simulink model "Hexalock.slx"  (R2026b)
settings: Solver=VariableStepAuto  StopTime=inf
undefined symbols (not defined in the file): gray
(part 1 of 5)
settings Model: Creator=joseph  LastModifiedBy=Medici

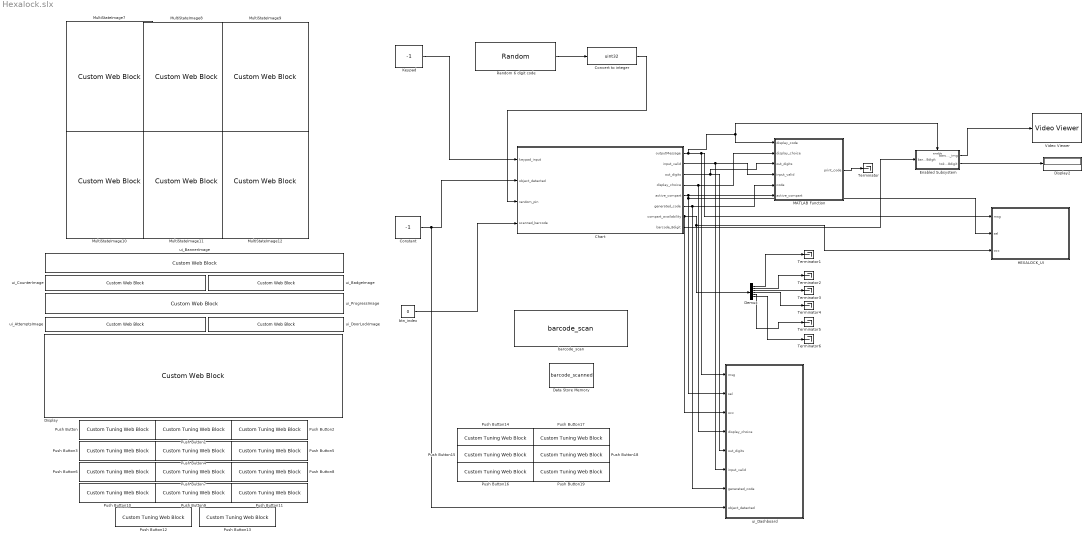
== system Hexalock.slx ==
  Chart : Stateflow chart  TreatAsAtomicUnit=on
  Constant : Constant  Value=-1
  Convert to integer : DataTypeConversion  OutDataTypeStr=uint32  RndMeth=Floor
  Data Store Memory : DataStoreMemory  DataStoreName=barcode_scanned  WriteAfterWriteMsg=warning  ShowAdditionalParam=off  OutDataTypeStr=double  Dimensions=1
  Demux : Demux  Outputs=6
  Display : CustomWebBlock  LabelPosition=Hide  ShowInitialText=on  Configuration="{\"components\":[{\"name\":\"DisplayComponent\",\"settings\":{\"alignment\":\"center\",\"bold\":false,\"font\":\"Noto Sans\",\"fontColor\":[255,255,200],\"fontSize\":18,\"format\":\"short\",\"formatString\":\"%d\",\"gridColor\":[252,252,197],\"italic\":false,\"position\":[0.1524671052631579,-0.02081787833827893,1.1009829376854599,0.7483552631578947],\"showGrid\":true,\"underline\":false}},{\"name\":\"BackgroundImageComponent\",\"settings\":{\"image\":{\"size\":[920,260],\"src\":\"data:image\\/svg+xml;base64,PHN2ZyB4bWxucz0iaHR0cDovL3d3dy53My5vcmcvMjAwMC9zdmciIHdpZHRoPSI5MjAiIGhlaWdodD0iMjYwIiB2aWV3Qm94PSIwIDAgOTIwIDI2MCI+CiAgPGRlZnM+CiAgICA8bGluZWFyR3JhZGllbnQgaWQ9InNoZWxsIiB4MT0iMCIgeTE9IjAiIHgyPSIwIiB5Mj0iMSI+CiAgICAgIDxzdG9wIG9mZnNldD0iMCIgc3RvcC1jb2xvcj0iIzQyNDk0RSIvPgogICAgICA8c3RvcCBvZmZzZXQ9IjAuNTAiIHN0b3AtY29sb3I9IiMyOTJGMzQiLz4KICAgICAgPHN0b3Agb2Zmc2V0PSIxIiBzdG9wLWNvbG9yPSIjMUIyMjI2Ii8+CiAg ...(+4416 chars)\",\"srcOrientation\":\"Right\"},\"position\":[0,0,1,1],\"scaleMode\":\"0\"}},{\"name\":\"ForegroundImageComponent\",\"settings\":{\"angle\":0,\"image\":{\"size\":[0,0],\"src\":\"default\"},\"isForeground\":1,\"position\":[0,0,1,1],\"scaleMode\":\"0\"}}],\"derived\":{\"blockParameters\":{\"alignment\":\"center\",\"fixedAspectRatio\":\"on\",\"format\":\"short\",\"formatString\":\"%d\",\"gridColor\":[252,252,197],\"showGrid\":true}},\"settings\":{\"BindingType\":\"signal\",\"aspectRatio\":1.032258064516129,\"backgroundColor\":[0,0,0,\"1\"],\"backgroundOffset\":0.14,\"backgroundOpacity\":1,\"fixedAspectRatio\":\"on\",\"showBackgroundColor\":false,\"value\":0,\"version\":\"R2026b\"},\"type\":\"Display\"}"
  Display2 : Display
  Enabled Subsystem : Subsystem  TreatAsAtomicUnit=on
  HEXALOCK_UI : Subsystem  Description=DISPLAY ONLY. Derives the per-locker visual code (0-11) from read-only branches of the controller outputs outputMessage, active_compart and compart_availability. Nothing in here feeds back into the controller.
  Keypad : Constant  Value=-1  VectorParams1D=off  OutDataTypeStr=double
  MATLAB Function : MATLAB Function  TreatAsAtomicUnit=on
  MultiStateImage10 : CustomWebBlock  LabelPosition=Hide  ShowInitialText=on  Configuration="{\"components\":[{\"name\":\"BackgroundImageComponent\",\"settings\":{\"image\":{\"size\":[0,0],\"src\":\"default\",\"srcOrientation\":\"Right\"},\"position\":[0,0,1,1],\"scaleMode\":\"0\"}},{\"name\":\"MultistateImageStateComponent\",\"settings\":{\"applyDefaults\":true,\"position\":[0,0,1,1],\"states\":[{\"image\":{\"size\":[0.7746478873239436,1],\"src\":\"data:image\\/svg+xml;base64,PHN2ZyB4bWxucz0iaHR0cDovL3d3dy53My5vcmcvMjAwMC9zdmciIHdpZHRoPSIyMjAiIGhlaWdodD0iMjg0IiB2aWV3Qm94PSIwIDAgMjIwIDI4NCIgcm9sZT0iaW1nIiA+Cjx0aXRsZT5IRVhBTE9DSyBtb2R1bGFyIGludGVyZmFjZSBhc3NldDwvdGl0bGU+CjxkZWZzPjwvZGVmcz4KICAgICAgPHJlY3QgeD0iOCIgeT0iOCIgd2lkdGg9IjIwNCIgaGVpZ2h0PSIyNjgiIHJ4PSIxNCIgZmlsbD0iIzExMUMyMiIgc3Ryb2tlPSIjNTM2NjZFIiBzdHJva2Utd2lkdGg9IjIiLz4KICAgICAgPHJlY3QgeD0iMTIiIHk9IjEyIiB3aWR0 ...(+3224 chars)\",\"srcOrientation\":\"Right\"},\"position\":[0,0,1,1],\"value\":[]},{\"image\":{\"size\":[0,0],\"src\":\"data:image\\/svg+xml;base64,PHN2ZyB4bWxucz0iaHR0cDovL3d3dy53My5vcmcvMjAwMC9zdmciIHdpZHRoPSIyMjAiIGhlaWdodD0iMjg0IiB2aWV3Qm94PSIwIDAgMjIwIDI4NCIgcm9sZT0iaW1nIiA+Cjx0aXRsZT5IRVhBTE9DSyBtb2R1bGFyIGludGVyZmFjZSBhc3NldDwvdGl0bGU+CjxkZWZzPjwvZGVmcz4KICAgICAgPHJlY3QgeD0iOCIgeT0iOCIgd2lkdGg9IjIwNCIgaGVpZ2h0PSIyNjgiIHJ4PSIxNCIgZmlsbD0iIzExMUMyMiIgc3Ryb2tlPSIjNTM2NjZFIiBzdHJva2Utd2lkdGg9IjIiLz4KICAgICAgPHJlY3QgeD0iMTIiIHk9IjEyIiB3aWR0 ...(+3224 chars)\",\"srcOrientation\":\"Right\"},\"position\":[0,0,1,1],\"value\":\"0\"},{\"image\":{\"size\":[0,0],\"src\":\"data:image\\/svg+xml;base64,PHN2ZyB4bWxucz0iaHR0cDovL3d3dy53My5vcmcvMjAwMC9zdmciIHdpZHRoPSIyMjAiIGhlaWdodD0iMjg0IiB2aWV3Qm94PSIwIDAgMjIwIDI4NCIgcm9sZT0iaW1nIiA+Cjx0aXRsZT5IRVhBTE9DSyBtb2R1bGFyIGludGVyZmFjZSBhc3NldDwvdGl0bGU+CjxkZWZzPjwvZGVmcz4KICAgICAgPHJlY3QgeD0iOCIgeT0iOCIgd2lkdGg9IjIwNCIgaGVpZ2h0PSIyNjgiIHJ4PSIxNCIgZmlsbD0iIzExMUMyMiIgc3Ryb2tlPSIjNTM2NjZFIiBzdHJva2Utd2lkdGg9IjIiLz4KICAgICAgPHJlY3QgeD0iMTIiIHk9IjEyIiB3aWR0 ...(+3220 chars)\",\"srcOrientation\":\"Right\"},\"position\":[0,0,1,1],\"value\":\"1\"},{\"image\":{\"size\":[0,0],\"src\":\"data:image\\/svg+xml;base64,PHN2ZyB4bWxucz0iaHR0cDovL3d3dy53My5vcmcvMjAwMC9zdmciIHdpZHRoPSIyMjAiIGhlaWdodD0iMjg0IiB2aWV3Qm94PSIwIDAgMjIwIDI4NCIgcm9sZT0iaW1nIiA+Cjx0aXRsZT5IRVhBTE9DSyBtb2R1bGFyIGludGVyZmFjZSBhc3NldDwvdGl0bGU+CjxkZWZzPjwvZGVmcz4KICAgICAgPHJlY3QgeD0iOCIgeT0iOCIgd2lkdGg9IjIwNCIgaGVpZ2h0PSIyNjgiIHJ4PSIxNCIgZmlsbD0iIzExMUMyMiIgc3Ryb2tlPSIjQjk4NTZFIiBzdHJva2Utd2lkdGg9IjIuNiIvPgogICAgICA8cmVjdCB4PSIxMiIgeT0iMTIiIHdp ...(+3488 chars)\",\"srcOrientation\":\"Right\"},\"position\":[0,0,1,1],\"value\":\"2\"},{\"image\":{\"size\":[0,0],\"src\":\"data:image\\/svg+xml;base64,PHN2ZyB4bWxucz0iaHR0cDovL3d3dy53My5vcmcvMjAwMC9zdmciIHdpZHRoPSIyMjAiIGhlaWdodD0iMjg0IiB2aWV3Qm94PSIwIDAgMjIwIDI4NCIgcm9sZT0iaW1nIiA+Cjx0aXRsZT5IRVhBTE9DSyBtb2R1bGFyIGludGVyZmFjZSBhc3NldDwvdGl0bGU+CjxkZWZzPjwvZGVmcz4KICAgICAgPHJlY3QgeD0iOCIgeT0iOCIgd2lkdGg9IjIwNCIgaGVpZ2h0PSIyNjgiIHJ4PSIxNCIgZmlsbD0iIzExMUMyMiIgc3Ryb2tlPSIjQjk4NTZFIiBzdHJva2Utd2lkdGg9IjIuNiIvPgogICAgICA8cmVjdCB4PSIxMiIgeT0iMTIiIHdp ...(+3484 chars)\",\"srcOrientation\":\"Right\"},\"position\":[0,0,1,1],\"value\":\"3\"},{\"image\":{\"size\":[0,0],\"src\":\"data:image\\/svg+xml;base64,PHN2ZyB4bWxucz0iaHR0cDovL3d3dy53My5vcmcvMjAwMC9zdmciIHdpZHRoPSIyMjAiIGhlaWdodD0iMjg0IiB2aWV3Qm94PSIwIDAgMjIwIDI4NCIgcm9sZT0iaW1nIiA+Cjx0aXRsZT5IRVhBTE9DSyBtb2R1bGFyIGludGVyZmFjZSBhc3NldDwvdGl0bGU+CjxkZWZzPjwvZGVmcz4KICAgICAgPHJlY3QgeD0iOCIgeT0iOCIgd2lkdGg9IjIwNCIgaGVpZ2h0PSIyNjgiIHJ4PSIxNCIgZmlsbD0iIzExMUMyMiIgc3Ryb2tlPSIjQjk4NTZFIiBzdHJva2Utd2lkdGg9IjIuNiIvPgogICAgICA8cmVjdCB4PSIxMiIgeT0iMTIiIHdp ...(+3532 chars)\",\"srcOrientation\":\"Right\"},\"position\":[0,0,1,1],\"value\":\"4\"},{\"image\":{\"size\":[0,0],\"src\":\"data:image\\/svg+xml;base64,PHN2ZyB4bWxucz0iaHR0cDovL3d3dy53My5vcmcvMjAwMC9zdmciIHdpZHRoPSIyMjAiIGhlaWdodD0iMjg0IiB2aWV3Qm94PSIwIDAgMjIwIDI4NCIgcm9sZT0iaW1nIiA+Cjx0aXRsZT5IRVhBTE9DSyBtb2R1bGFyIGludGVyZmFjZSBhc3NldDwvdGl0bGU+CjxkZWZzPjwvZGVmcz4KICAgICAgPHJlY3QgeD0iOCIgeT0iOCIgd2lkdGg9IjIwNCIgaGVpZ2h0PSIyNjgiIHJ4PSIxNCIgZmlsbD0iIzExMUMyMiIgc3Ryb2tlPSIjQjk4NTZFIiBzdHJva2Utd2lkdGg9IjIuNiIvPgogICAgICA8cmVjdCB4PSIxMiIgeT0iMTIiIHdp ...(+3532 chars)\",\"srcOrientation\":\"Right\"},\"position\":[0,0,1,1],\"value\":\"5\"},{\"image\":{\"size\":[0,0],\"src\":\"data:image\\/svg+xml;base64,PHN2ZyB4bWxucz0iaHR0cDovL3d3dy53My5vcmcvMjAwMC9zdmciIHdpZHRoPSIyMjAiIGhlaWdodD0iMjg0IiB2aWV3Qm94PSIwIDAgMjIwIDI4NCIgcm9sZT0iaW1nIiA+Cjx0aXRsZT5IRVhBTE9DSyBtb2R1bGFyIGludGVyZmFjZSBhc3NldDwvdGl0bGU+CjxkZWZzPjwvZGVmcz4KICAgICAgPHJlY3QgeD0iOCIgeT0iOCIgd2lkdGg9IjIwNCIgaGVpZ2h0PSIyNjgiIHJ4PSIxNCIgZmlsbD0iIzExMUMyMiIgc3Ryb2tlPSIjQjk4NTZFIiBzdHJva2Utd2lkdGg9IjIuNiIvPgogICAgICA8cmVjdCB4PSIxMiIgeT0iMTIiIHdp ...(+3532 chars)\",\"srcOrientation\":\"Right\"},\"position\":[0,0,1,1],\"value\":\"6\"},{\"image\":{\"size\":[0,0],\"src\":\"data:image\\/svg+xml;base64,PHN2ZyB4bWxucz0iaHR0cDovL3d3dy53My5vcmcvMjAwMC9zdmciIHdpZHRoPSIyMjAiIGhlaWdodD0iMjg0IiB2aWV3Qm94PSIwIDAgMjIwIDI4NCIgcm9sZT0iaW1nIiA+Cjx0aXRsZT5IRVhBTE9DSyBtb2R1bGFyIGludGVyZmFjZSBhc3NldDwvdGl0bGU+CjxkZWZzPjwvZGVmcz4KICAgICAgPHJlY3QgeD0iOCIgeT0iOCIgd2lkdGg9IjIwNCIgaGVpZ2h0PSIyNjgiIHJ4PSIxNCIgZmlsbD0iIzExMUMyMiIgc3Ryb2tlPSIjQjk4NTZFIiBzdHJva2Utd2lkdGg9IjIuNiIvPgogICAgICA8cmVjdCB4PSIxMiIgeT0iMTIiIHdp ...(+3524 chars)\",\"srcOrientation\":\"Right\"},\"position\":[0,0,1,1],\"value\":\"7\"},{\"image\":{\"size\":[0,0],\"src\":\"data:image\\/svg+xml;base64,PHN2ZyB4bWxucz0iaHR0cDovL3d3dy53My5vcmcvMjAwMC9zdmciIHdpZHRoPSIyMjAiIGhlaWdodD0iMjg0IiB2aWV3Qm94PSIwIDAgMjIwIDI4NCIgcm9sZT0iaW1nIiA+Cjx0aXRsZT5IRVhBTE9DSyBtb2R1bGFyIGludGVyZmFjZSBhc3NldDwvdGl0bGU+CjxkZWZzPjwvZGVmcz4KICAgICAgPHJlY3QgeD0iOCIgeT0iOCIgd2lkdGg9IjIwNCIgaGVpZ2h0PSIyNjgiIHJ4PSIxNCIgZmlsbD0iIzExMUMyMiIgc3Ryb2tlPSIjQjk4NTZFIiBzdHJva2Utd2lkdGg9IjIuNiIvPgogICAgICA8cmVjdCB4PSIxMiIgeT0iMTIiIHdp ...(+3532 chars)\",\"srcOrientation\":\"Right\"},\"position\":[0,0,1,1],\"value\":\"8\"},{\"image\":{\"size\":[0,0],\"src\":\"data:image\\/svg+xml;base64,PHN2ZyB4bWxucz0iaHR0cDovL3d3dy53My5vcmcvMjAwMC9zdmciIHdpZHRoPSIyMjAiIGhlaWdodD0iMjg0IiB2aWV3Qm94PSIwIDAgMjIwIDI4NCIgcm9sZT0iaW1nIiA+Cjx0aXRsZT5IRVhBTE9DSyBtb2R1bGFyIGludGVyZmFjZSBhc3NldDwvdGl0bGU+CjxkZWZzPjwvZGVmcz4KICAgICAgPHJlY3QgeD0iOCIgeT0iOCIgd2lkdGg9IjIwNCIgaGVpZ2h0PSIyNjgiIHJ4PSIxNCIgZmlsbD0iIzExMUMyMiIgc3Ryb2tlPSIjQjk4NTZFIiBzdHJva2Utd2lkdGg9IjIuNiIvPgogICAgICA8cmVjdCB4PSIxMiIgeT0iMTIiIHdp ...(+3532 chars)\",\"srcOrientation\":\"Right\"},\"position\":[0,0,1,1],\"value\":\"9\"},{\"image\":{\"size\":[0,0],\"src\":\"data:image\\/svg+xml;base64,PHN2ZyB4bWxucz0iaHR0cDovL3d3dy53My5vcmcvMjAwMC9zdmciIHdpZHRoPSIyMjAiIGhlaWdodD0iMjg0IiB2aWV3Qm94PSIwIDAgMjIwIDI4NCIgcm9sZT0iaW1nIiA+Cjx0aXRsZT5IRVhBTE9DSyBtb2R1bGFyIGludGVyZmFjZSBhc3NldDwvdGl0bGU+CjxkZWZzPjwvZGVmcz4KICAgICAgPHJlY3QgeD0iOCIgeT0iOCIgd2lkdGg9IjIwNCIgaGVpZ2h0PSIyNjgiIHJ4PSIxNCIgZmlsbD0iIzExMUMyMiIgc3Ryb2tlPSIjQjk4NTZFIiBzdHJva2Utd2lkdGg9IjIuNiIvPgogICAgICA8cmVjdCB4PSIxMiIgeT0iMTIiIHdp ...(+3532 chars)\",\"srcOrientation\":\"Right\"},\"position\":[0,0,1,1],\"value\":\"10\"},{\"image\":{\"size\":[0,0],\"src\":\"data:image\\/svg+xml;base64,PHN2ZyB4bWxucz0iaHR0cDovL3d3dy53My5vcmcvMjAwMC9zdmciIHdpZHRoPSIyMjAiIGhlaWdodD0iMjg0IiB2aWV3Qm94PSIwIDAgMjIwIDI4NCIgcm9sZT0iaW1nIiA+Cjx0aXRsZT5IRVhBTE9DSyBtb2R1bGFyIGludGVyZmFjZSBhc3NldDwvdGl0bGU+CjxkZWZzPjwvZGVmcz4KICAgICAgPHJlY3QgeD0iOCIgeT0iOCIgd2lkdGg9IjIwNCIgaGVpZ2h0PSIyNjgiIHJ4PSIxNCIgZmlsbD0iIzExMUMyMiIgc3Ryb2tlPSIjNTM2NjZFIiBzdHJva2Utd2lkdGg9IjIiLz4KICAgICAgPHJlY3QgeD0iMTIiIHk9IjEyIiB3aWR0 ...(+3220 chars)\",\"srcOrientation\":\"Right\"},\"position\":[0,0,1,1],\"value\":\"11\"},{\"image\":{\"size\":[0,0],\"src\":\"data:image\\/svg+xml;base64,PHN2ZyB4bWxucz0iaHR0cDovL3d3dy53My5vcmcvMjAwMC9zdmciIHdpZHRoPSIyMjAiIGhlaWdodD0iMjg0IiB2aWV3Qm94PSIwIDAgMjIwIDI4NCIgcm9sZT0iaW1nIiA+Cjx0aXRsZT5IRVhBTE9DSyBtb2R1bGFyIGludGVyZmFjZSBhc3NldDwvdGl0bGU+CjxkZWZzPjxsaW5lYXJHcmFkaWVudCBpZD0ia3JhZnRGcm9udCIgeDE9IjAiIHkxPSIwIiB4Mj0iMSIgeTI9IjEiPjxzdG9wIHN0b3AtY29sb3I9IiNEM0I5OUEiLz48c3RvcCBvZmZzZXQ9IjEiIHN0b3AtY29sb3I9IiNBMzgzNjMiLz48L2xpbmVhckdyYWRpZW50Pjxs ...(+4752 chars)\",\"srcOrientation\":\"Right\"},\"position\":[0,0,1,1],\"value\":\"20\"},{\"image\":{\"size\":[0,0],\"src\":\"data:image\\/svg+xml;base64,PHN2ZyB4bWxucz0iaHR0cDovL3d3dy53My5vcmcvMjAwMC9zdmciIHdpZHRoPSIyMjAiIGhlaWdodD0iMjg0IiB2aWV3Qm94PSIwIDAgMjIwIDI4NCIgcm9sZT0iaW1nIiA+Cjx0aXRsZT5IRVhBTE9DSyBtb2R1bGFyIGludGVyZmFjZSBhc3NldDwvdGl0bGU+CjxkZWZzPjxsaW5lYXJHcmFkaWVudCBpZD0ia3JhZnRGcm9udCIgeDE9IjAiIHkxPSIwIiB4Mj0iMSIgeTI9IjEiPjxzdG9wIHN0b3AtY29sb3I9IiNEM0I5OUEiLz48c3RvcCBvZmZzZXQ9IjEiIHN0b3AtY29sb3I9IiNBMzgzNjMiLz48L2xpbmVhckdyYWRpZW50Pjxs ...(+7264 chars)\",\"srcOrientation\":\"Right\"},\"position\":[0,0,1,1],\"value\":\"21\"},{\"image\":{\"size\":[0,0],\"src\":\"data:image\\/svg+xml;base64,PHN2ZyB4bWxucz0iaHR0cDovL3d3dy53My5vcmcvMjAwMC9zdmciIHdpZHRoPSIyMjAiIGhlaWdodD0iMjg0IiB2aWV3Qm94PSIwIDAgMjIwIDI4NCIgcm9sZT0iaW1nIiA+Cjx0aXRsZT5IRVhBTE9DSyBtb2R1bGFyIGludGVyZmFjZSBhc3NldDwvdGl0bGU+CjxkZWZzPjxsaW5lYXJHcmFkaWVudCBpZD0ia3JhZnRGcm9udCIgeDE9IjAiIHkxPSIwIiB4Mj0iMSIgeTI9IjEiPjxzdG9wIHN0b3AtY29sb3I9IiNEM0I5OUEiLz48c3RvcCBvZmZzZXQ9IjEiIHN0b3AtY29sb3I9IiNBMzgzNjMiLz48L2xpbmVhckdyYWRpZW50Pjxs ...(+7264 chars)\",\"srcOrientation\":\"Right\"},\"position\":[0,0,1,1],\"value\":\"22\"},{\"image\":{\"size\":[0,0],\"src\":\"data:image\\/svg+xml;base64,PHN2ZyB4bWxucz0iaHR0cDovL3d3dy53My5vcmcvMjAwMC9zdmciIHdpZHRoPSIyMjAiIGhlaWdodD0iMjg0IiB2aWV3Qm94PSIwIDAgMjIwIDI4NCIgcm9sZT0iaW1nIiA+Cjx0aXRsZT5IRVhBTE9DSyBtb2R1bGFyIGludGVyZmFjZSBhc3NldDwvdGl0bGU+CjxkZWZzPjxsaW5lYXJHcmFkaWVudCBpZD0ia3JhZnRGcm9udCIgeDE9IjAiIHkxPSIwIiB4Mj0iMSIgeTI9IjEiPjxzdG9wIHN0b3AtY29sb3I9IiNEM0I5OUEiLz48c3RvcCBvZmZzZXQ9IjEiIHN0b3AtY29sb3I9IiNBMzgzNjMiLz48L2xpbmVhckdyYWRpZW50Pjxs ...(+7264 chars)\",\"srcOrientation\":\"Right\"},\"position\":[0,0,1,1],\"value\":\"23\"},{\"image\":{\"size\":[0,0],\"src\":\"data:image\\/svg+xml;base64,PHN2ZyB4bWxucz0iaHR0cDovL3d3dy53My5vcmcvMjAwMC9zdmciIHdpZHRoPSIyMjAiIGhlaWdodD0iMjg0IiB2aWV3Qm94PSIwIDAgMjIwIDI4NCIgcm9sZT0iaW1nIiA+Cjx0aXRsZT5IRVhBTE9DSyBtb2R1bGFyIGludGVyZmFjZSBhc3NldDwvdGl0bGU+CjxkZWZzPjxsaW5lYXJHcmFkaWVudCBpZD0ia3JhZnRGcm9udCIgeDE9IjAiIHkxPSIwIiB4Mj0iMSIgeTI9IjEiPjxzdG9wIHN0b3AtY29sb3I9IiNEM0I5OUEiLz48c3RvcCBvZmZzZXQ9IjEiIHN0b3AtY29sb3I9IiNBMzgzNjMiLz48L2xpbmVhckdyYWRpZW50Pjxs ...(+7260 chars)\",\"srcOrientation\":\"Right\"},\"position\":[0,0,1,1],\"value\":\"24\"},{\"image\":{\"size\":[0,0],\"src\":\"data:image\\/svg+xml;base64,PHN2ZyB4bWxucz0iaHR0cDovL3d3dy53My5vcmcvMjAwMC9zdmciIHdpZHRoPSIyMjAiIGhlaWdodD0iMjg0IiB2aWV3Qm94PSIwIDAgMjIwIDI4NCIgcm9sZT0iaW1nIiA+Cjx0aXRsZT5IRVhBTE9DSyBtb2R1bGFyIGludGVyZmFjZSBhc3NldDwvdGl0bGU+CjxkZWZzPjxsaW5lYXJHcmFkaWVudCBpZD0ia3JhZnRGcm9udCIgeDE9IjAiIHkxPSIwIiB4Mj0iMSIgeTI9IjEiPjxzdG9wIHN0b3AtY29sb3I9IiNEM0I5OUEiLz48c3RvcCBvZmZzZXQ9IjEiIHN0b3AtY29sb3I9IiNBMzgzNjMiLz48L2xpbmVhckdyYWRpZW50Pjxs ...(+7264 chars)\",\"srcOrientation\":\"Right\"},\"position\":[0,0,1,1],\"value\":\"25\"},{\"image\":{\"size\":[0,0],\"src\":\"data:image\\/svg+xml;base64,PHN2ZyB4bWxucz0iaHR0cDovL3d3dy53My5vcmcvMjAwMC9zdmciIHdpZHRoPSIyMjAiIGhlaWdodD0iMjg0IiB2aWV3Qm94PSIwIDAgMjIwIDI4NCIgcm9sZT0iaW1nIiA+Cjx0aXRsZT5IRVhBTE9DSyBtb2R1bGFyIGludGVyZmFjZSBhc3NldDwvdGl0bGU+CjxkZWZzPjxsaW5lYXJHcmFkaWVudCBpZD0ia3JhZnRGcm9udCIgeDE9IjAiIHkxPSIwIiB4Mj0iMSIgeTI9IjEiPjxzdG9wIHN0b3AtY29sb3I9IiNEM0I5OUEiLz48c3RvcCBvZmZzZXQ9IjEiIHN0b3AtY29sb3I9IiNBMzgzNjMiLz48L2xpbmVhckdyYWRpZW50Pjxs ...(+7272 chars)\",\"srcOrientation\":\"Right\"},\"position\":[0,0,1,1],\"value\":\"26\"},{\"image\":{\"size\":[0,0],\"src\":\"data:image\\/svg+xml;base64,PHN2ZyB4bWxucz0iaHR0cDovL3d3dy53My5vcmcvMjAwMC9zdmciIHdpZHRoPSIyMjAiIGhlaWdodD0iMjg0IiB2aWV3Qm94PSIwIDAgMjIwIDI4NCIgcm9sZT0iaW1nIiA+Cjx0aXRsZT5IRVhBTE9DSyBtb2R1bGFyIGludGVyZmFjZSBhc3NldDwvdGl0bGU+CjxkZWZzPjxsaW5lYXJHcmFkaWVudCBpZD0ia3JhZnRGcm9udCIgeDE9IjAiIHkxPSIwIiB4Mj0iMSIgeTI9IjEiPjxzdG9wIHN0b3AtY29sb3I9IiNEM0I5OUEiLz48c3RvcCBvZmZzZXQ9IjEiIHN0b3AtY29sb3I9IiNBMzgzNjMiLz48L2xpbmVhckdyYWRpZW50Pjxs ...(+7264 chars)\",\"srcOrientation\":\"Right\"},\"position\":[0,0,1,1],\"value\":\"27\"},{\"image\":{\"size\":[0,0],\"src\":\"data:image\\/svg+xml;base64,PHN2ZyB4bWxucz0iaHR0cDovL3d3dy53My5vcmcvMjAwMC9zdmciIHdpZHRoPSIyMjAiIGhlaWdodD0iMjg0IiB2aWV3Qm94PSIwIDAgMjIwIDI4NCIgcm9sZT0iaW1nIiA+Cjx0aXRsZT5IRVhBTE9DSyBtb2R1bGFyIGludGVyZmFjZSBhc3NldDwvdGl0bGU+CjxkZWZzPjxsaW5lYXJHcmFkaWVudCBpZD0ia3JhZnRGcm9udCIgeDE9IjAiIHkxPSIwIiB4Mj0iMSIgeTI9IjEiPjxzdG9wIHN0b3AtY29sb3I9IiNEM0I5OUEiLz48c3RvcCBvZmZzZXQ9IjEiIHN0b3AtY29sb3I9IiNBMzgzNjMiLz48L2xpbmVhckdyYWRpZW50Pjxs ...(+7268 chars)\",\"srcOrientation\":\"Right\"},\"position\":[0,0,1,1],\"value\":\"28\"},{\"image\":{\"size\":[0,0],\"src\":\"data:image\\/svg+xml;base64,PHN2ZyB4bWxucz0iaHR0cDovL3d3dy53My5vcmcvMjAwMC9zdmciIHdpZHRoPSIyMjAiIGhlaWdodD0iMjg0IiB2aWV3Qm94PSIwIDAgMjIwIDI4NCIgcm9sZT0iaW1nIiA+Cjx0aXRsZT5IRVhBTE9DSyBtb2R1bGFyIGludGVyZmFjZSBhc3NldDwvdGl0bGU+CjxkZWZzPjxsaW5lYXJHcmFkaWVudCBpZD0ia3JhZnRGcm9udCIgeDE9IjAiIHkxPSIwIiB4Mj0iMSIgeTI9IjEiPjxzdG9wIHN0b3AtY29sb3I9IiNEM0I5OUEiLz48c3RvcCBvZmZzZXQ9IjEiIHN0b3AtY29sb3I9IiNBMzgzNjMiLz48L2xpbmVhckdyYWRpZW50Pjxs ...(+7268 chars)\",\"srcOrientation\":\"Right\"},\"position\":[0,0,1,1],\"value\":\"29\"},{\"image\":{\"size\":[0,0],\"src\":\"data:image\\/svg+xml;base64,PHN2ZyB4bWxucz0iaHR0cDovL3d3dy53My5vcmcvMjAwMC9zdmciIHdpZHRoPSIyMjAiIGhlaWdodD0iMjg0IiB2aWV3Qm94PSIwIDAgMjIwIDI4NCIgcm9sZT0iaW1nIiA+Cjx0aXRsZT5IRVhBTE9DSyBtb2R1bGFyIGludGVyZmFjZSBhc3NldDwvdGl0bGU+CjxkZWZzPjxsaW5lYXJHcmFkaWVudCBpZD0ia3JhZnRGcm9udCIgeDE9IjAiIHkxPSIwIiB4Mj0iMSIgeTI9IjEiPjxzdG9wIHN0b3AtY29sb3I9IiNEM0I5OUEiLz48c3RvcCBvZmZzZXQ9IjEiIHN0b3AtY29sb3I9IiNBMzgzNjMiLz48L2xpbmVhckdyYWRpZW50Pjxs ...(+7268 chars)\",\"srcOrientation\":\"Right\"},\"position\":[0,0,1,1],\"value\":\"30\"},{\"image\":{\"size\":[0,0],\"src\":\"data:image\\/svg+xml;base64,PHN2ZyB4bWxucz0iaHR0cDovL3d3dy53My5vcmcvMjAwMC9zdmciIHdpZHRoPSIyMjAiIGhlaWdodD0iMjg0IiB2aWV3Qm94PSIwIDAgMjIwIDI4NCIgcm9sZT0iaW1nIiA+Cjx0aXRsZT5IRVhBTE9DSyBtb2R1bGFyIGludGVyZmFjZSBhc3NldDwvdGl0bGU+CjxkZWZzPjxsaW5lYXJHcmFkaWVudCBpZD0ia3JhZnRGcm9udCIgeDE9IjAiIHkxPSIwIiB4Mj0iMSIgeTI9IjEiPjxzdG9wIHN0b3AtY29sb3I9IiNEM0I5OUEiLz48c3RvcCBvZmZzZXQ9IjEiIHN0b3AtY29sb3I9IiNBMzgzNjMiLz48L2xpbmVhckdyYWRpZW50Pjxs ...(+4756 chars)\",\"srcOrientation\":\"Right\"},\"position\":[0,0,1,1],\"value\":\"31\"},{\"image\":{\"size\":[0,0],\"src\":\"data:image\\/svg+xml;base64,PHN2ZyB4bWxucz0iaHR0cDovL3d3dy53My5vcmcvMjAwMC9zdmciIHdpZHRoPSIyMjAiIGhlaWdodD0iMjg0IiB2aWV3Qm94PSIwIDAgMjIwIDI4NCIgcm9sZT0iaW1nIiA+Cjx0aXRsZT5IRVhBTE9DSyBtb2R1bGFyIGludGVyZmFjZSBhc3NldDwvdGl0bGU+CjxkZWZzPjxsaW5lYXJHcmFkaWVudCBpZD0ia3JhZnRGcm9udCIgeDE9IjAiIHkxPSIwIiB4Mj0iMSIgeTI9IjEiPjxzdG9wIHN0b3AtY29sb3I9IiNEM0I5OUEiLz48c3RvcCBvZmZzZXQ9IjEiIHN0b3AtY29sb3I9IiNBMzgzNjMiLz48L2xpbmVhckdyYWRpZW50Pjxs ...(+4752 chars)\",\"srcOrientation\":\"Right\"},\"position\":[0,0,1,1],\"value\":\"32\"},{\"image\":{\"size\":[0,0],\"src\":\"data:image\\/svg+xml;base64,PHN2ZyB4bWxucz0iaHR0cDovL3d3dy53My5vcmcvMjAwMC9zdmciIHdpZHRoPSIyMjAiIGhlaWdodD0iMjg0IiB2aWV3Qm94PSIwIDAgMjIwIDI4NCIgcm9sZT0iaW1nIiA+Cjx0aXRsZT5IRVhBTE9DSyBtb2R1bGFyIGludGVyZmFjZSBhc3NldDwvdGl0bGU+CjxkZWZzPjxsaW5lYXJHcmFkaWVudCBpZD0ia3JhZnRGcm9udCIgeDE9IjAiIHkxPSIwIiB4Mj0iMSIgeTI9IjEiPjxzdG9wIHN0b3AtY29sb3I9IiNEM0I5OUEiLz48c3RvcCBvZmZzZXQ9IjEiIHN0b3AtY29sb3I9IiNBMzgzNjMiLz48L2xpbmVhckdyYWRpZW50Pjxs ...(+6860 chars)\",\"srcOrientation\":\"Right\"},\"position\":[0,0,1,1],\"value\":\"33\"},{\"image\":{\"size\":[0,0],\"src\":\"data:image\\/svg+xml;base64,PHN2ZyB4bWxucz0iaHR0cDovL3d3dy53My5vcmcvMjAwMC9zdmciIHdpZHRoPSIyMjAiIGhlaWdodD0iMjg0IiB2aWV3Qm94PSIwIDAgMjIwIDI4NCIgcm9sZT0iaW1nIiA+Cjx0aXRsZT5IRVhBTE9DSyBtb2R1bGFyIGludGVyZmFjZSBhc3NldDwvdGl0bGU+CjxkZWZzPjxsaW5lYXJHcmFkaWVudCBpZD0ia3JhZnRGcm9udCIgeDE9IjAiIHkxPSIwIiB4Mj0iMSIgeTI9IjEiPjxzdG9wIHN0b3AtY29sb3I9IiNEM0I5OUEiLz48c3RvcCBvZmZzZXQ9IjEiIHN0b3AtY29sb3I9IiNBMzgzNjMiLz48L2xpbmVhckdyYWRpZW50Pjxs ...(+6860 chars)\",\"srcOrientation\":\"Right\"},\"position\":[0,0,1,1],\"value\":\"34\"},{\"image\":{\"size\":[0,0],\"src\":\"data:image\\/svg+xml;base64,PHN2ZyB4bWxucz0iaHR0cDovL3d3dy53My5vcmcvMjAwMC9zdmciIHdpZHRoPSIyMjAiIGhlaWdodD0iMjg0IiB2aWV3Qm94PSIwIDAgMjIwIDI4NCIgcm9sZT0iaW1nIiA+Cjx0aXRsZT5IRVhBTE9DSyBtb2R1bGFyIGludGVyZmFjZSBhc3NldDwvdGl0bGU+CjxkZWZzPjxsaW5lYXJHcmFkaWVudCBpZD0ia3JhZnRGcm9udCIgeDE9IjAiIHkxPSIwIiB4Mj0iMSIgeTI9IjEiPjxzdG9wIHN0b3AtY29sb3I9IiNEM0I5OUEiLz48c3RvcCBvZmZzZXQ9IjEiIHN0b3AtY29sb3I9IiNBMzgzNjMiLz48L2xpbmVhckdyYWRpZW50Pjxs ...(+6860 chars)\",\"srcOrientation\":\"Right\"},\"position\":[0,0,1,1],\"value\":\"35\"},{\"image\":{\"size\":[0,0],\"src\":\"data:image\\/svg+xml;base64,PHN2ZyB4bWxucz0iaHR0cDovL3d3dy53My5vcmcvMjAwMC9zdmciIHdpZHRoPSIyMjAiIGhlaWdodD0iMjg0IiB2aWV3Qm94PSIwIDAgMjIwIDI4NCIgcm9sZT0iaW1nIiA+DQo8dGl0bGU+SEVYQUxPQ0sgbW9kdWxhciBpbnRlcmZhY2UgYXNzZXQ8L3RpdGxlPg0KPGRlZnM+PGxpbmVhckdyYWRpZW50IGlkPSJrcmFmdEZyb250IiB4MT0iMCIgeTE9IjAiIHgyPSIxIiB5Mj0iMSI+PHN0b3Agc3RvcC1jb2xvcj0iI0QzQjk5QSIvPjxzdG9wIG9mZnNldD0iMSIgc3RvcC1jb2xvcj0iI0EzODM2MyIvPjwvbGluZWFyR3JhZGllbnQ+ ...(+6912 chars)\",\"srcOrientation\":\"Right\"},\"position\":[0,0,1,1],\"value\":\"36\"},{\"image\":{\"size\":[0,0],\"src\":\"data:image\\/svg+xml;base64,PHN2ZyB4bWxucz0iaHR0cDovL3d3dy53My5vcmcvMjAwMC9zdmciIHdpZHRoPSIyMjAiIGhlaWdodD0iMjg0IiB2aWV3Qm94PSIwIDAgMjIwIDI4NCIgcm9sZT0iaW1nIiA+DQo8dGl0bGU+SEVYQUxPQ0sgbW9kdWxhciBpbnRlcmZhY2UgYXNzZXQ8L3RpdGxlPg0KPGRlZnM+PGxpbmVhckdyYWRpZW50IGlkPSJrcmFmdEZyb250IiB4MT0iMCIgeTE9IjAiIHgyPSIxIiB5Mj0iMSI+PHN0b3Agc3RvcC1jb2xvcj0iI0QzQjk5QSIvPjxzdG9wIG9mZnNldD0iMSIgc3RvcC1jb2xvcj0iI0EzODM2MyIvPjwvbGluZWFyR3JhZGllbnQ+ ...(+6912 chars)\",\"srcOrientation\":\"Right\"},\"position\":[0,0,1,1],\"value\":\"37\"},{\"image\":{\"size\":[0,0],\"src\":\"data:image\\/svg+xml;base64,PHN2ZyB4bWxucz0iaHR0cDovL3d3dy53My5vcmcvMjAwMC9zdmciIHdpZHRoPSIyMjAiIGhlaWdodD0iMjg0IiB2aWV3Qm94PSIwIDAgMjIwIDI4NCIgcm9sZT0iaW1nIiA+DQo8dGl0bGU+SEVYQUxPQ0sgbW9kdWxhciBpbnRlcmZhY2UgYXNzZXQ8L3RpdGxlPg0KPGRlZnM+PGxpbmVhckdyYWRpZW50IGlkPSJrcmFmdEZyb250IiB4MT0iMCIgeTE9IjAiIHgyPSIxIiB5Mj0iMSI+PHN0b3Agc3RvcC1jb2xvcj0iI0QzQjk5QSIvPjxzdG9wIG9mZnNldD0iMSIgc3RvcC1jb2xvcj0iI0EzODM2MyIvPjwvbGluZWFyR3JhZGllbnQ+ ...(+6912 chars)\",\"srcOrientation\":\"Right\"},\"position\":[0,0,1,1],\"value\":\"38\"}],\"valueType\":\"discrete\"}},{\"name\":\"ForegroundImageComponent\",\"settings\":{\"image\":{\"size\":[0,0],\"src\":\"default\",\"srcOrientation\":\"Right\"},\"isForeground\":1,\"position\":[0,0,1,1],\"scaleMode\":\"0\"}}],\"derived\":{\"blockParameters\":{\"DefaultImage\":\"data:image\\/svg+xml;base64,PHN2ZyB4bWxucz0iaHR0cDovL3d3dy53My5vcmcvMjAwMC9zdmciIHdpZHRoPSIyMjAiIGhlaWdodD0iMjg0IiB2aWV3Qm94PSIwIDAgMjIwIDI4NCIgcm9sZT0iaW1nIiA+Cjx0aXRsZT5IRVhBTE9DSyBtb2R1bGFyIGludGVyZmFjZSBhc3NldDwvdGl0bGU+CjxkZWZzPjwvZGVmcz4KICAgICAgPHJlY3QgeD0iOCIgeT0iOCIgd2lkdGg9IjIwNCIgaGVpZ2h0PSIyNjgiIHJ4PSIxNCIgZmlsbD0iIzExMUMyMiIgc3Ryb2tlPSIjNTM2NjZFIiBzdHJva2Utd2lkdGg9IjIiLz4KICAgICAgPHJlY3QgeD0iMTIiIHk9IjEyIiB3aWR0 ...(+3224 chars)\",\"StateValueType\":\"discrete\",\"States\":[{\"image\":\"data:image\\/svg+xml;base64,PHN2ZyB4bWxucz0iaHR0cDovL3d3dy53My5vcmcvMjAwMC9zdmciIHdpZHRoPSIyMjAiIGhlaWdodD0iMjg0IiB2aWV3Qm94PSIwIDAgMjIwIDI4NCIgcm9sZT0iaW1nIiA+Cjx0aXRsZT5IRVhBTE9DSyBtb2R1bGFyIGludGVyZmFjZSBhc3NldDwvdGl0bGU+CjxkZWZzPjwvZGVmcz4KICAgICAgPHJlY3QgeD0iOCIgeT0iOCIgd2lkdGg9IjIwNCIgaGVpZ2h0PSIyNjgiIHJ4PSIxNCIgZmlsbD0iIzExMUMyMiIgc3Ryb2tlPSIjNTM2NjZFIiBzdHJva2Utd2lkdGg9IjIiLz4KICAgICAgPHJlY3QgeD0iMTIiIHk9IjEyIiB3aWR0 ...(+3224 chars)\",\"value\":\"0\"},{\"image\":\"data:image\\/svg+xml;base64,PHN2ZyB4bWxucz0iaHR0cDovL3d3dy53My5vcmcvMjAwMC9zdmciIHdpZHRoPSIyMjAiIGhlaWdodD0iMjg0IiB2aWV3Qm94PSIwIDAgMjIwIDI4NCIgcm9sZT0iaW1nIiA+Cjx0aXRsZT5IRVhBTE9DSyBtb2R1bGFyIGludGVyZmFjZSBhc3NldDwvdGl0bGU+CjxkZWZzPjwvZGVmcz4KICAgICAgPHJlY3QgeD0iOCIgeT0iOCIgd2lkdGg9IjIwNCIgaGVpZ2h0PSIyNjgiIHJ4PSIxNCIgZmlsbD0iIzExMUMyMiIgc3Ryb2tlPSIjNTM2NjZFIiBzdHJva2Utd2lkdGg9IjIiLz4KICAgICAgPHJlY3QgeD0iMTIiIHk9IjEyIiB3aWR0 ...(+3220 chars)\",\"value\":\"1\"},{\"image\":\"data:image\\/svg+xml;base64,PHN2ZyB4bWxucz0iaHR0cDovL3d3dy53My5vcmcvMjAwMC9zdmciIHdpZHRoPSIyMjAiIGhlaWdodD0iMjg0IiB2aWV3Qm94PSIwIDAgMjIwIDI4NCIgcm9sZT0iaW1nIiA+Cjx0aXRsZT5IRVhBTE9DSyBtb2R1bGFyIGludGVyZmFjZSBhc3NldDwvdGl0bGU+CjxkZWZzPjwvZGVmcz4KICAgICAgPHJlY3QgeD0iOCIgeT0iOCIgd2lkdGg9IjIwNCIgaGVpZ2h0PSIyNjgiIHJ4PSIxNCIgZmlsbD0iIzExMUMyMiIgc3Ryb2tlPSIjQjk4NTZFIiBzdHJva2Utd2lkdGg9IjIuNiIvPgogICAgICA8cmVjdCB4PSIxMiIgeT0iMTIiIHdp ...(+3488 chars)\",\"value\":\"2\"},{\"image\":\"data:image\\/svg+xml;base64,PHN2ZyB4bWxucz0iaHR0cDovL3d3dy53My5vcmcvMjAwMC9zdmciIHdpZHRoPSIyMjAiIGhlaWdodD0iMjg0IiB2aWV3Qm94PSIwIDAgMjIwIDI4NCIgcm9sZT0iaW1nIiA+Cjx0aXRsZT5IRVhBTE9DSyBtb2R1bGFyIGludGVyZmFjZSBhc3NldDwvdGl0bGU+CjxkZWZzPjwvZGVmcz4KICAgICAgPHJlY3QgeD0iOCIgeT0iOCIgd2lkdGg9IjIwNCIgaGVpZ2h0PSIyNjgiIHJ4PSIxNCIgZmlsbD0iIzExMUMyMiIgc3Ryb2tlPSIjQjk4NTZFIiBzdHJva2Utd2lkdGg9IjIuNiIvPgogICAgICA8cmVjdCB4PSIxMiIgeT0iMTIiIHdp ...(+3484 chars)\",\"value\":\"3\"},{\"image\":\"data:image\\/svg+xml;base64,PHN2ZyB4bWxucz0iaHR0cDovL3d3dy53My5vcmcvMjAwMC9zdmciIHdpZHRoPSIyMjAiIGhlaWdodD0iMjg0IiB2aWV3Qm94PSIwIDAgMjIwIDI4NCIgcm9sZT0iaW1nIiA+Cjx0aXRsZT5IRVhBTE9DSyBtb2R1bGFyIGludGVyZmFjZSBhc3NldDwvdGl0bGU+CjxkZWZzPjwvZGVmcz4KICAgICAgPHJlY3QgeD0iOCIgeT0iOCIgd2lkdGg9IjIwNCIgaGVpZ2h0PSIyNjgiIHJ4PSIxNCIgZmlsbD0iIzExMUMyMiIgc3Ryb2tlPSIjQjk4NTZFIiBzdHJva2Utd2lkdGg9IjIuNiIvPgogICAgICA8cmVjdCB4PSIxMiIgeT0iMTIiIHdp ...(+3532 chars)\",\"value\":\"4\"},{\"image\":\"data:image\\/svg+xml;base64,PHN2ZyB4bWxucz0iaHR0cDovL3d3dy53My5vcmcvMjAwMC9zdmciIHdpZHRoPSIyMjAiIGhlaWdodD0iMjg0IiB2aWV3Qm94PSIwIDAgMjIwIDI4NCIgcm9sZT0iaW1nIiA+Cjx0aXRsZT5IRVhBTE9DSyBtb2R1bGFyIGludGVyZmFjZSBhc3NldDwvdGl0bGU+CjxkZWZzPjwvZGVmcz4KICAgICAgPHJlY3QgeD0iOCIgeT0iOCIgd2lkdGg9IjIwNCIgaGVpZ2h0PSIyNjgiIHJ4PSIxNCIgZmlsbD0iIzExMUMyMiIgc3Ryb2tlPSIjQjk4NTZFIiBzdHJva2Utd2lkdGg9IjIuNiIvPgogICAgICA8cmVjdCB4PSIxMiIgeT0iMTIiIHdp ...(+3532 chars)\",\"value\":\"5\"},{\"image\":\"data:image\\/svg+xml;base64,PHN2ZyB4bWxucz0iaHR0cDovL3d3dy53My5vcmcvMjAwMC9zdmciIHdpZHRoPSIyMjAiIGhlaWdodD0iMjg0IiB2aWV3Qm94PSIwIDAgMjIwIDI4NCIgcm9sZT0iaW1nIiA+Cjx0aXRsZT5IRVhBTE9DSyBtb2R1bGFyIGludGVyZmFjZSBhc3NldDwvdGl0bGU+CjxkZWZzPjwvZGVmcz4KICAgICAgPHJlY3QgeD0iOCIgeT0iOCIgd2lkdGg9IjIwNCIgaGVpZ2h0PSIyNjgiIHJ4PSIxNCIgZmlsbD0iIzExMUMyMiIgc3Ryb2tlPSIjQjk4NTZFIiBzdHJva2Utd2lkdGg9IjIuNiIvPgogICAgICA8cmVjdCB4PSIxMiIgeT0iMTIiIHdp ...(+3532 chars)\",\"value\":\"6\"},{\"image\":\"data:image\\/svg+xml;base64,PHN2ZyB4bWxucz0iaHR0cDovL3d3dy53My5vcmcvMjAwMC9zdmciIHdpZHRoPSIyMjAiIGhlaWdodD0iMjg0IiB2aWV3Qm94PSIwIDAgMjIwIDI4NCIgcm9sZT0iaW1nIiA+Cjx0aXRsZT5IRVhBTE9DSyBtb2R1bGFyIGludGVyZmFjZSBhc3NldDwvdGl0bGU+CjxkZWZzPjwvZGVmcz4KICAgICAgPHJlY3QgeD0iOCIgeT0iOCIgd2lkdGg9IjIwNCIgaGVpZ2h0PSIyNjgiIHJ4PSIxNCIgZmlsbD0iIzExMUMyMiIgc3Ryb2tlPSIjQjk4NTZFIiBzdHJva2Utd2lkdGg9IjIuNiIvPgogICAgICA8cmVjdCB4PSIxMiIgeT0iMTIiIHdp ...(+3524 chars)\",\"value\":\"7\"},{\"image\":\"data:image\\/svg+xml;base64,PHN2ZyB4bWxucz0iaHR0cDovL3d3dy53My5vcmcvMjAwMC9zdmciIHdpZHRoPSIyMjAiIGhlaWdodD0iMjg0IiB2aWV3Qm94PSIwIDAgMjIwIDI4NCIgcm9sZT0iaW1nIiA+Cjx0aXRsZT5IRVhBTE9DSyBtb2R1bGFyIGludGVyZmFjZSBhc3NldDwvdGl0bGU+CjxkZWZzPjwvZGVmcz4KICAgICAgPHJlY3QgeD0iOCIgeT0iOCIgd2lkdGg9IjIwNCIgaGVpZ2h0PSIyNjgiIHJ4PSIxNCIgZmlsbD0iIzExMUMyMiIgc3Ryb2tlPSIjQjk4NTZFIiBzdHJva2Utd2lkdGg9IjIuNiIvPgogICAgICA8cmVjdCB4PSIxMiIgeT0iMTIiIHdp ...(+3532 chars)\",\"value\":\"8\"},{\"image\":\"data:image\\/svg+xml;base64,PHN2ZyB4bWxucz0iaHR0cDovL3d3dy53My5vcmcvMjAwMC9zdmciIHdpZHRoPSIyMjAiIGhlaWdodD0iMjg0IiB2aWV3Qm94PSIwIDAgMjIwIDI4NCIgcm9sZT0iaW1nIiA+Cjx0aXRsZT5IRVhBTE9DSyBtb2R1bGFyIGludGVyZmFjZSBhc3NldDwvdGl0bGU+CjxkZWZzPjwvZGVmcz4KICAgICAgPHJlY3QgeD0iOCIgeT0iOCIgd2lkdGg9IjIwNCIgaGVpZ2h0PSIyNjgiIHJ4PSIxNCIgZmlsbD0iIzExMUMyMiIgc3Ryb2tlPSIjQjk4NTZFIiBzdHJva2Utd2lkdGg9IjIuNiIvPgogICAgICA8cmVjdCB4PSIxMiIgeT0iMTIiIHdp ...(+3532 chars)\",\"value\":\"9\"},{\"image\":\"data:image\\/svg+xml;base64,PHN2ZyB4bWxucz0iaHR0cDovL3d3dy53My5vcmcvMjAwMC9zdmciIHdpZHRoPSIyMjAiIGhlaWdodD0iMjg0IiB2aWV3Qm94PSIwIDAgMjIwIDI4NCIgcm9sZT0iaW1nIiA+Cjx0aXRsZT5IRVhBTE9DSyBtb2R1bGFyIGludGVyZmFjZSBhc3NldDwvdGl0bGU+CjxkZWZzPjwvZGVmcz4KICAgICAgPHJlY3QgeD0iOCIgeT0iOCIgd2lkdGg9IjIwNCIgaGVpZ2h0PSIyNjgiIHJ4PSIxNCIgZmlsbD0iIzExMUMyMiIgc3Ryb2tlPSIjQjk4NTZFIiBzdHJva2Utd2lkdGg9IjIuNiIvPgogICAgICA8cmVjdCB4PSIxMiIgeT0iMTIiIHdp ...(+3532 chars)\",\"value\":\"10\"},{\"image\":\"data:image\\/svg+xml;base64,PHN2ZyB4bWxucz0iaHR0cDovL3d3dy53My5vcmcvMjAwMC9zdmciIHdpZHRoPSIyMjAiIGhlaWdodD0iMjg0IiB2aWV3Qm94PSIwIDAgMjIwIDI4NCIgcm9sZT0iaW1nIiA+Cjx0aXRsZT5IRVhBTE9DSyBtb2R1bGFyIGludGVyZmFjZSBhc3NldDwvdGl0bGU+CjxkZWZzPjwvZGVmcz4KICAgICAgPHJlY3QgeD0iOCIgeT0iOCIgd2lkdGg9IjIwNCIgaGVpZ2h0PSIyNjgiIHJ4PSIxNCIgZmlsbD0iIzExMUMyMiIgc3Ryb2tlPSIjNTM2NjZFIiBzdHJva2Utd2lkdGg9IjIiLz4KICAgICAgPHJlY3QgeD0iMTIiIHk9IjEyIiB3aWR0 ...(+3220 chars)\",\"value\":\"11\"},{\"image\":\"data:image\\/svg+xml;base64,PHN2ZyB4bWxucz0iaHR0cDovL3d3dy53My5vcmcvMjAwMC9zdmciIHdpZHRoPSIyMjAiIGhlaWdodD0iMjg0IiB2aWV3Qm94PSIwIDAgMjIwIDI4NCIgcm9sZT0iaW1nIiA+Cjx0aXRsZT5IRVhBTE9DSyBtb2R1bGFyIGludGVyZmFjZSBhc3NldDwvdGl0bGU+CjxkZWZzPjxsaW5lYXJHcmFkaWVudCBpZD0ia3JhZnRGcm9udCIgeDE9IjAiIHkxPSIwIiB4Mj0iMSIgeTI9IjEiPjxzdG9wIHN0b3AtY29sb3I9IiNEM0I5OUEiLz48c3RvcCBvZmZzZXQ9IjEiIHN0b3AtY29sb3I9IiNBMzgzNjMiLz48L2xpbmVhckdyYWRpZW50Pjxs ...(+4752 chars)\",\"value\":\"20\"},{\"image\":\"data:image\\/svg+xml;base64,PHN2ZyB4bWxucz0iaHR0cDovL3d3dy53My5vcmcvMjAwMC9zdmciIHdpZHRoPSIyMjAiIGhlaWdodD0iMjg0IiB2aWV3Qm94PSIwIDAgMjIwIDI4NCIgcm9sZT0iaW1nIiA+Cjx0aXRsZT5IRVhBTE9DSyBtb2R1bGFyIGludGVyZmFjZSBhc3NldDwvdGl0bGU+CjxkZWZzPjxsaW5lYXJHcmFkaWVudCBpZD0ia3JhZnRGcm9udCIgeDE9IjAiIHkxPSIwIiB4Mj0iMSIgeTI9IjEiPjxzdG9wIHN0b3AtY29sb3I9IiNEM0I5OUEiLz48c3RvcCBvZmZzZXQ9IjEiIHN0b3AtY29sb3I9IiNBMzgzNjMiLz48L2xpbmVhckdyYWRpZW50Pjxs ...(+7264 chars)\",\"value\":\"21\"},{\"image\":\"data:image\\/svg+xml;base64,PHN2ZyB4bWxucz0iaHR0cDovL3d3dy53My5vcmcvMjAwMC9zdmciIHdpZHRoPSIyMjAiIGhlaWdodD0iMjg0IiB2aWV3Qm94PSIwIDAgMjIwIDI4NCIgcm9sZT0iaW1nIiA+Cjx0aXRsZT5IRVhBTE9DSyBtb2R1bGFyIGludGVyZmFjZSBhc3NldDwvdGl0bGU+CjxkZWZzPjxsaW5lYXJHcmFkaWVudCBpZD0ia3JhZnRGcm9udCIgeDE9IjAiIHkxPSIwIiB4Mj0iMSIgeTI9IjEiPjxzdG9wIHN0b3AtY29sb3I9IiNEM0I5OUEiLz48c3RvcCBvZmZzZXQ9IjEiIHN0b3AtY29sb3I9IiNBMzgzNjMiLz48L2xpbmVhckdyYWRpZW50Pjxs ...(+7264 chars)\",\"value\":\"22\"},{\"image\":\"data:image\\/svg+xml;base64,PHN2ZyB4bWxucz0iaHR0cDovL3d3dy53My5vcmcvMjAwMC9zdmciIHdpZHRoPSIyMjAiIGhlaWdodD0iMjg0IiB2aWV3Qm94PSIwIDAgMjIwIDI4NCIgcm9sZT0iaW1nIiA+Cjx0aXRsZT5IRVhBTE9DSyBtb2R1bGFyIGludGVyZmFjZSBhc3NldDwvdGl0bGU+CjxkZWZzPjxsaW5lYXJHcmFkaWVudCBpZD0ia3JhZnRGcm9udCIgeDE9IjAiIHkxPSIwIiB4Mj0iMSIgeTI9IjEiPjxzdG9wIHN0b3AtY29sb3I9IiNEM0I5OUEiLz48c3RvcCBvZmZzZXQ9IjEiIHN0b3AtY29sb3I9IiNBMzgzNjMiLz48L2xpbmVhckdyYWRpZW50Pjxs ...(+7264 chars)\",\"value\":\"23\"},{\"image\":\"data:image\\/svg+xml;base64,PHN2ZyB4bWxucz0iaHR0cDovL3d3dy53My5vcmcvMjAwMC9zdmciIHdpZHRoPSIyMjAiIGhlaWdodD0iMjg0IiB2aWV3Qm94PSIwIDAgMjIwIDI4NCIgcm9sZT0iaW1nIiA+Cjx0aXRsZT5IRVhBTE9DSyBtb2R1bGFyIGludGVyZmFjZSBhc3NldDwvdGl0bGU+CjxkZWZzPjxsaW5lYXJHcmFkaWVudCBpZD0ia3JhZnRGcm9udCIgeDE9IjAiIHkxPSIwIiB4Mj0iMSIgeTI9IjEiPjxzdG9wIHN0b3AtY29sb3I9IiNEM0I5OUEiLz48c3RvcCBvZmZzZXQ9IjEiIHN0b3AtY29sb3I9IiNBMzgzNjMiLz48L2xpbmVhckdyYWRpZW50Pjxs ...(+7260 chars)\",\"value\":\"24\"},{\"image\":\"data:image\\/svg+xml;base64,PHN2ZyB4bWxucz0iaHR0cDovL3d3dy53My5vcmcvMjAwMC9zdmciIHdpZHRoPSIyMjAiIGhlaWdodD0iMjg0IiB2aWV3Qm94PSIwIDAgMjIwIDI4NCIgcm9sZT0iaW1nIiA+Cjx0aXRsZT5IRVhBTE9DSyBtb2R1bGFyIGludGVyZmFjZSBhc3NldDwvdGl0bGU+CjxkZWZzPjxsaW5lYXJHcmFkaWVudCBpZD0ia3JhZnRGcm9udCIgeDE9IjAiIHkxPSIwIiB4Mj0iMSIgeTI9IjEiPjxzdG9wIHN0b3AtY29sb3I9IiNEM0I5OUEiLz48c3RvcCBvZmZzZXQ9IjEiIHN0b3AtY29sb3I9IiNBMzgzNjMiLz48L2xpbmVhckdyYWRpZW50Pjxs ...(+7264 chars)\",\"value\":\"25\"},{\"image\":\"data:image\\/svg+xml;base64,PHN2ZyB4bWxucz0iaHR0cDovL3d3dy53My5vcmcvMjAwMC9zdmciIHdpZHRoPSIyMjAiIGhlaWdodD0iMjg0IiB2aWV3Qm94PSIwIDAgMjIwIDI4NCIgcm9sZT0iaW1nIiA+Cjx0aXRsZT5IRVhBTE9DSyBtb2R1bGFyIGludGVyZmFjZSBhc3NldDwvdGl0bGU+CjxkZWZzPjxsaW5lYXJHcmFkaWVudCBpZD0ia3JhZnRGcm9udCIgeDE9IjAiIHkxPSIwIiB4Mj0iMSIgeTI9IjEiPjxzdG9wIHN0b3AtY29sb3I9IiNEM0I5OUEiLz48c3RvcCBvZmZzZXQ9IjEiIHN0b3AtY29sb3I9IiNBMzgzNjMiLz48L2xpbmVhckdyYWRpZW50Pjxs ...(+7272 chars)\",\"value\":\"26\"},{\"image\":\"data:image\\/svg+xml;base64,PHN2ZyB4bWxucz0iaHR0cDovL3d3dy53My5vcmcvMjAwMC9zdmciIHdpZHRoPSIyMjAiIGhlaWdodD0iMjg0IiB2aWV3Qm94PSIwIDAgMjIwIDI4NCIgcm9sZT0iaW1nIiA+Cjx0aXRsZT5IRVhBTE9DSyBtb2R1bGFyIGludGVyZmFjZSBhc3NldDwvdGl0bGU+CjxkZWZzPjxsaW5lYXJHcmFkaWVudCBpZD0ia3JhZnRGcm9udCIgeDE9IjAiIHkxPSIwIiB4Mj0iMSIgeTI9IjEiPjxzdG9wIHN0b3AtY29sb3I9IiNEM0I5OUEiLz48c3RvcCBvZmZzZXQ9IjEiIHN0b3AtY29sb3I9IiNBMzgzNjMiLz48L2xpbmVhckdyYWRpZW50Pjxs ...(+7264 chars)\",\"value\":\"27\"},{\"image\":\"data:image\\/svg+xml;base64,PHN2ZyB4bWxucz0iaHR0cDovL3d3dy53My5vcmcvMjAwMC9zdmciIHdpZHRoPSIyMjAiIGhlaWdodD0iMjg0IiB2aWV3Qm94PSIwIDAgMjIwIDI4NCIgcm9sZT0iaW1nIiA+Cjx0aXRsZT5IRVhBTE9DSyBtb2R1bGFyIGludGVyZmFjZSBhc3NldDwvdGl0bGU+CjxkZWZzPjxsaW5lYXJHcmFkaWVudCBpZD0ia3JhZnRGcm9udCIgeDE9IjAiIHkxPSIwIiB4Mj0iMSIgeTI9IjEiPjxzdG9wIHN0b3AtY29sb3I9IiNEM0I5OUEiLz48c3RvcCBvZmZzZXQ9IjEiIHN0b3AtY29sb3I9IiNBMzgzNjMiLz48L2xpbmVhckdyYWRpZW50Pjxs ...(+7268 chars)\",\"value\":\"28\"},{\"image\":\"data:image\\/svg+xml;base64,PHN2ZyB4bWxucz0iaHR0cDovL3d3dy53My5vcmcvMjAwMC9zdmciIHdpZHRoPSIyMjAiIGhlaWdodD0iMjg0IiB2aWV3Qm94PSIwIDAgMjIwIDI4NCIgcm9sZT0iaW1nIiA+Cjx0aXRsZT5IRVhBTE9DSyBtb2R1bGFyIGludGVyZmFjZSBhc3NldDwvdGl0bGU+CjxkZWZzPjxsaW5lYXJHcmFkaWVudCBpZD0ia3JhZnRGcm9udCIgeDE9IjAiIHkxPSIwIiB4Mj0iMSIgeTI9IjEiPjxzdG9wIHN0b3AtY29sb3I9IiNEM0I5OUEiLz48c3RvcCBvZmZzZXQ9IjEiIHN0b3AtY29sb3I9IiNBMzgzNjMiLz48L2xpbmVhckdyYWRpZW50Pjxs ...(+7268 chars)\",\"value\":\"29\"},{\"image\":\"data:image\\/svg+xml;base64,PHN2ZyB4bWxucz0iaHR0cDovL3d3dy53My5vcmcvMjAwMC9zdmciIHdpZHRoPSIyMjAiIGhlaWdodD0iMjg0IiB2aWV3Qm94PSIwIDAgMjIwIDI4NCIgcm9sZT0iaW1nIiA+Cjx0aXRsZT5IRVhBTE9DSyBtb2R1bGFyIGludGVyZmFjZSBhc3NldDwvdGl0bGU+CjxkZWZzPjxsaW5lYXJHcmFkaWVudCBpZD0ia3JhZnRGcm9udCIgeDE9IjAiIHkxPSIwIiB4Mj0iMSIgeTI9IjEiPjxzdG9wIHN0b3AtY29sb3I9IiNEM0I5OUEiLz48c3RvcCBvZmZzZXQ9IjEiIHN0b3AtY29sb3I9IiNBMzgzNjMiLz48L2xpbmVhckdyYWRpZW50Pjxs ...(+7268 chars)\",\"value\":\"30\"},{\"image\":\"data:image\\/svg+xml;base64,PHN2ZyB4bWxucz0iaHR0cDovL3d3dy53My5vcmcvMjAwMC9zdmciIHdpZHRoPSIyMjAiIGhlaWdodD0iMjg0IiB2aWV3Qm94PSIwIDAgMjIwIDI4NCIgcm9sZT0iaW1nIiA+Cjx0aXRsZT5IRVhBTE9DSyBtb2R1bGFyIGludGVyZmFjZSBhc3NldDwvdGl0bGU+CjxkZWZzPjxsaW5lYXJHcmFkaWVudCBpZD0ia3JhZnRGcm9udCIgeDE9IjAiIHkxPSIwIiB4Mj0iMSIgeTI9IjEiPjxzdG9wIHN0b3AtY29sb3I9IiNEM0I5OUEiLz48c3RvcCBvZmZzZXQ9IjEiIHN0b3AtY29sb3I9IiNBMzgzNjMiLz48L2xpbmVhckdyYWRpZW50Pjxs ...(+4756 chars)\",\"value\":\"31\"},{\"image\":\"data:image\\/svg+xml;base64,PHN2ZyB4bWxucz0iaHR0cDovL3d3dy53My5vcmcvMjAwMC9zdmciIHdpZHRoPSIyMjAiIGhlaWdodD0iMjg0IiB2aWV3Qm94PSIwIDAgMjIwIDI4NCIgcm9sZT0iaW1nIiA+Cjx0aXRsZT5IRVhBTE9DSyBtb2R1bGFyIGludGVyZmFjZSBhc3NldDwvdGl0bGU+CjxkZWZzPjxsaW5lYXJHcmFkaWVudCBpZD0ia3JhZnRGcm9udCIgeDE9IjAiIHkxPSIwIiB4Mj0iMSIgeTI9IjEiPjxzdG9wIHN0b3AtY29sb3I9IiNEM0I5OUEiLz48c3RvcCBvZmZzZXQ9IjEiIHN0b3AtY29sb3I9IiNBMzgzNjMiLz48L2xpbmVhckdyYWRpZW50Pjxs ...(+4752 chars)\",\"value\":\"32\"},{\"image\":\"data:image\\/svg+xml;base64,PHN2ZyB4bWxucz0iaHR0cDovL3d3dy53My5vcmcvMjAwMC9zdmciIHdpZHRoPSIyMjAiIGhlaWdodD0iMjg0IiB2aWV3Qm94PSIwIDAgMjIwIDI4NCIgcm9sZT0iaW1nIiA+Cjx0aXRsZT5IRVhBTE9DSyBtb2R1bGFyIGludGVyZmFjZSBhc3NldDwvdGl0bGU+CjxkZWZzPjxsaW5lYXJHcmFkaWVudCBpZD0ia3JhZnRGcm9udCIgeDE9IjAiIHkxPSIwIiB4Mj0iMSIgeTI9IjEiPjxzdG9wIHN0b3AtY29sb3I9IiNEM0I5OUEiLz48c3RvcCBvZmZzZXQ9IjEiIHN0b3AtY29sb3I9IiNBMzgzNjMiLz48L2xpbmVhckdyYWRpZW50Pjxs ...(+6860 chars)\",\"value\":\"33\"},{\"image\":\"data:image\\/svg+xml;base64,PHN2ZyB4bWxucz0iaHR0cDovL3d3dy53My5vcmcvMjAwMC9zdmciIHdpZHRoPSIyMjAiIGhlaWdodD0iMjg0IiB2aWV3Qm94PSIwIDAgMjIwIDI4NCIgcm9sZT0iaW1nIiA+Cjx0aXRsZT5IRVhBTE9DSyBtb2R1bGFyIGludGVyZmFjZSBhc3NldDwvdGl0bGU+CjxkZWZzPjxsaW5lYXJHcmFkaWVudCBpZD0ia3JhZnRGcm9udCIgeDE9IjAiIHkxPSIwIiB4Mj0iMSIgeTI9IjEiPjxzdG9wIHN0b3AtY29sb3I9IiNEM0I5OUEiLz48c3RvcCBvZmZzZXQ9IjEiIHN0b3AtY29sb3I9IiNBMzgzNjMiLz48L2xpbmVhckdyYWRpZW50Pjxs ...(+6860 chars)\",\"value\":\"34\"},{\"image\":\"data:image\\/svg+xml;base64,PHN2ZyB4bWxucz0iaHR0cDovL3d3dy53My5vcmcvMjAwMC9zdmciIHdpZHRoPSIyMjAiIGhlaWdodD0iMjg0IiB2aWV3Qm94PSIwIDAgMjIwIDI4NCIgcm9sZT0iaW1nIiA+Cjx0aXRsZT5IRVhBTE9DSyBtb2R1bGFyIGludGVyZmFjZSBhc3NldDwvdGl0bGU+CjxkZWZzPjxsaW5lYXJHcmFkaWVudCBpZD0ia3JhZnRGcm9udCIgeDE9IjAiIHkxPSIwIiB4Mj0iMSIgeTI9IjEiPjxzdG9wIHN0b3AtY29sb3I9IiNEM0I5OUEiLz48c3RvcCBvZmZzZXQ9IjEiIHN0b3AtY29sb3I9IiNBMzgzNjMiLz48L2xpbmVhckdyYWRpZW50Pjxs ...(+6860 chars)\",\"value\":\"35\"},{\"image\":\"data:image\\/svg+xml;base64,PHN2ZyB4bWxucz0iaHR0cDovL3d3dy53My5vcmcvMjAwMC9zdmciIHdpZHRoPSIyMjAiIGhlaWdodD0iMjg0IiB2aWV3Qm94PSIwIDAgMjIwIDI4NCIgcm9sZT0iaW1nIiA+DQo8dGl0bGU+SEVYQUxPQ0sgbW9kdWxhciBpbnRlcmZhY2UgYXNzZXQ8L3RpdGxlPg0KPGRlZnM+PGxpbmVhckdyYWRpZW50IGlkPSJrcmFmdEZyb250IiB4MT0iMCIgeTE9IjAiIHgyPSIxIiB5Mj0iMSI+PHN0b3Agc3RvcC1jb2xvcj0iI0QzQjk5QSIvPjxzdG9wIG9mZnNldD0iMSIgc3RvcC1jb2xvcj0iI0EzODM2MyIvPjwvbGluZWFyR3JhZGllbnQ+ ...(+6912 chars)\",\"value\":\"36\"},{\"image\":\"data:image\\/svg+xml;base64,PHN2ZyB4bWxucz0iaHR0cDovL3d3dy53My5vcmcvMjAwMC9zdmciIHdpZHRoPSIyMjAiIGhlaWdodD0iMjg0IiB2aWV3Qm94PSIwIDAgMjIwIDI4NCIgcm9sZT0iaW1nIiA+DQo8dGl0bGU+SEVYQUxPQ0sgbW9kdWxhciBpbnRlcmZhY2UgYXNzZXQ8L3RpdGxlPg0KPGRlZnM+PGxpbmVhckdyYWRpZW50IGlkPSJrcmFmdEZyb250IiB4MT0iMCIgeTE9IjAiIHgyPSIxIiB5Mj0iMSI+PHN0b3Agc3RvcC1jb2xvcj0iI0QzQjk5QSIvPjxzdG9wIG9mZnNldD0iMSIgc3RvcC1jb2xvcj0iI0EzODM2MyIvPjwvbGluZWFyR3JhZGllbnQ+ ...(+6912 chars)\",\"value\":\"37\"},{\"image\":\"data:image\\/svg+xml;base64,PHN2ZyB4bWxucz0iaHR0cDovL3d3dy53My5vcmcvMjAwMC9zdmciIHdpZHRoPSIyMjAiIGhlaWdodD0iMjg0IiB2aWV3Qm94PSIwIDAgMjIwIDI4NCIgcm9sZT0iaW1nIiA+DQo8dGl0bGU+SEVYQUxPQ0sgbW9kdWxhciBpbnRlcmZhY2UgYXNzZXQ8L3RpdGxlPg0KPGRlZnM+PGxpbmVhckdyYWRpZW50IGlkPSJrcmFmdEZyb250IiB4MT0iMCIgeTE9IjAiIHgyPSIxIiB5Mj0iMSI+PHN0b3Agc3RvcC1jb2xvcj0iI0QzQjk5QSIvPjxzdG9wIG9mZnNldD0iMSIgc3RvcC1jb2xvcj0iI0EzODM2MyIvPjwvbGluZWFyR3JhZGllbnQ+ ...(+6912 chars)\",\"value\":\"38\"}],\"fixedAspectRatio\":\"on\"}},\"settings\":{\"BindingType\":\"signal\",\"backgroundColor\":[0,0,0],\"backgroundOffset\":0.14,\"backgroundOpacity\":1,\"blockOrientation\":\"Right\",\"fixedAspectRatio\":\"on\",\"showBackgroundColor\":false,\"value\":0,\"version\":\"R2026b\"},\"type\":\"MultistateImage\"}"
  MultiStateImage11 : CustomWebBlock  LabelPosition=Hide  ShowInitialText=on  Configuration="{\"components\":[{\"name\":\"BackgroundImageComponent\",\"settings\":{\"image\":{\"size\":[0,0],\"src\":\"default\",\"srcOrientation\":\"Right\"},\"position\":[0,0,1,1],\"scaleMode\":\"0\"}},{\"name\":\"MultistateImageStateComponent\",\"settings\":{\"applyDefaults\":true,\"position\":[0,0,1,1],\"states\":[{\"image\":{\"size\":[0.7746478873239436,1],\"src\":\"data:image\\/svg+xml;base64,PHN2ZyB4bWxucz0iaHR0cDovL3d3dy53My5vcmcvMjAwMC9zdmciIHdpZHRoPSIyMjAiIGhlaWdodD0iMjg0IiB2aWV3Qm94PSIwIDAgMjIwIDI4NCIgcm9sZT0iaW1nIiA+Cjx0aXRsZT5IRVhBTE9DSyBtb2R1bGFyIGludGVyZmFjZSBhc3NldDwvdGl0bGU+CjxkZWZzPjwvZGVmcz4KICAgICAgPHJlY3QgeD0iOCIgeT0iOCIgd2lkdGg9IjIwNCIgaGVpZ2h0PSIyNjgiIHJ4PSIxNCIgZmlsbD0iIzExMUMyMiIgc3Ryb2tlPSIjNTM2NjZFIiBzdHJva2Utd2lkdGg9IjIiLz4KICAgICAgPHJlY3QgeD0iMTIiIHk9IjEyIiB3aWR0 ...(+3224 chars)\",\"srcOrientation\":\"Right\"},\"position\":[0,0,1,1],\"value\":[]},{\"image\":{\"size\":[0,0],\"src\":\"data:image\\/svg+xml;base64,PHN2ZyB4bWxucz0iaHR0cDovL3d3dy53My5vcmcvMjAwMC9zdmciIHdpZHRoPSIyMjAiIGhlaWdodD0iMjg0IiB2aWV3Qm94PSIwIDAgMjIwIDI4NCIgcm9sZT0iaW1nIiA+Cjx0aXRsZT5IRVhBTE9DSyBtb2R1bGFyIGludGVyZmFjZSBhc3NldDwvdGl0bGU+CjxkZWZzPjwvZGVmcz4KICAgICAgPHJlY3QgeD0iOCIgeT0iOCIgd2lkdGg9IjIwNCIgaGVpZ2h0PSIyNjgiIHJ4PSIxNCIgZmlsbD0iIzExMUMyMiIgc3Ryb2tlPSIjNTM2NjZFIiBzdHJva2Utd2lkdGg9IjIiLz4KICAgICAgPHJlY3QgeD0iMTIiIHk9IjEyIiB3aWR0 ...(+3224 chars)\",\"srcOrientation\":\"Right\"},\"position\":[0,0,1,1],\"value\":\"0\"},{\"image\":{\"size\":[0,0],\"src\":\"data:image\\/svg+xml;base64,PHN2ZyB4bWxucz0iaHR0cDovL3d3dy53My5vcmcvMjAwMC9zdmciIHdpZHRoPSIyMjAiIGhlaWdodD0iMjg0IiB2aWV3Qm94PSIwIDAgMjIwIDI4NCIgcm9sZT0iaW1nIiA+Cjx0aXRsZT5IRVhBTE9DSyBtb2R1bGFyIGludGVyZmFjZSBhc3NldDwvdGl0bGU+CjxkZWZzPjwvZGVmcz4KICAgICAgPHJlY3QgeD0iOCIgeT0iOCIgd2lkdGg9IjIwNCIgaGVpZ2h0PSIyNjgiIHJ4PSIxNCIgZmlsbD0iIzExMUMyMiIgc3Ryb2tlPSIjNTM2NjZFIiBzdHJva2Utd2lkdGg9IjIiLz4KICAgICAgPHJlY3QgeD0iMTIiIHk9IjEyIiB3aWR0 ...(+3220 chars)\",\"srcOrientation\":\"Right\"},\"position\":[0,0,1,1],\"value\":\"1\"},{\"image\":{\"size\":[0,0],\"src\":\"data:image\\/svg+xml;base64,PHN2ZyB4bWxucz0iaHR0cDovL3d3dy53My5vcmcvMjAwMC9zdmciIHdpZHRoPSIyMjAiIGhlaWdodD0iMjg0IiB2aWV3Qm94PSIwIDAgMjIwIDI4NCIgcm9sZT0iaW1nIiA+Cjx0aXRsZT5IRVhBTE9DSyBtb2R1bGFyIGludGVyZmFjZSBhc3NldDwvdGl0bGU+CjxkZWZzPjwvZGVmcz4KICAgICAgPHJlY3QgeD0iOCIgeT0iOCIgd2lkdGg9IjIwNCIgaGVpZ2h0PSIyNjgiIHJ4PSIxNCIgZmlsbD0iIzExMUMyMiIgc3Ryb2tlPSIjQjk4NTZFIiBzdHJva2Utd2lkdGg9IjIuNiIvPgogICAgICA8cmVjdCB4PSIxMiIgeT0iMTIiIHdp ...(+3488 chars)\",\"srcOrientation\":\"Right\"},\"position\":[0,0,1,1],\"value\":\"2\"},{\"image\":{\"size\":[0,0],\"src\":\"data:image\\/svg+xml;base64,PHN2ZyB4bWxucz0iaHR0cDovL3d3dy53My5vcmcvMjAwMC9zdmciIHdpZHRoPSIyMjAiIGhlaWdodD0iMjg0IiB2aWV3Qm94PSIwIDAgMjIwIDI4NCIgcm9sZT0iaW1nIiA+Cjx0aXRsZT5IRVhBTE9DSyBtb2R1bGFyIGludGVyZmFjZSBhc3NldDwvdGl0bGU+CjxkZWZzPjwvZGVmcz4KICAgICAgPHJlY3QgeD0iOCIgeT0iOCIgd2lkdGg9IjIwNCIgaGVpZ2h0PSIyNjgiIHJ4PSIxNCIgZmlsbD0iIzExMUMyMiIgc3Ryb2tlPSIjQjk4NTZFIiBzdHJva2Utd2lkdGg9IjIuNiIvPgogICAgICA8cmVjdCB4PSIxMiIgeT0iMTIiIHdp ...(+3484 chars)\",\"srcOrientation\":\"Right\"},\"position\":[0,0,1,1],\"value\":\"3\"},{\"image\":{\"size\":[0,0],\"src\":\"data:image\\/svg+xml;base64,PHN2ZyB4bWxucz0iaHR0cDovL3d3dy53My5vcmcvMjAwMC9zdmciIHdpZHRoPSIyMjAiIGhlaWdodD0iMjg0IiB2aWV3Qm94PSIwIDAgMjIwIDI4NCIgcm9sZT0iaW1nIiA+Cjx0aXRsZT5IRVhBTE9DSyBtb2R1bGFyIGludGVyZmFjZSBhc3NldDwvdGl0bGU+CjxkZWZzPjwvZGVmcz4KICAgICAgPHJlY3QgeD0iOCIgeT0iOCIgd2lkdGg9IjIwNCIgaGVpZ2h0PSIyNjgiIHJ4PSIxNCIgZmlsbD0iIzExMUMyMiIgc3Ryb2tlPSIjQjk4NTZFIiBzdHJva2Utd2lkdGg9IjIuNiIvPgogICAgICA8cmVjdCB4PSIxMiIgeT0iMTIiIHdp ...(+3532 chars)\",\"srcOrientation\":\"Right\"},\"position\":[0,0,1,1],\"value\":\"4\"},{\"image\":{\"size\":[0,0],\"src\":\"data:image\\/svg+xml;base64,PHN2ZyB4bWxucz0iaHR0cDovL3d3dy53My5vcmcvMjAwMC9zdmciIHdpZHRoPSIyMjAiIGhlaWdodD0iMjg0IiB2aWV3Qm94PSIwIDAgMjIwIDI4NCIgcm9sZT0iaW1nIiA+Cjx0aXRsZT5IRVhBTE9DSyBtb2R1bGFyIGludGVyZmFjZSBhc3NldDwvdGl0bGU+CjxkZWZzPjwvZGVmcz4KICAgICAgPHJlY3QgeD0iOCIgeT0iOCIgd2lkdGg9IjIwNCIgaGVpZ2h0PSIyNjgiIHJ4PSIxNCIgZmlsbD0iIzExMUMyMiIgc3Ryb2tlPSIjQjk4NTZFIiBzdHJva2Utd2lkdGg9IjIuNiIvPgogICAgICA8cmVjdCB4PSIxMiIgeT0iMTIiIHdp ...(+3532 chars)\",\"srcOrientation\":\"Right\"},\"position\":[0,0,1,1],\"value\":\"5\"},{\"image\":{\"size\":[0,0],\"src\":\"data:image\\/svg+xml;base64,PHN2ZyB4bWxucz0iaHR0cDovL3d3dy53My5vcmcvMjAwMC9zdmciIHdpZHRoPSIyMjAiIGhlaWdodD0iMjg0IiB2aWV3Qm94PSIwIDAgMjIwIDI4NCIgcm9sZT0iaW1nIiA+Cjx0aXRsZT5IRVhBTE9DSyBtb2R1bGFyIGludGVyZmFjZSBhc3NldDwvdGl0bGU+CjxkZWZzPjwvZGVmcz4KICAgICAgPHJlY3QgeD0iOCIgeT0iOCIgd2lkdGg9IjIwNCIgaGVpZ2h0PSIyNjgiIHJ4PSIxNCIgZmlsbD0iIzExMUMyMiIgc3Ryb2tlPSIjQjk4NTZFIiBzdHJva2Utd2lkdGg9IjIuNiIvPgogICAgICA8cmVjdCB4PSIxMiIgeT0iMTIiIHdp ...(+3532 chars)\",\"srcOrientation\":\"Right\"},\"position\":[0,0,1,1],\"value\":\"6\"},{\"image\":{\"size\":[0,0],\"src\":\"data:image\\/svg+xml;base64,PHN2ZyB4bWxucz0iaHR0cDovL3d3dy53My5vcmcvMjAwMC9zdmciIHdpZHRoPSIyMjAiIGhlaWdodD0iMjg0IiB2aWV3Qm94PSIwIDAgMjIwIDI4NCIgcm9sZT0iaW1nIiA+Cjx0aXRsZT5IRVhBTE9DSyBtb2R1bGFyIGludGVyZmFjZSBhc3NldDwvdGl0bGU+CjxkZWZzPjwvZGVmcz4KICAgICAgPHJlY3QgeD0iOCIgeT0iOCIgd2lkdGg9IjIwNCIgaGVpZ2h0PSIyNjgiIHJ4PSIxNCIgZmlsbD0iIzExMUMyMiIgc3Ryb2tlPSIjQjk4NTZFIiBzdHJva2Utd2lkdGg9IjIuNiIvPgogICAgICA8cmVjdCB4PSIxMiIgeT0iMTIiIHdp ...(+3524 chars)\",\"srcOrientation\":\"Right\"},\"position\":[0,0,1,1],\"value\":\"7\"},{\"image\":{\"size\":[0,0],\"src\":\"data:image\\/svg+xml;base64,PHN2ZyB4bWxucz0iaHR0cDovL3d3dy53My5vcmcvMjAwMC9zdmciIHdpZHRoPSIyMjAiIGhlaWdodD0iMjg0IiB2aWV3Qm94PSIwIDAgMjIwIDI4NCIgcm9sZT0iaW1nIiA+Cjx0aXRsZT5IRVhBTE9DSyBtb2R1bGFyIGludGVyZmFjZSBhc3NldDwvdGl0bGU+CjxkZWZzPjwvZGVmcz4KICAgICAgPHJlY3QgeD0iOCIgeT0iOCIgd2lkdGg9IjIwNCIgaGVpZ2h0PSIyNjgiIHJ4PSIxNCIgZmlsbD0iIzExMUMyMiIgc3Ryb2tlPSIjQjk4NTZFIiBzdHJva2Utd2lkdGg9IjIuNiIvPgogICAgICA8cmVjdCB4PSIxMiIgeT0iMTIiIHdp ...(+3532 chars)\",\"srcOrientation\":\"Right\"},\"position\":[0,0,1,1],\"value\":\"8\"},{\"image\":{\"size\":[0,0],\"src\":\"data:image\\/svg+xml;base64,PHN2ZyB4bWxucz0iaHR0cDovL3d3dy53My5vcmcvMjAwMC9zdmciIHdpZHRoPSIyMjAiIGhlaWdodD0iMjg0IiB2aWV3Qm94PSIwIDAgMjIwIDI4NCIgcm9sZT0iaW1nIiA+Cjx0aXRsZT5IRVhBTE9DSyBtb2R1bGFyIGludGVyZmFjZSBhc3NldDwvdGl0bGU+CjxkZWZzPjwvZGVmcz4KICAgICAgPHJlY3QgeD0iOCIgeT0iOCIgd2lkdGg9IjIwNCIgaGVpZ2h0PSIyNjgiIHJ4PSIxNCIgZmlsbD0iIzExMUMyMiIgc3Ryb2tlPSIjQjk4NTZFIiBzdHJva2Utd2lkdGg9IjIuNiIvPgogICAgICA8cmVjdCB4PSIxMiIgeT0iMTIiIHdp ...(+3532 chars)\",\"srcOrientation\":\"Right\"},\"position\":[0,0,1,1],\"value\":\"9\"},{\"image\":{\"size\":[0,0],\"src\":\"data:image\\/svg+xml;base64,PHN2ZyB4bWxucz0iaHR0cDovL3d3dy53My5vcmcvMjAwMC9zdmciIHdpZHRoPSIyMjAiIGhlaWdodD0iMjg0IiB2aWV3Qm94PSIwIDAgMjIwIDI4NCIgcm9sZT0iaW1nIiA+Cjx0aXRsZT5IRVhBTE9DSyBtb2R1bGFyIGludGVyZmFjZSBhc3NldDwvdGl0bGU+CjxkZWZzPjwvZGVmcz4KICAgICAgPHJlY3QgeD0iOCIgeT0iOCIgd2lkdGg9IjIwNCIgaGVpZ2h0PSIyNjgiIHJ4PSIxNCIgZmlsbD0iIzExMUMyMiIgc3Ryb2tlPSIjQjk4NTZFIiBzdHJva2Utd2lkdGg9IjIuNiIvPgogICAgICA8cmVjdCB4PSIxMiIgeT0iMTIiIHdp ...(+3532 chars)\",\"srcOrientation\":\"Right\"},\"position\":[0,0,1,1],\"value\":\"10\"},{\"image\":{\"size\":[0,0],\"src\":\"data:image\\/svg+xml;base64,PHN2ZyB4bWxucz0iaHR0cDovL3d3dy53My5vcmcvMjAwMC9zdmciIHdpZHRoPSIyMjAiIGhlaWdodD0iMjg0IiB2aWV3Qm94PSIwIDAgMjIwIDI4NCIgcm9sZT0iaW1nIiA+Cjx0aXRsZT5IRVhBTE9DSyBtb2R1bGFyIGludGVyZmFjZSBhc3NldDwvdGl0bGU+CjxkZWZzPjwvZGVmcz4KICAgICAgPHJlY3QgeD0iOCIgeT0iOCIgd2lkdGg9IjIwNCIgaGVpZ2h0PSIyNjgiIHJ4PSIxNCIgZmlsbD0iIzExMUMyMiIgc3Ryb2tlPSIjNTM2NjZFIiBzdHJva2Utd2lkdGg9IjIiLz4KICAgICAgPHJlY3QgeD0iMTIiIHk9IjEyIiB3aWR0 ...(+3220 chars)\",\"srcOrientation\":\"Right\"},\"position\":[0,0,1,1],\"value\":\"11\"},{\"image\":{\"size\":[0,0],\"src\":\"data:image\\/svg+xml;base64,PHN2ZyB4bWxucz0iaHR0cDovL3d3dy53My5vcmcvMjAwMC9zdmciIHdpZHRoPSIyMjAiIGhlaWdodD0iMjg0IiB2aWV3Qm94PSIwIDAgMjIwIDI4NCIgcm9sZT0iaW1nIiA+Cjx0aXRsZT5IRVhBTE9DSyBtb2R1bGFyIGludGVyZmFjZSBhc3NldDwvdGl0bGU+CjxkZWZzPjxsaW5lYXJHcmFkaWVudCBpZD0ia3JhZnRGcm9udCIgeDE9IjAiIHkxPSIwIiB4Mj0iMSIgeTI9IjEiPjxzdG9wIHN0b3AtY29sb3I9IiNEM0I5OUEiLz48c3RvcCBvZmZzZXQ9IjEiIHN0b3AtY29sb3I9IiNBMzgzNjMiLz48L2xpbmVhckdyYWRpZW50Pjxs ...(+4752 chars)\",\"srcOrientation\":\"Right\"},\"position\":[0,0,1,1],\"value\":\"20\"},{\"image\":{\"size\":[0,0],\"src\":\"data:image\\/svg+xml;base64,PHN2ZyB4bWxucz0iaHR0cDovL3d3dy53My5vcmcvMjAwMC9zdmciIHdpZHRoPSIyMjAiIGhlaWdodD0iMjg0IiB2aWV3Qm94PSIwIDAgMjIwIDI4NCIgcm9sZT0iaW1nIiA+Cjx0aXRsZT5IRVhBTE9DSyBtb2R1bGFyIGludGVyZmFjZSBhc3NldDwvdGl0bGU+CjxkZWZzPjxsaW5lYXJHcmFkaWVudCBpZD0ia3JhZnRGcm9udCIgeDE9IjAiIHkxPSIwIiB4Mj0iMSIgeTI9IjEiPjxzdG9wIHN0b3AtY29sb3I9IiNEM0I5OUEiLz48c3RvcCBvZmZzZXQ9IjEiIHN0b3AtY29sb3I9IiNBMzgzNjMiLz48L2xpbmVhckdyYWRpZW50Pjxs ...(+7264 chars)\",\"srcOrientation\":\"Right\"},\"position\":[0,0,1,1],\"value\":\"21\"},{\"image\":{\"size\":[0,0],\"src\":\"data:image\\/svg+xml;base64,PHN2ZyB4bWxucz0iaHR0cDovL3d3dy53My5vcmcvMjAwMC9zdmciIHdpZHRoPSIyMjAiIGhlaWdodD0iMjg0IiB2aWV3Qm94PSIwIDAgMjIwIDI4NCIgcm9sZT0iaW1nIiA+Cjx0aXRsZT5IRVhBTE9DSyBtb2R1bGFyIGludGVyZmFjZSBhc3NldDwvdGl0bGU+CjxkZWZzPjxsaW5lYXJHcmFkaWVudCBpZD0ia3JhZnRGcm9udCIgeDE9IjAiIHkxPSIwIiB4Mj0iMSIgeTI9IjEiPjxzdG9wIHN0b3AtY29sb3I9IiNEM0I5OUEiLz48c3RvcCBvZmZzZXQ9IjEiIHN0b3AtY29sb3I9IiNBMzgzNjMiLz48L2xpbmVhckdyYWRpZW50Pjxs ...(+7264 chars)\",\"srcOrientation\":\"Right\"},\"position\":[0,0,1,1],\"value\":\"22\"},{\"image\":{\"size\":[0,0],\"src\":\"data:image\\/svg+xml;base64,PHN2ZyB4bWxucz0iaHR0cDovL3d3dy53My5vcmcvMjAwMC9zdmciIHdpZHRoPSIyMjAiIGhlaWdodD0iMjg0IiB2aWV3Qm94PSIwIDAgMjIwIDI4NCIgcm9sZT0iaW1nIiA+Cjx0aXRsZT5IRVhBTE9DSyBtb2R1bGFyIGludGVyZmFjZSBhc3NldDwvdGl0bGU+CjxkZWZzPjxsaW5lYXJHcmFkaWVudCBpZD0ia3JhZnRGcm9udCIgeDE9IjAiIHkxPSIwIiB4Mj0iMSIgeTI9IjEiPjxzdG9wIHN0b3AtY29sb3I9IiNEM0I5OUEiLz48c3RvcCBvZmZzZXQ9IjEiIHN0b3AtY29sb3I9IiNBMzgzNjMiLz48L2xpbmVhckdyYWRpZW50Pjxs ...(+7264 chars)\",\"srcOrientation\":\"Right\"},\"position\":[0,0,1,1],\"value\":\"23\"},{\"image\":{\"size\":[0,0],\"src\":\"data:image\\/svg+xml;base64,PHN2ZyB4bWxucz0iaHR0cDovL3d3dy53My5vcmcvMjAwMC9zdmciIHdpZHRoPSIyMjAiIGhlaWdodD0iMjg0IiB2aWV3Qm94PSIwIDAgMjIwIDI4NCIgcm9sZT0iaW1nIiA+Cjx0aXRsZT5IRVhBTE9DSyBtb2R1bGFyIGludGVyZmFjZSBhc3NldDwvdGl0bGU+CjxkZWZzPjxsaW5lYXJHcmFkaWVudCBpZD0ia3JhZnRGcm9udCIgeDE9IjAiIHkxPSIwIiB4Mj0iMSIgeTI9IjEiPjxzdG9wIHN0b3AtY29sb3I9IiNEM0I5OUEiLz48c3RvcCBvZmZzZXQ9IjEiIHN0b3AtY29sb3I9IiNBMzgzNjMiLz48L2xpbmVhckdyYWRpZW50Pjxs ...(+7260 chars)\",\"srcOrientation\":\"Right\"},\"position\":[0,0,1,1],\"value\":\"24\"},{\"image\":{\"size\":[0,0],\"src\":\"data:image\\/svg+xml;base64,PHN2ZyB4bWxucz0iaHR0cDovL3d3dy53My5vcmcvMjAwMC9zdmciIHdpZHRoPSIyMjAiIGhlaWdodD0iMjg0IiB2aWV3Qm94PSIwIDAgMjIwIDI4NCIgcm9sZT0iaW1nIiA+Cjx0aXRsZT5IRVhBTE9DSyBtb2R1bGFyIGludGVyZmFjZSBhc3NldDwvdGl0bGU+CjxkZWZzPjxsaW5lYXJHcmFkaWVudCBpZD0ia3JhZnRGcm9udCIgeDE9IjAiIHkxPSIwIiB4Mj0iMSIgeTI9IjEiPjxzdG9wIHN0b3AtY29sb3I9IiNEM0I5OUEiLz48c3RvcCBvZmZzZXQ9IjEiIHN0b3AtY29sb3I9IiNBMzgzNjMiLz48L2xpbmVhckdyYWRpZW50Pjxs ...(+7264 chars)\",\"srcOrientation\":\"Right\"},\"position\":[0,0,1,1],\"value\":\"25\"},{\"image\":{\"size\":[0,0],\"src\":\"data:image\\/svg+xml;base64,PHN2ZyB4bWxucz0iaHR0cDovL3d3dy53My5vcmcvMjAwMC9zdmciIHdpZHRoPSIyMjAiIGhlaWdodD0iMjg0IiB2aWV3Qm94PSIwIDAgMjIwIDI4NCIgcm9sZT0iaW1nIiA+Cjx0aXRsZT5IRVhBTE9DSyBtb2R1bGFyIGludGVyZmFjZSBhc3NldDwvdGl0bGU+CjxkZWZzPjxsaW5lYXJHcmFkaWVudCBpZD0ia3JhZnRGcm9udCIgeDE9IjAiIHkxPSIwIiB4Mj0iMSIgeTI9IjEiPjxzdG9wIHN0b3AtY29sb3I9IiNEM0I5OUEiLz48c3RvcCBvZmZzZXQ9IjEiIHN0b3AtY29sb3I9IiNBMzgzNjMiLz48L2xpbmVhckdyYWRpZW50Pjxs ...(+7272 chars)\",\"srcOrientation\":\"Right\"},\"position\":[0,0,1,1],\"value\":\"26\"},{\"image\":{\"size\":[0,0],\"src\":\"data:image\\/svg+xml;base64,PHN2ZyB4bWxucz0iaHR0cDovL3d3dy53My5vcmcvMjAwMC9zdmciIHdpZHRoPSIyMjAiIGhlaWdodD0iMjg0IiB2aWV3Qm94PSIwIDAgMjIwIDI4NCIgcm9sZT0iaW1nIiA+Cjx0aXRsZT5IRVhBTE9DSyBtb2R1bGFyIGludGVyZmFjZSBhc3NldDwvdGl0bGU+CjxkZWZzPjxsaW5lYXJHcmFkaWVudCBpZD0ia3JhZnRGcm9udCIgeDE9IjAiIHkxPSIwIiB4Mj0iMSIgeTI9IjEiPjxzdG9wIHN0b3AtY29sb3I9IiNEM0I5OUEiLz48c3RvcCBvZmZzZXQ9IjEiIHN0b3AtY29sb3I9IiNBMzgzNjMiLz48L2xpbmVhckdyYWRpZW50Pjxs ...(+7264 chars)\",\"srcOrientation\":\"Right\"},\"position\":[0,0,1,1],\"value\":\"27\"},{\"image\":{\"size\":[0,0],\"src\":\"data:image\\/svg+xml;base64,PHN2ZyB4bWxucz0iaHR0cDovL3d3dy53My5vcmcvMjAwMC9zdmciIHdpZHRoPSIyMjAiIGhlaWdodD0iMjg0IiB2aWV3Qm94PSIwIDAgMjIwIDI4NCIgcm9sZT0iaW1nIiA+Cjx0aXRsZT5IRVhBTE9DSyBtb2R1bGFyIGludGVyZmFjZSBhc3NldDwvdGl0bGU+CjxkZWZzPjxsaW5lYXJHcmFkaWVudCBpZD0ia3JhZnRGcm9udCIgeDE9IjAiIHkxPSIwIiB4Mj0iMSIgeTI9IjEiPjxzdG9wIHN0b3AtY29sb3I9IiNEM0I5OUEiLz48c3RvcCBvZmZzZXQ9IjEiIHN0b3AtY29sb3I9IiNBMzgzNjMiLz48L2xpbmVhckdyYWRpZW50Pjxs ...(+7268 chars)\",\"srcOrientation\":\"Right\"},\"position\":[0,0,1,1],\"value\":\"28\"},{\"image\":{\"size\":[0,0],\"src\":\"data:image\\/svg+xml;base64,PHN2ZyB4bWxucz0iaHR0cDovL3d3dy53My5vcmcvMjAwMC9zdmciIHdpZHRoPSIyMjAiIGhlaWdodD0iMjg0IiB2aWV3Qm94PSIwIDAgMjIwIDI4NCIgcm9sZT0iaW1nIiA+Cjx0aXRsZT5IRVhBTE9DSyBtb2R1bGFyIGludGVyZmFjZSBhc3NldDwvdGl0bGU+CjxkZWZzPjxsaW5lYXJHcmFkaWVudCBpZD0ia3JhZnRGcm9udCIgeDE9IjAiIHkxPSIwIiB4Mj0iMSIgeTI9IjEiPjxzdG9wIHN0b3AtY29sb3I9IiNEM0I5OUEiLz48c3RvcCBvZmZzZXQ9IjEiIHN0b3AtY29sb3I9IiNBMzgzNjMiLz48L2xpbmVhckdyYWRpZW50Pjxs ...(+7268 chars)\",\"srcOrientation\":\"Right\"},\"position\":[0,0,1,1],\"value\":\"29\"},{\"image\":{\"size\":[0,0],\"src\":\"data:image\\/svg+xml;base64,PHN2ZyB4bWxucz0iaHR0cDovL3d3dy53My5vcmcvMjAwMC9zdmciIHdpZHRoPSIyMjAiIGhlaWdodD0iMjg0IiB2aWV3Qm94PSIwIDAgMjIwIDI4NCIgcm9sZT0iaW1nIiA+Cjx0aXRsZT5IRVhBTE9DSyBtb2R1bGFyIGludGVyZmFjZSBhc3NldDwvdGl0bGU+CjxkZWZzPjxsaW5lYXJHcmFkaWVudCBpZD0ia3JhZnRGcm9udCIgeDE9IjAiIHkxPSIwIiB4Mj0iMSIgeTI9IjEiPjxzdG9wIHN0b3AtY29sb3I9IiNEM0I5OUEiLz48c3RvcCBvZmZzZXQ9IjEiIHN0b3AtY29sb3I9IiNBMzgzNjMiLz48L2xpbmVhckdyYWRpZW50Pjxs ...(+7268 chars)\",\"srcOrientation\":\"Right\"},\"position\":[0,0,1,1],\"value\":\"30\"},{\"image\":{\"size\":[0,0],\"src\":\"data:image\\/svg+xml;base64,PHN2ZyB4bWxucz0iaHR0cDovL3d3dy53My5vcmcvMjAwMC9zdmciIHdpZHRoPSIyMjAiIGhlaWdodD0iMjg0IiB2aWV3Qm94PSIwIDAgMjIwIDI4NCIgcm9sZT0iaW1nIiA+Cjx0aXRsZT5IRVhBTE9DSyBtb2R1bGFyIGludGVyZmFjZSBhc3NldDwvdGl0bGU+CjxkZWZzPjxsaW5lYXJHcmFkaWVudCBpZD0ia3JhZnRGcm9udCIgeDE9IjAiIHkxPSIwIiB4Mj0iMSIgeTI9IjEiPjxzdG9wIHN0b3AtY29sb3I9IiNEM0I5OUEiLz48c3RvcCBvZmZzZXQ9IjEiIHN0b3AtY29sb3I9IiNBMzgzNjMiLz48L2xpbmVhckdyYWRpZW50Pjxs ...(+4756 chars)\",\"srcOrientation\":\"Right\"},\"position\":[0,0,1,1],\"value\":\"31\"},{\"image\":{\"size\":[0,0],\"src\":\"data:image\\/svg+xml;base64,PHN2ZyB4bWxucz0iaHR0cDovL3d3dy53My5vcmcvMjAwMC9zdmciIHdpZHRoPSIyMjAiIGhlaWdodD0iMjg0IiB2aWV3Qm94PSIwIDAgMjIwIDI4NCIgcm9sZT0iaW1nIiA+Cjx0aXRsZT5IRVhBTE9DSyBtb2R1bGFyIGludGVyZmFjZSBhc3NldDwvdGl0bGU+CjxkZWZzPjxsaW5lYXJHcmFkaWVudCBpZD0ia3JhZnRGcm9udCIgeDE9IjAiIHkxPSIwIiB4Mj0iMSIgeTI9IjEiPjxzdG9wIHN0b3AtY29sb3I9IiNEM0I5OUEiLz48c3RvcCBvZmZzZXQ9IjEiIHN0b3AtY29sb3I9IiNBMzgzNjMiLz48L2xpbmVhckdyYWRpZW50Pjxs ...(+4752 chars)\",\"srcOrientation\":\"Right\"},\"position\":[0,0,1,1],\"value\":\"32\"},{\"image\":{\"size\":[0,0],\"src\":\"data:image\\/svg+xml;base64,PHN2ZyB4bWxucz0iaHR0cDovL3d3dy53My5vcmcvMjAwMC9zdmciIHdpZHRoPSIyMjAiIGhlaWdodD0iMjg0IiB2aWV3Qm94PSIwIDAgMjIwIDI4NCIgcm9sZT0iaW1nIiA+Cjx0aXRsZT5IRVhBTE9DSyBtb2R1bGFyIGludGVyZmFjZSBhc3NldDwvdGl0bGU+CjxkZWZzPjxsaW5lYXJHcmFkaWVudCBpZD0ia3JhZnRGcm9udCIgeDE9IjAiIHkxPSIwIiB4Mj0iMSIgeTI9IjEiPjxzdG9wIHN0b3AtY29sb3I9IiNEM0I5OUEiLz48c3RvcCBvZmZzZXQ9IjEiIHN0b3AtY29sb3I9IiNBMzgzNjMiLz48L2xpbmVhckdyYWRpZW50Pjxs ...(+6860 chars)\",\"srcOrientation\":\"Right\"},\"position\":[0,0,1,1],\"value\":\"33\"},{\"image\":{\"size\":[0,0],\"src\":\"data:image\\/svg+xml;base64,PHN2ZyB4bWxucz0iaHR0cDovL3d3dy53My5vcmcvMjAwMC9zdmciIHdpZHRoPSIyMjAiIGhlaWdodD0iMjg0IiB2aWV3Qm94PSIwIDAgMjIwIDI4NCIgcm9sZT0iaW1nIiA+Cjx0aXRsZT5IRVhBTE9DSyBtb2R1bGFyIGludGVyZmFjZSBhc3NldDwvdGl0bGU+CjxkZWZzPjxsaW5lYXJHcmFkaWVudCBpZD0ia3JhZnRGcm9udCIgeDE9IjAiIHkxPSIwIiB4Mj0iMSIgeTI9IjEiPjxzdG9wIHN0b3AtY29sb3I9IiNEM0I5OUEiLz48c3RvcCBvZmZzZXQ9IjEiIHN0b3AtY29sb3I9IiNBMzgzNjMiLz48L2xpbmVhckdyYWRpZW50Pjxs ...(+6860 chars)\",\"srcOrientation\":\"Right\"},\"position\":[0,0,1,1],\"value\":\"34\"},{\"image\":{\"size\":[0,0],\"src\":\"data:image\\/svg+xml;base64,PHN2ZyB4bWxucz0iaHR0cDovL3d3dy53My5vcmcvMjAwMC9zdmciIHdpZHRoPSIyMjAiIGhlaWdodD0iMjg0IiB2aWV3Qm94PSIwIDAgMjIwIDI4NCIgcm9sZT0iaW1nIiA+Cjx0aXRsZT5IRVhBTE9DSyBtb2R1bGFyIGludGVyZmFjZSBhc3NldDwvdGl0bGU+CjxkZWZzPjxsaW5lYXJHcmFkaWVudCBpZD0ia3JhZnRGcm9udCIgeDE9IjAiIHkxPSIwIiB4Mj0iMSIgeTI9IjEiPjxzdG9wIHN0b3AtY29sb3I9IiNEM0I5OUEiLz48c3RvcCBvZmZzZXQ9IjEiIHN0b3AtY29sb3I9IiNBMzgzNjMiLz48L2xpbmVhckdyYWRpZW50Pjxs ...(+6860 chars)\",\"srcOrientation\":\"Right\"},\"position\":[0,0,1,1],\"value\":\"35\"},{\"image\":{\"size\":[0,0],\"src\":\"data:image\\/svg+xml;base64,PHN2ZyB4bWxucz0iaHR0cDovL3d3dy53My5vcmcvMjAwMC9zdmciIHdpZHRoPSIyMjAiIGhlaWdodD0iMjg0IiB2aWV3Qm94PSIwIDAgMjIwIDI4NCIgcm9sZT0iaW1nIiA+DQo8dGl0bGU+SEVYQUxPQ0sgbW9kdWxhciBpbnRlcmZhY2UgYXNzZXQ8L3RpdGxlPg0KPGRlZnM+PGxpbmVhckdyYWRpZW50IGlkPSJrcmFmdEZyb250IiB4MT0iMCIgeTE9IjAiIHgyPSIxIiB5Mj0iMSI+PHN0b3Agc3RvcC1jb2xvcj0iI0QzQjk5QSIvPjxzdG9wIG9mZnNldD0iMSIgc3RvcC1jb2xvcj0iI0EzODM2MyIvPjwvbGluZWFyR3JhZGllbnQ+ ...(+6912 chars)\",\"srcOrientation\":\"Right\"},\"position\":[0,0,1,1],\"value\":\"36\"},{\"image\":{\"size\":[0,0],\"src\":\"data:image\\/svg+xml;base64,PHN2ZyB4bWxucz0iaHR0cDovL3d3dy53My5vcmcvMjAwMC9zdmciIHdpZHRoPSIyMjAiIGhlaWdodD0iMjg0IiB2aWV3Qm94PSIwIDAgMjIwIDI4NCIgcm9sZT0iaW1nIiA+DQo8dGl0bGU+SEVYQUxPQ0sgbW9kdWxhciBpbnRlcmZhY2UgYXNzZXQ8L3RpdGxlPg0KPGRlZnM+PGxpbmVhckdyYWRpZW50IGlkPSJrcmFmdEZyb250IiB4MT0iMCIgeTE9IjAiIHgyPSIxIiB5Mj0iMSI+PHN0b3Agc3RvcC1jb2xvcj0iI0QzQjk5QSIvPjxzdG9wIG9mZnNldD0iMSIgc3RvcC1jb2xvcj0iI0EzODM2MyIvPjwvbGluZWFyR3JhZGllbnQ+ ...(+6912 chars)\",\"srcOrientation\":\"Right\"},\"position\":[0,0,1,1],\"value\":\"37\"},{\"image\":{\"size\":[0,0],\"src\":\"data:image\\/svg+xml;base64,PHN2ZyB4bWxucz0iaHR0cDovL3d3dy53My5vcmcvMjAwMC9zdmciIHdpZHRoPSIyMjAiIGhlaWdodD0iMjg0IiB2aWV3Qm94PSIwIDAgMjIwIDI4NCIgcm9sZT0iaW1nIiA+DQo8dGl0bGU+SEVYQUxPQ0sgbW9kdWxhciBpbnRlcmZhY2UgYXNzZXQ8L3RpdGxlPg0KPGRlZnM+PGxpbmVhckdyYWRpZW50IGlkPSJrcmFmdEZyb250IiB4MT0iMCIgeTE9IjAiIHgyPSIxIiB5Mj0iMSI+PHN0b3Agc3RvcC1jb2xvcj0iI0QzQjk5QSIvPjxzdG9wIG9mZnNldD0iMSIgc3RvcC1jb2xvcj0iI0EzODM2MyIvPjwvbGluZWFyR3JhZGllbnQ+ ...(+6912 chars)\",\"srcOrientation\":\"Right\"},\"position\":[0,0,1,1],\"value\":\"38\"}],\"valueType\":\"discrete\"}},{\"name\":\"ForegroundImageComponent\",\"settings\":{\"image\":{\"size\":[0,0],\"src\":\"default\",\"srcOrientation\":\"Right\"},\"isForeground\":1,\"position\":[0,0,1,1],\"scaleMode\":\"0\"}}],\"derived\":{\"blockParameters\":{\"DefaultImage\":\"data:image\\/svg+xml;base64,PHN2ZyB4bWxucz0iaHR0cDovL3d3dy53My5vcmcvMjAwMC9zdmciIHdpZHRoPSIyMjAiIGhlaWdodD0iMjg0IiB2aWV3Qm94PSIwIDAgMjIwIDI4NCIgcm9sZT0iaW1nIiA+Cjx0aXRsZT5IRVhBTE9DSyBtb2R1bGFyIGludGVyZmFjZSBhc3NldDwvdGl0bGU+CjxkZWZzPjwvZGVmcz4KICAgICAgPHJlY3QgeD0iOCIgeT0iOCIgd2lkdGg9IjIwNCIgaGVpZ2h0PSIyNjgiIHJ4PSIxNCIgZmlsbD0iIzExMUMyMiIgc3Ryb2tlPSIjNTM2NjZFIiBzdHJva2Utd2lkdGg9IjIiLz4KICAgICAgPHJlY3QgeD0iMTIiIHk9IjEyIiB3aWR0 ...(+3224 chars)\",\"StateValueType\":\"discrete\",\"States\":[{\"image\":\"data:image\\/svg+xml;base64,PHN2ZyB4bWxucz0iaHR0cDovL3d3dy53My5vcmcvMjAwMC9zdmciIHdpZHRoPSIyMjAiIGhlaWdodD0iMjg0IiB2aWV3Qm94PSIwIDAgMjIwIDI4NCIgcm9sZT0iaW1nIiA+Cjx0aXRsZT5IRVhBTE9DSyBtb2R1bGFyIGludGVyZmFjZSBhc3NldDwvdGl0bGU+CjxkZWZzPjwvZGVmcz4KICAgICAgPHJlY3QgeD0iOCIgeT0iOCIgd2lkdGg9IjIwNCIgaGVpZ2h0PSIyNjgiIHJ4PSIxNCIgZmlsbD0iIzExMUMyMiIgc3Ryb2tlPSIjNTM2NjZFIiBzdHJva2Utd2lkdGg9IjIiLz4KICAgICAgPHJlY3QgeD0iMTIiIHk9IjEyIiB3aWR0 ...(+3224 chars)\",\"value\":\"0\"},{\"image\":\"data:image\\/svg+xml;base64,PHN2ZyB4bWxucz0iaHR0cDovL3d3dy53My5vcmcvMjAwMC9zdmciIHdpZHRoPSIyMjAiIGhlaWdodD0iMjg0IiB2aWV3Qm94PSIwIDAgMjIwIDI4NCIgcm9sZT0iaW1nIiA+Cjx0aXRsZT5IRVhBTE9DSyBtb2R1bGFyIGludGVyZmFjZSBhc3NldDwvdGl0bGU+CjxkZWZzPjwvZGVmcz4KICAgICAgPHJlY3QgeD0iOCIgeT0iOCIgd2lkdGg9IjIwNCIgaGVpZ2h0PSIyNjgiIHJ4PSIxNCIgZmlsbD0iIzExMUMyMiIgc3Ryb2tlPSIjNTM2NjZFIiBzdHJva2Utd2lkdGg9IjIiLz4KICAgICAgPHJlY3QgeD0iMTIiIHk9IjEyIiB3aWR0 ...(+3220 chars)\",\"value\":\"1\"},{\"image\":\"data:image\\/svg+xml;base64,PHN2ZyB4bWxucz0iaHR0cDovL3d3dy53My5vcmcvMjAwMC9zdmciIHdpZHRoPSIyMjAiIGhlaWdodD0iMjg0IiB2aWV3Qm94PSIwIDAgMjIwIDI4NCIgcm9sZT0iaW1nIiA+Cjx0aXRsZT5IRVhBTE9DSyBtb2R1bGFyIGludGVyZmFjZSBhc3NldDwvdGl0bGU+CjxkZWZzPjwvZGVmcz4KICAgICAgPHJlY3QgeD0iOCIgeT0iOCIgd2lkdGg9IjIwNCIgaGVpZ2h0PSIyNjgiIHJ4PSIxNCIgZmlsbD0iIzExMUMyMiIgc3Ryb2tlPSIjQjk4NTZFIiBzdHJva2Utd2lkdGg9IjIuNiIvPgogICAgICA8cmVjdCB4PSIxMiIgeT0iMTIiIHdp ...(+3488 chars)\",\"value\":\"2\"},{\"image\":\"data:image\\/svg+xml;base64,PHN2ZyB4bWxucz0iaHR0cDovL3d3dy53My5vcmcvMjAwMC9zdmciIHdpZHRoPSIyMjAiIGhlaWdodD0iMjg0IiB2aWV3Qm94PSIwIDAgMjIwIDI4NCIgcm9sZT0iaW1nIiA+Cjx0aXRsZT5IRVhBTE9DSyBtb2R1bGFyIGludGVyZmFjZSBhc3NldDwvdGl0bGU+CjxkZWZzPjwvZGVmcz4KICAgICAgPHJlY3QgeD0iOCIgeT0iOCIgd2lkdGg9IjIwNCIgaGVpZ2h0PSIyNjgiIHJ4PSIxNCIgZmlsbD0iIzExMUMyMiIgc3Ryb2tlPSIjQjk4NTZFIiBzdHJva2Utd2lkdGg9IjIuNiIvPgogICAgICA8cmVjdCB4PSIxMiIgeT0iMTIiIHdp ...(+3484 chars)\",\"value\":\"3\"},{\"image\":\"data:image\\/svg+xml;base64,PHN2ZyB4bWxucz0iaHR0cDovL3d3dy53My5vcmcvMjAwMC9zdmciIHdpZHRoPSIyMjAiIGhlaWdodD0iMjg0IiB2aWV3Qm94PSIwIDAgMjIwIDI4NCIgcm9sZT0iaW1nIiA+Cjx0aXRsZT5IRVhBTE9DSyBtb2R1bGFyIGludGVyZmFjZSBhc3NldDwvdGl0bGU+CjxkZWZzPjwvZGVmcz4KICAgICAgPHJlY3QgeD0iOCIgeT0iOCIgd2lkdGg9IjIwNCIgaGVpZ2h0PSIyNjgiIHJ4PSIxNCIgZmlsbD0iIzExMUMyMiIgc3Ryb2tlPSIjQjk4NTZFIiBzdHJva2Utd2lkdGg9IjIuNiIvPgogICAgICA8cmVjdCB4PSIxMiIgeT0iMTIiIHdp ...(+3532 chars)\",\"value\":\"4\"},{\"image\":\"data:image\\/svg+xml;base64,PHN2ZyB4bWxucz0iaHR0cDovL3d3dy53My5vcmcvMjAwMC9zdmciIHdpZHRoPSIyMjAiIGhlaWdodD0iMjg0IiB2aWV3Qm94PSIwIDAgMjIwIDI4NCIgcm9sZT0iaW1nIiA+Cjx0aXRsZT5IRVhBTE9DSyBtb2R1bGFyIGludGVyZmFjZSBhc3NldDwvdGl0bGU+CjxkZWZzPjwvZGVmcz4KICAgICAgPHJlY3QgeD0iOCIgeT0iOCIgd2lkdGg9IjIwNCIgaGVpZ2h0PSIyNjgiIHJ4PSIxNCIgZmlsbD0iIzExMUMyMiIgc3Ryb2tlPSIjQjk4NTZFIiBzdHJva2Utd2lkdGg9IjIuNiIvPgogICAgICA8cmVjdCB4PSIxMiIgeT0iMTIiIHdp ...(+3532 chars)\",\"value\":\"5\"},{\"image\":\"data:image\\/svg+xml;base64,PHN2ZyB4bWxucz0iaHR0cDovL3d3dy53My5vcmcvMjAwMC9zdmciIHdpZHRoPSIyMjAiIGhlaWdodD0iMjg0IiB2aWV3Qm94PSIwIDAgMjIwIDI4NCIgcm9sZT0iaW1nIiA+Cjx0aXRsZT5IRVhBTE9DSyBtb2R1bGFyIGludGVyZmFjZSBhc3NldDwvdGl0bGU+CjxkZWZzPjwvZGVmcz4KICAgICAgPHJlY3QgeD0iOCIgeT0iOCIgd2lkdGg9IjIwNCIgaGVpZ2h0PSIyNjgiIHJ4PSIxNCIgZmlsbD0iIzExMUMyMiIgc3Ryb2tlPSIjQjk4NTZFIiBzdHJva2Utd2lkdGg9IjIuNiIvPgogICAgICA8cmVjdCB4PSIxMiIgeT0iMTIiIHdp ...(+3532 chars)\",\"value\":\"6\"},{\"image\":\"data:image\\/svg+xml;base64,PHN2ZyB4bWxucz0iaHR0cDovL3d3dy53My5vcmcvMjAwMC9zdmciIHdpZHRoPSIyMjAiIGhlaWdodD0iMjg0IiB2aWV3Qm94PSIwIDAgMjIwIDI4NCIgcm9sZT0iaW1nIiA+Cjx0aXRsZT5IRVhBTE9DSyBtb2R1bGFyIGludGVyZmFjZSBhc3NldDwvdGl0bGU+CjxkZWZzPjwvZGVmcz4KICAgICAgPHJlY3QgeD0iOCIgeT0iOCIgd2lkdGg9IjIwNCIgaGVpZ2h0PSIyNjgiIHJ4PSIxNCIgZmlsbD0iIzExMUMyMiIgc3Ryb2tlPSIjQjk4NTZFIiBzdHJva2Utd2lkdGg9IjIuNiIvPgogICAgICA8cmVjdCB4PSIxMiIgeT0iMTIiIHdp ...(+3524 chars)\",\"value\":\"7\"},{\"image\":\"data:image\\/svg+xml;base64,PHN2ZyB4bWxucz0iaHR0cDovL3d3dy53My5vcmcvMjAwMC9zdmciIHdpZHRoPSIyMjAiIGhlaWdodD0iMjg0IiB2aWV3Qm94PSIwIDAgMjIwIDI4NCIgcm9sZT0iaW1nIiA+Cjx0aXRsZT5IRVhBTE9DSyBtb2R1bGFyIGludGVyZmFjZSBhc3NldDwvdGl0bGU+CjxkZWZzPjwvZGVmcz4KICAgICAgPHJlY3QgeD0iOCIgeT0iOCIgd2lkdGg9IjIwNCIgaGVpZ2h0PSIyNjgiIHJ4PSIxNCIgZmlsbD0iIzExMUMyMiIgc3Ryb2tlPSIjQjk4NTZFIiBzdHJva2Utd2lkdGg9IjIuNiIvPgogICAgICA8cmVjdCB4PSIxMiIgeT0iMTIiIHdp ...(+3532 chars)\",\"value\":\"8\"},{\"image\":\"data:image\\/svg+xml;base64,PHN2ZyB4bWxucz0iaHR0cDovL3d3dy53My5vcmcvMjAwMC9zdmciIHdpZHRoPSIyMjAiIGhlaWdodD0iMjg0IiB2aWV3Qm94PSIwIDAgMjIwIDI4NCIgcm9sZT0iaW1nIiA+Cjx0aXRsZT5IRVhBTE9DSyBtb2R1bGFyIGludGVyZmFjZSBhc3NldDwvdGl0bGU+CjxkZWZzPjwvZGVmcz4KICAgICAgPHJlY3QgeD0iOCIgeT0iOCIgd2lkdGg9IjIwNCIgaGVpZ2h0PSIyNjgiIHJ4PSIxNCIgZmlsbD0iIzExMUMyMiIgc3Ryb2tlPSIjQjk4NTZFIiBzdHJva2Utd2lkdGg9IjIuNiIvPgogICAgICA8cmVjdCB4PSIxMiIgeT0iMTIiIHdp ...(+3532 chars)\",\"value\":\"9\"},{\"image\":\"data:image\\/svg+xml;base64,PHN2ZyB4bWxucz0iaHR0cDovL3d3dy53My5vcmcvMjAwMC9zdmciIHdpZHRoPSIyMjAiIGhlaWdodD0iMjg0IiB2aWV3Qm94PSIwIDAgMjIwIDI4NCIgcm9sZT0iaW1nIiA+Cjx0aXRsZT5IRVhBTE9DSyBtb2R1bGFyIGludGVyZmFjZSBhc3NldDwvdGl0bGU+CjxkZWZzPjwvZGVmcz4KICAgICAgPHJlY3QgeD0iOCIgeT0iOCIgd2lkdGg9IjIwNCIgaGVpZ2h0PSIyNjgiIHJ4PSIxNCIgZmlsbD0iIzExMUMyMiIgc3Ryb2tlPSIjQjk4NTZFIiBzdHJva2Utd2lkdGg9IjIuNiIvPgogICAgICA8cmVjdCB4PSIxMiIgeT0iMTIiIHdp ...(+3532 chars)\",\"value\":\"10\"},{\"image\":\"data:image\\/svg+xml;base64,PHN2ZyB4bWxucz0iaHR0cDovL3d3dy53My5vcmcvMjAwMC9zdmciIHdpZHRoPSIyMjAiIGhlaWdodD0iMjg0IiB2aWV3Qm94PSIwIDAgMjIwIDI4NCIgcm9sZT0iaW1nIiA+Cjx0aXRsZT5IRVhBTE9DSyBtb2R1bGFyIGludGVyZmFjZSBhc3NldDwvdGl0bGU+CjxkZWZzPjwvZGVmcz4KICAgICAgPHJlY3QgeD0iOCIgeT0iOCIgd2lkdGg9IjIwNCIgaGVpZ2h0PSIyNjgiIHJ4PSIxNCIgZmlsbD0iIzExMUMyMiIgc3Ryb2tlPSIjNTM2NjZFIiBzdHJva2Utd2lkdGg9IjIiLz4KICAgICAgPHJlY3QgeD0iMTIiIHk9IjEyIiB3aWR0 ...(+3220 chars)\",\"value\":\"11\"},{\"image\":\"data:image\\/svg+xml;base64,PHN2ZyB4bWxucz0iaHR0cDovL3d3dy53My5vcmcvMjAwMC9zdmciIHdpZHRoPSIyMjAiIGhlaWdodD0iMjg0IiB2aWV3Qm94PSIwIDAgMjIwIDI4NCIgcm9sZT0iaW1nIiA+Cjx0aXRsZT5IRVhBTE9DSyBtb2R1bGFyIGludGVyZmFjZSBhc3NldDwvdGl0bGU+CjxkZWZzPjxsaW5lYXJHcmFkaWVudCBpZD0ia3JhZnRGcm9udCIgeDE9IjAiIHkxPSIwIiB4Mj0iMSIgeTI9IjEiPjxzdG9wIHN0b3AtY29sb3I9IiNEM0I5OUEiLz48c3RvcCBvZmZzZXQ9IjEiIHN0b3AtY29sb3I9IiNBMzgzNjMiLz48L2xpbmVhckdyYWRpZW50Pjxs ...(+4752 chars)\",\"value\":\"20\"},{\"image\":\"data:image\\/svg+xml;base64,PHN2ZyB4bWxucz0iaHR0cDovL3d3dy53My5vcmcvMjAwMC9zdmciIHdpZHRoPSIyMjAiIGhlaWdodD0iMjg0IiB2aWV3Qm94PSIwIDAgMjIwIDI4NCIgcm9sZT0iaW1nIiA+Cjx0aXRsZT5IRVhBTE9DSyBtb2R1bGFyIGludGVyZmFjZSBhc3NldDwvdGl0bGU+CjxkZWZzPjxsaW5lYXJHcmFkaWVudCBpZD0ia3JhZnRGcm9udCIgeDE9IjAiIHkxPSIwIiB4Mj0iMSIgeTI9IjEiPjxzdG9wIHN0b3AtY29sb3I9IiNEM0I5OUEiLz48c3RvcCBvZmZzZXQ9IjEiIHN0b3AtY29sb3I9IiNBMzgzNjMiLz48L2xpbmVhckdyYWRpZW50Pjxs ...(+7264 chars)\",\"value\":\"21\"},{\"image\":\"data:image\\/svg+xml;base64,PHN2ZyB4bWxucz0iaHR0cDovL3d3dy53My5vcmcvMjAwMC9zdmciIHdpZHRoPSIyMjAiIGhlaWdodD0iMjg0IiB2aWV3Qm94PSIwIDAgMjIwIDI4NCIgcm9sZT0iaW1nIiA+Cjx0aXRsZT5IRVhBTE9DSyBtb2R1bGFyIGludGVyZmFjZSBhc3NldDwvdGl0bGU+CjxkZWZzPjxsaW5lYXJHcmFkaWVudCBpZD0ia3JhZnRGcm9udCIgeDE9IjAiIHkxPSIwIiB4Mj0iMSIgeTI9IjEiPjxzdG9wIHN0b3AtY29sb3I9IiNEM0I5OUEiLz48c3RvcCBvZmZzZXQ9IjEiIHN0b3AtY29sb3I9IiNBMzgzNjMiLz48L2xpbmVhckdyYWRpZW50Pjxs ...(+7264 chars)\",\"value\":\"22\"},{\"image\":\"data:image\\/svg+xml;base64,PHN2ZyB4bWxucz0iaHR0cDovL3d3dy53My5vcmcvMjAwMC9zdmciIHdpZHRoPSIyMjAiIGhlaWdodD0iMjg0IiB2aWV3Qm94PSIwIDAgMjIwIDI4NCIgcm9sZT0iaW1nIiA+Cjx0aXRsZT5IRVhBTE9DSyBtb2R1bGFyIGludGVyZmFjZSBhc3NldDwvdGl0bGU+CjxkZWZzPjxsaW5lYXJHcmFkaWVudCBpZD0ia3JhZnRGcm9udCIgeDE9IjAiIHkxPSIwIiB4Mj0iMSIgeTI9IjEiPjxzdG9wIHN0b3AtY29sb3I9IiNEM0I5OUEiLz48c3RvcCBvZmZzZXQ9IjEiIHN0b3AtY29sb3I9IiNBMzgzNjMiLz48L2xpbmVhckdyYWRpZW50Pjxs ...(+7264 chars)\",\"value\":\"23\"},{\"image\":\"data:image\\/svg+xml;base64,PHN2ZyB4bWxucz0iaHR0cDovL3d3dy53My5vcmcvMjAwMC9zdmciIHdpZHRoPSIyMjAiIGhlaWdodD0iMjg0IiB2aWV3Qm94PSIwIDAgMjIwIDI4NCIgcm9sZT0iaW1nIiA+Cjx0aXRsZT5IRVhBTE9DSyBtb2R1bGFyIGludGVyZmFjZSBhc3NldDwvdGl0bGU+CjxkZWZzPjxsaW5lYXJHcmFkaWVudCBpZD0ia3JhZnRGcm9udCIgeDE9IjAiIHkxPSIwIiB4Mj0iMSIgeTI9IjEiPjxzdG9wIHN0b3AtY29sb3I9IiNEM0I5OUEiLz48c3RvcCBvZmZzZXQ9IjEiIHN0b3AtY29sb3I9IiNBMzgzNjMiLz48L2xpbmVhckdyYWRpZW50Pjxs ...(+7260 chars)\",\"value\":\"24\"},{\"image\":\"data:image\\/svg+xml;base64,PHN2ZyB4bWxucz0iaHR0cDovL3d3dy53My5vcmcvMjAwMC9zdmciIHdpZHRoPSIyMjAiIGhlaWdodD0iMjg0IiB2aWV3Qm94PSIwIDAgMjIwIDI4NCIgcm9sZT0iaW1nIiA+Cjx0aXRsZT5IRVhBTE9DSyBtb2R1bGFyIGludGVyZmFjZSBhc3NldDwvdGl0bGU+CjxkZWZzPjxsaW5lYXJHcmFkaWVudCBpZD0ia3JhZnRGcm9udCIgeDE9IjAiIHkxPSIwIiB4Mj0iMSIgeTI9IjEiPjxzdG9wIHN0b3AtY29sb3I9IiNEM0I5OUEiLz48c3RvcCBvZmZzZXQ9IjEiIHN0b3AtY29sb3I9IiNBMzgzNjMiLz48L2xpbmVhckdyYWRpZW50Pjxs ...(+7264 chars)\",\"value\":\"25\"},{\"image\":\"data:image\\/svg+xml;base64,PHN2ZyB4bWxucz0iaHR0cDovL3d3dy53My5vcmcvMjAwMC9zdmciIHdpZHRoPSIyMjAiIGhlaWdodD0iMjg0IiB2aWV3Qm94PSIwIDAgMjIwIDI4NCIgcm9sZT0iaW1nIiA+Cjx0aXRsZT5IRVhBTE9DSyBtb2R1bGFyIGludGVyZmFjZSBhc3NldDwvdGl0bGU+CjxkZWZzPjxsaW5lYXJHcmFkaWVudCBpZD0ia3JhZnRGcm9udCIgeDE9IjAiIHkxPSIwIiB4Mj0iMSIgeTI9IjEiPjxzdG9wIHN0b3AtY29sb3I9IiNEM0I5OUEiLz48c3RvcCBvZmZzZXQ9IjEiIHN0b3AtY29sb3I9IiNBMzgzNjMiLz48L2xpbmVhckdyYWRpZW50Pjxs ...(+7272 chars)\",\"value\":\"26\"},{\"image\":\"data:image\\/svg+xml;base64,PHN2ZyB4bWxucz0iaHR0cDovL3d3dy53My5vcmcvMjAwMC9zdmciIHdpZHRoPSIyMjAiIGhlaWdodD0iMjg0IiB2aWV3Qm94PSIwIDAgMjIwIDI4NCIgcm9sZT0iaW1nIiA+Cjx0aXRsZT5IRVhBTE9DSyBtb2R1bGFyIGludGVyZmFjZSBhc3NldDwvdGl0bGU+CjxkZWZzPjxsaW5lYXJHcmFkaWVudCBpZD0ia3JhZnRGcm9udCIgeDE9IjAiIHkxPSIwIiB4Mj0iMSIgeTI9IjEiPjxzdG9wIHN0b3AtY29sb3I9IiNEM0I5OUEiLz48c3RvcCBvZmZzZXQ9IjEiIHN0b3AtY29sb3I9IiNBMzgzNjMiLz48L2xpbmVhckdyYWRpZW50Pjxs ...(+7264 chars)\",\"value\":\"27\"},{\"image\":\"data:image\\/svg+xml;base64,PHN2ZyB4bWxucz0iaHR0cDovL3d3dy53My5vcmcvMjAwMC9zdmciIHdpZHRoPSIyMjAiIGhlaWdodD0iMjg0IiB2aWV3Qm94PSIwIDAgMjIwIDI4NCIgcm9sZT0iaW1nIiA+Cjx0aXRsZT5IRVhBTE9DSyBtb2R1bGFyIGludGVyZmFjZSBhc3NldDwvdGl0bGU+CjxkZWZzPjxsaW5lYXJHcmFkaWVudCBpZD0ia3JhZnRGcm9udCIgeDE9IjAiIHkxPSIwIiB4Mj0iMSIgeTI9IjEiPjxzdG9wIHN0b3AtY29sb3I9IiNEM0I5OUEiLz48c3RvcCBvZmZzZXQ9IjEiIHN0b3AtY29sb3I9IiNBMzgzNjMiLz48L2xpbmVhckdyYWRpZW50Pjxs ...(+7268 chars)\",\"value\":\"28\"},{\"image\":\"data:image\\/svg+xml;base64,PHN2ZyB4bWxucz0iaHR0cDovL3d3dy53My5vcmcvMjAwMC9zdmciIHdpZHRoPSIyMjAiIGhlaWdodD0iMjg0IiB2aWV3Qm94PSIwIDAgMjIwIDI4NCIgcm9sZT0iaW1nIiA+Cjx0aXRsZT5IRVhBTE9DSyBtb2R1bGFyIGludGVyZmFjZSBhc3NldDwvdGl0bGU+CjxkZWZzPjxsaW5lYXJHcmFkaWVudCBpZD0ia3JhZnRGcm9udCIgeDE9IjAiIHkxPSIwIiB4Mj0iMSIgeTI9IjEiPjxzdG9wIHN0b3AtY29sb3I9IiNEM0I5OUEiLz48c3RvcCBvZmZzZXQ9IjEiIHN0b3AtY29sb3I9IiNBMzgzNjMiLz48L2xpbmVhckdyYWRpZW50Pjxs ...(+7268 chars)\",\"value\":\"29\"},{\"image\":\"data:image\\/svg+xml;base64,PHN2ZyB4bWxucz0iaHR0cDovL3d3dy53My5vcmcvMjAwMC9zdmciIHdpZHRoPSIyMjAiIGhlaWdodD0iMjg0IiB2aWV3Qm94PSIwIDAgMjIwIDI4NCIgcm9sZT0iaW1nIiA+Cjx0aXRsZT5IRVhBTE9DSyBtb2R1bGFyIGludGVyZmFjZSBhc3NldDwvdGl0bGU+CjxkZWZzPjxsaW5lYXJHcmFkaWVudCBpZD0ia3JhZnRGcm9udCIgeDE9IjAiIHkxPSIwIiB4Mj0iMSIgeTI9IjEiPjxzdG9wIHN0b3AtY29sb3I9IiNEM0I5OUEiLz48c3RvcCBvZmZzZXQ9IjEiIHN0b3AtY29sb3I9IiNBMzgzNjMiLz48L2xpbmVhckdyYWRpZW50Pjxs ...(+7268 chars)\",\"value\":\"30\"},{\"image\":\"data:image\\/svg+xml;base64,PHN2ZyB4bWxucz0iaHR0cDovL3d3dy53My5vcmcvMjAwMC9zdmciIHdpZHRoPSIyMjAiIGhlaWdodD0iMjg0IiB2aWV3Qm94PSIwIDAgMjIwIDI4NCIgcm9sZT0iaW1nIiA+Cjx0aXRsZT5IRVhBTE9DSyBtb2R1bGFyIGludGVyZmFjZSBhc3NldDwvdGl0bGU+CjxkZWZzPjxsaW5lYXJHcmFkaWVudCBpZD0ia3JhZnRGcm9udCIgeDE9IjAiIHkxPSIwIiB4Mj0iMSIgeTI9IjEiPjxzdG9wIHN0b3AtY29sb3I9IiNEM0I5OUEiLz48c3RvcCBvZmZzZXQ9IjEiIHN0b3AtY29sb3I9IiNBMzgzNjMiLz48L2xpbmVhckdyYWRpZW50Pjxs ...(+4756 chars)\",\"value\":\"31\"},{\"image\":\"data:image\\/svg+xml;base64,PHN2ZyB4bWxucz0iaHR0cDovL3d3dy53My5vcmcvMjAwMC9zdmciIHdpZHRoPSIyMjAiIGhlaWdodD0iMjg0IiB2aWV3Qm94PSIwIDAgMjIwIDI4NCIgcm9sZT0iaW1nIiA+Cjx0aXRsZT5IRVhBTE9DSyBtb2R1bGFyIGludGVyZmFjZSBhc3NldDwvdGl0bGU+CjxkZWZzPjxsaW5lYXJHcmFkaWVudCBpZD0ia3JhZnRGcm9udCIgeDE9IjAiIHkxPSIwIiB4Mj0iMSIgeTI9IjEiPjxzdG9wIHN0b3AtY29sb3I9IiNEM0I5OUEiLz48c3RvcCBvZmZzZXQ9IjEiIHN0b3AtY29sb3I9IiNBMzgzNjMiLz48L2xpbmVhckdyYWRpZW50Pjxs ...(+4752 chars)\",\"value\":\"32\"},{\"image\":\"data:image\\/svg+xml;base64,PHN2ZyB4bWxucz0iaHR0cDovL3d3dy53My5vcmcvMjAwMC9zdmciIHdpZHRoPSIyMjAiIGhlaWdodD0iMjg0IiB2aWV3Qm94PSIwIDAgMjIwIDI4NCIgcm9sZT0iaW1nIiA+Cjx0aXRsZT5IRVhBTE9DSyBtb2R1bGFyIGludGVyZmFjZSBhc3NldDwvdGl0bGU+CjxkZWZzPjxsaW5lYXJHcmFkaWVudCBpZD0ia3JhZnRGcm9udCIgeDE9IjAiIHkxPSIwIiB4Mj0iMSIgeTI9IjEiPjxzdG9wIHN0b3AtY29sb3I9IiNEM0I5OUEiLz48c3RvcCBvZmZzZXQ9IjEiIHN0b3AtY29sb3I9IiNBMzgzNjMiLz48L2xpbmVhckdyYWRpZW50Pjxs ...(+6860 chars)\",\"value\":\"33\"},{\"image\":\"data:image\\/svg+xml;base64,PHN2ZyB4bWxucz0iaHR0cDovL3d3dy53My5vcmcvMjAwMC9zdmciIHdpZHRoPSIyMjAiIGhlaWdodD0iMjg0IiB2aWV3Qm94PSIwIDAgMjIwIDI4NCIgcm9sZT0iaW1nIiA+Cjx0aXRsZT5IRVhBTE9DSyBtb2R1bGFyIGludGVyZmFjZSBhc3NldDwvdGl0bGU+CjxkZWZzPjxsaW5lYXJHcmFkaWVudCBpZD0ia3JhZnRGcm9udCIgeDE9IjAiIHkxPSIwIiB4Mj0iMSIgeTI9IjEiPjxzdG9wIHN0b3AtY29sb3I9IiNEM0I5OUEiLz48c3RvcCBvZmZzZXQ9IjEiIHN0b3AtY29sb3I9IiNBMzgzNjMiLz48L2xpbmVhckdyYWRpZW50Pjxs ...(+6860 chars)\",\"value\":\"34\"},{\"image\":\"data:image\\/svg+xml;base64,PHN2ZyB4bWxucz0iaHR0cDovL3d3dy53My5vcmcvMjAwMC9zdmciIHdpZHRoPSIyMjAiIGhlaWdodD0iMjg0IiB2aWV3Qm94PSIwIDAgMjIwIDI4NCIgcm9sZT0iaW1nIiA+Cjx0aXRsZT5IRVhBTE9DSyBtb2R1bGFyIGludGVyZmFjZSBhc3NldDwvdGl0bGU+CjxkZWZzPjxsaW5lYXJHcmFkaWVudCBpZD0ia3JhZnRGcm9udCIgeDE9IjAiIHkxPSIwIiB4Mj0iMSIgeTI9IjEiPjxzdG9wIHN0b3AtY29sb3I9IiNEM0I5OUEiLz48c3RvcCBvZmZzZXQ9IjEiIHN0b3AtY29sb3I9IiNBMzgzNjMiLz48L2xpbmVhckdyYWRpZW50Pjxs ...(+6860 chars)\",\"value\":\"35\"},{\"image\":\"data:image\\/svg+xml;base64,PHN2ZyB4bWxucz0iaHR0cDovL3d3dy53My5vcmcvMjAwMC9zdmciIHdpZHRoPSIyMjAiIGhlaWdodD0iMjg0IiB2aWV3Qm94PSIwIDAgMjIwIDI4NCIgcm9sZT0iaW1nIiA+DQo8dGl0bGU+SEVYQUxPQ0sgbW9kdWxhciBpbnRlcmZhY2UgYXNzZXQ8L3RpdGxlPg0KPGRlZnM+PGxpbmVhckdyYWRpZW50IGlkPSJrcmFmdEZyb250IiB4MT0iMCIgeTE9IjAiIHgyPSIxIiB5Mj0iMSI+PHN0b3Agc3RvcC1jb2xvcj0iI0QzQjk5QSIvPjxzdG9wIG9mZnNldD0iMSIgc3RvcC1jb2xvcj0iI0EzODM2MyIvPjwvbGluZWFyR3JhZGllbnQ+ ...(+6912 chars)\",\"value\":\"36\"},{\"image\":\"data:image\\/svg+xml;base64,PHN2ZyB4bWxucz0iaHR0cDovL3d3dy53My5vcmcvMjAwMC9zdmciIHdpZHRoPSIyMjAiIGhlaWdodD0iMjg0IiB2aWV3Qm94PSIwIDAgMjIwIDI4NCIgcm9sZT0iaW1nIiA+DQo8dGl0bGU+SEVYQUxPQ0sgbW9kdWxhciBpbnRlcmZhY2UgYXNzZXQ8L3RpdGxlPg0KPGRlZnM+PGxpbmVhckdyYWRpZW50IGlkPSJrcmFmdEZyb250IiB4MT0iMCIgeTE9IjAiIHgyPSIxIiB5Mj0iMSI+PHN0b3Agc3RvcC1jb2xvcj0iI0QzQjk5QSIvPjxzdG9wIG9mZnNldD0iMSIgc3RvcC1jb2xvcj0iI0EzODM2MyIvPjwvbGluZWFyR3JhZGllbnQ+ ...(+6912 chars)\",\"value\":\"37\"},{\"image\":\"data:image\\/svg+xml;base64,PHN2ZyB4bWxucz0iaHR0cDovL3d3dy53My5vcmcvMjAwMC9zdmciIHdpZHRoPSIyMjAiIGhlaWdodD0iMjg0IiB2aWV3Qm94PSIwIDAgMjIwIDI4NCIgcm9sZT0iaW1nIiA+DQo8dGl0bGU+SEVYQUxPQ0sgbW9kdWxhciBpbnRlcmZhY2UgYXNzZXQ8L3RpdGxlPg0KPGRlZnM+PGxpbmVhckdyYWRpZW50IGlkPSJrcmFmdEZyb250IiB4MT0iMCIgeTE9IjAiIHgyPSIxIiB5Mj0iMSI+PHN0b3Agc3RvcC1jb2xvcj0iI0QzQjk5QSIvPjxzdG9wIG9mZnNldD0iMSIgc3RvcC1jb2xvcj0iI0EzODM2MyIvPjwvbGluZWFyR3JhZGllbnQ+ ...(+6912 chars)\",\"value\":\"38\"}],\"fixedAspectRatio\":\"on\"}},\"settings\":{\"BindingType\":\"signal\",\"backgroundColor\":[0,0,0],\"backgroundOffset\":0.14,\"backgroundOpacity\":1,\"blockOrientation\":\"Right\",\"fixedAspectRatio\":\"on\",\"showBackgroundColor\":false,\"value\":0,\"version\":\"R2026b\"},\"type\":\"MultistateImage\"}"
  MultiStateImage12 : CustomWebBlock  LabelPosition=Hide  ShowInitialText=on  Configuration="{\"components\":[{\"name\":\"BackgroundImageComponent\",\"settings\":{\"image\":{\"size\":[0,0],\"src\":\"default\",\"srcOrientation\":\"Right\"},\"position\":[0,0,1,1],\"scaleMode\":\"0\"}},{\"name\":\"MultistateImageStateComponent\",\"settings\":{\"applyDefaults\":true,\"position\":[0,0,1,1],\"states\":[{\"image\":{\"size\":[0.7746478873239436,1],\"src\":\"data:image\\/svg+xml;base64,PHN2ZyB4bWxucz0iaHR0cDovL3d3dy53My5vcmcvMjAwMC9zdmciIHdpZHRoPSIyMjAiIGhlaWdodD0iMjg0IiB2aWV3Qm94PSIwIDAgMjIwIDI4NCIgcm9sZT0iaW1nIiA+Cjx0aXRsZT5IRVhBTE9DSyBtb2R1bGFyIGludGVyZmFjZSBhc3NldDwvdGl0bGU+CjxkZWZzPjwvZGVmcz4KICAgICAgPHJlY3QgeD0iOCIgeT0iOCIgd2lkdGg9IjIwNCIgaGVpZ2h0PSIyNjgiIHJ4PSIxNCIgZmlsbD0iIzExMUMyMiIgc3Ryb2tlPSIjNTM2NjZFIiBzdHJva2Utd2lkdGg9IjIiLz4KICAgICAgPHJlY3QgeD0iMTIiIHk9IjEyIiB3aWR0 ...(+3224 chars)\",\"srcOrientation\":\"Right\"},\"position\":[0,0,1,1],\"value\":[]},{\"image\":{\"size\":[0,0],\"src\":\"data:image\\/svg+xml;base64,PHN2ZyB4bWxucz0iaHR0cDovL3d3dy53My5vcmcvMjAwMC9zdmciIHdpZHRoPSIyMjAiIGhlaWdodD0iMjg0IiB2aWV3Qm94PSIwIDAgMjIwIDI4NCIgcm9sZT0iaW1nIiA+Cjx0aXRsZT5IRVhBTE9DSyBtb2R1bGFyIGludGVyZmFjZSBhc3NldDwvdGl0bGU+CjxkZWZzPjwvZGVmcz4KICAgICAgPHJlY3QgeD0iOCIgeT0iOCIgd2lkdGg9IjIwNCIgaGVpZ2h0PSIyNjgiIHJ4PSIxNCIgZmlsbD0iIzExMUMyMiIgc3Ryb2tlPSIjNTM2NjZFIiBzdHJva2Utd2lkdGg9IjIiLz4KICAgICAgPHJlY3QgeD0iMTIiIHk9IjEyIiB3aWR0 ...(+3224 chars)\",\"srcOrientation\":\"Right\"},\"position\":[0,0,1,1],\"value\":\"0\"},{\"image\":{\"size\":[0,0],\"src\":\"data:image\\/svg+xml;base64,PHN2ZyB4bWxucz0iaHR0cDovL3d3dy53My5vcmcvMjAwMC9zdmciIHdpZHRoPSIyMjAiIGhlaWdodD0iMjg0IiB2aWV3Qm94PSIwIDAgMjIwIDI4NCIgcm9sZT0iaW1nIiA+Cjx0aXRsZT5IRVhBTE9DSyBtb2R1bGFyIGludGVyZmFjZSBhc3NldDwvdGl0bGU+CjxkZWZzPjwvZGVmcz4KICAgICAgPHJlY3QgeD0iOCIgeT0iOCIgd2lkdGg9IjIwNCIgaGVpZ2h0PSIyNjgiIHJ4PSIxNCIgZmlsbD0iIzExMUMyMiIgc3Ryb2tlPSIjNTM2NjZFIiBzdHJva2Utd2lkdGg9IjIiLz4KICAgICAgPHJlY3QgeD0iMTIiIHk9IjEyIiB3aWR0 ...(+3220 chars)\",\"srcOrientation\":\"Right\"},\"position\":[0,0,1,1],\"value\":\"1\"},{\"image\":{\"size\":[0,0],\"src\":\"data:image\\/svg+xml;base64,PHN2ZyB4bWxucz0iaHR0cDovL3d3dy53My5vcmcvMjAwMC9zdmciIHdpZHRoPSIyMjAiIGhlaWdodD0iMjg0IiB2aWV3Qm94PSIwIDAgMjIwIDI4NCIgcm9sZT0iaW1nIiA+Cjx0aXRsZT5IRVhBTE9DSyBtb2R1bGFyIGludGVyZmFjZSBhc3NldDwvdGl0bGU+CjxkZWZzPjwvZGVmcz4KICAgICAgPHJlY3QgeD0iOCIgeT0iOCIgd2lkdGg9IjIwNCIgaGVpZ2h0PSIyNjgiIHJ4PSIxNCIgZmlsbD0iIzExMUMyMiIgc3Ryb2tlPSIjQjk4NTZFIiBzdHJva2Utd2lkdGg9IjIuNiIvPgogICAgICA8cmVjdCB4PSIxMiIgeT0iMTIiIHdp ...(+3488 chars)\",\"srcOrientation\":\"Right\"},\"position\":[0,0,1,1],\"value\":\"2\"},{\"image\":{\"size\":[0,0],\"src\":\"data:image\\/svg+xml;base64,PHN2ZyB4bWxucz0iaHR0cDovL3d3dy53My5vcmcvMjAwMC9zdmciIHdpZHRoPSIyMjAiIGhlaWdodD0iMjg0IiB2aWV3Qm94PSIwIDAgMjIwIDI4NCIgcm9sZT0iaW1nIiA+Cjx0aXRsZT5IRVhBTE9DSyBtb2R1bGFyIGludGVyZmFjZSBhc3NldDwvdGl0bGU+CjxkZWZzPjwvZGVmcz4KICAgICAgPHJlY3QgeD0iOCIgeT0iOCIgd2lkdGg9IjIwNCIgaGVpZ2h0PSIyNjgiIHJ4PSIxNCIgZmlsbD0iIzExMUMyMiIgc3Ryb2tlPSIjQjk4NTZFIiBzdHJva2Utd2lkdGg9IjIuNiIvPgogICAgICA8cmVjdCB4PSIxMiIgeT0iMTIiIHdp ...(+3484 chars)\",\"srcOrientation\":\"Right\"},\"position\":[0,0,1,1],\"value\":\"3\"},{\"image\":{\"size\":[0,0],\"src\":\"data:image\\/svg+xml;base64,PHN2ZyB4bWxucz0iaHR0cDovL3d3dy53My5vcmcvMjAwMC9zdmciIHdpZHRoPSIyMjAiIGhlaWdodD0iMjg0IiB2aWV3Qm94PSIwIDAgMjIwIDI4NCIgcm9sZT0iaW1nIiA+Cjx0aXRsZT5IRVhBTE9DSyBtb2R1bGFyIGludGVyZmFjZSBhc3NldDwvdGl0bGU+CjxkZWZzPjwvZGVmcz4KICAgICAgPHJlY3QgeD0iOCIgeT0iOCIgd2lkdGg9IjIwNCIgaGVpZ2h0PSIyNjgiIHJ4PSIxNCIgZmlsbD0iIzExMUMyMiIgc3Ryb2tlPSIjQjk4NTZFIiBzdHJva2Utd2lkdGg9IjIuNiIvPgogICAgICA8cmVjdCB4PSIxMiIgeT0iMTIiIHdp ...(+3532 chars)\",\"srcOrientation\":\"Right\"},\"position\":[0,0,1,1],\"value\":\"4\"},{\"image\":{\"size\":[0,0],\"src\":\"data:image\\/svg+xml;base64,PHN2ZyB4bWxucz0iaHR0cDovL3d3dy53My5vcmcvMjAwMC9zdmciIHdpZHRoPSIyMjAiIGhlaWdodD0iMjg0IiB2aWV3Qm94PSIwIDAgMjIwIDI4NCIgcm9sZT0iaW1nIiA+Cjx0aXRsZT5IRVhBTE9DSyBtb2R1bGFyIGludGVyZmFjZSBhc3NldDwvdGl0bGU+CjxkZWZzPjwvZGVmcz4KICAgICAgPHJlY3QgeD0iOCIgeT0iOCIgd2lkdGg9IjIwNCIgaGVpZ2h0PSIyNjgiIHJ4PSIxNCIgZmlsbD0iIzExMUMyMiIgc3Ryb2tlPSIjQjk4NTZFIiBzdHJva2Utd2lkdGg9IjIuNiIvPgogICAgICA8cmVjdCB4PSIxMiIgeT0iMTIiIHdp ...(+3532 chars)\",\"srcOrientation\":\"Right\"},\"position\":[0,0,1,1],\"value\":\"5\"},{\"image\":{\"size\":[0,0],\"src\":\"data:image\\/svg+xml;base64,PHN2ZyB4bWxucz0iaHR0cDovL3d3dy53My5vcmcvMjAwMC9zdmciIHdpZHRoPSIyMjAiIGhlaWdodD0iMjg0IiB2aWV3Qm94PSIwIDAgMjIwIDI4NCIgcm9sZT0iaW1nIiA+Cjx0aXRsZT5IRVhBTE9DSyBtb2R1bGFyIGludGVyZmFjZSBhc3NldDwvdGl0bGU+CjxkZWZzPjwvZGVmcz4KICAgICAgPHJlY3QgeD0iOCIgeT0iOCIgd2lkdGg9IjIwNCIgaGVpZ2h0PSIyNjgiIHJ4PSIxNCIgZmlsbD0iIzExMUMyMiIgc3Ryb2tlPSIjQjk4NTZFIiBzdHJva2Utd2lkdGg9IjIuNiIvPgogICAgICA8cmVjdCB4PSIxMiIgeT0iMTIiIHdp ...(+3532 chars)\",\"srcOrientation\":\"Right\"},\"position\":[0,0,1,1],\"value\":\"6\"},{\"image\":{\"size\":[0,0],\"src\":\"data:image\\/svg+xml;base64,PHN2ZyB4bWxucz0iaHR0cDovL3d3dy53My5vcmcvMjAwMC9zdmciIHdpZHRoPSIyMjAiIGhlaWdodD0iMjg0IiB2aWV3Qm94PSIwIDAgMjIwIDI4NCIgcm9sZT0iaW1nIiA+Cjx0aXRsZT5IRVhBTE9DSyBtb2R1bGFyIGludGVyZmFjZSBhc3NldDwvdGl0bGU+CjxkZWZzPjwvZGVmcz4KICAgICAgPHJlY3QgeD0iOCIgeT0iOCIgd2lkdGg9IjIwNCIgaGVpZ2h0PSIyNjgiIHJ4PSIxNCIgZmlsbD0iIzExMUMyMiIgc3Ryb2tlPSIjQjk4NTZFIiBzdHJva2Utd2lkdGg9IjIuNiIvPgogICAgICA8cmVjdCB4PSIxMiIgeT0iMTIiIHdp ...(+3524 chars)\",\"srcOrientation\":\"Right\"},\"position\":[0,0,1,1],\"value\":\"7\"},{\"image\":{\"size\":[0,0],\"src\":\"data:image\\/svg+xml;base64,PHN2ZyB4bWxucz0iaHR0cDovL3d3dy53My5vcmcvMjAwMC9zdmciIHdpZHRoPSIyMjAiIGhlaWdodD0iMjg0IiB2aWV3Qm94PSIwIDAgMjIwIDI4NCIgcm9sZT0iaW1nIiA+Cjx0aXRsZT5IRVhBTE9DSyBtb2R1bGFyIGludGVyZmFjZSBhc3NldDwvdGl0bGU+CjxkZWZzPjwvZGVmcz4KICAgICAgPHJlY3QgeD0iOCIgeT0iOCIgd2lkdGg9IjIwNCIgaGVpZ2h0PSIyNjgiIHJ4PSIxNCIgZmlsbD0iIzExMUMyMiIgc3Ryb2tlPSIjQjk4NTZFIiBzdHJva2Utd2lkdGg9IjIuNiIvPgogICAgICA8cmVjdCB4PSIxMiIgeT0iMTIiIHdp ...(+3532 chars)\",\"srcOrientation\":\"Right\"},\"position\":[0,0,1,1],\"value\":\"8\"},{\"image\":{\"size\":[0,0],\"src\":\"data:image\\/svg+xml;base64,PHN2ZyB4bWxucz0iaHR0cDovL3d3dy53My5vcmcvMjAwMC9zdmciIHdpZHRoPSIyMjAiIGhlaWdodD0iMjg0IiB2aWV3Qm94PSIwIDAgMjIwIDI4NCIgcm9sZT0iaW1nIiA+Cjx0aXRsZT5IRVhBTE9DSyBtb2R1bGFyIGludGVyZmFjZSBhc3NldDwvdGl0bGU+CjxkZWZzPjwvZGVmcz4KICAgICAgPHJlY3QgeD0iOCIgeT0iOCIgd2lkdGg9IjIwNCIgaGVpZ2h0PSIyNjgiIHJ4PSIxNCIgZmlsbD0iIzExMUMyMiIgc3Ryb2tlPSIjQjk4NTZFIiBzdHJva2Utd2lkdGg9IjIuNiIvPgogICAgICA8cmVjdCB4PSIxMiIgeT0iMTIiIHdp ...(+3532 chars)\",\"srcOrientation\":\"Right\"},\"position\":[0,0,1,1],\"value\":\"9\"},{\"image\":{\"size\":[0,0],\"src\":\"data:image\\/svg+xml;base64,PHN2ZyB4bWxucz0iaHR0cDovL3d3dy53My5vcmcvMjAwMC9zdmciIHdpZHRoPSIyMjAiIGhlaWdodD0iMjg0IiB2aWV3Qm94PSIwIDAgMjIwIDI4NCIgcm9sZT0iaW1nIiA+Cjx0aXRsZT5IRVhBTE9DSyBtb2R1bGFyIGludGVyZmFjZSBhc3NldDwvdGl0bGU+CjxkZWZzPjwvZGVmcz4KICAgICAgPHJlY3QgeD0iOCIgeT0iOCIgd2lkdGg9IjIwNCIgaGVpZ2h0PSIyNjgiIHJ4PSIxNCIgZmlsbD0iIzExMUMyMiIgc3Ryb2tlPSIjQjk4NTZFIiBzdHJva2Utd2lkdGg9IjIuNiIvPgogICAgICA8cmVjdCB4PSIxMiIgeT0iMTIiIHdp ...(+3532 chars)\",\"srcOrientation\":\"Right\"},\"position\":[0,0,1,1],\"value\":\"10\"},{\"image\":{\"size\":[0,0],\"src\":\"data:image\\/svg+xml;base64,PHN2ZyB4bWxucz0iaHR0cDovL3d3dy53My5vcmcvMjAwMC9zdmciIHdpZHRoPSIyMjAiIGhlaWdodD0iMjg0IiB2aWV3Qm94PSIwIDAgMjIwIDI4NCIgcm9sZT0iaW1nIiA+Cjx0aXRsZT5IRVhBTE9DSyBtb2R1bGFyIGludGVyZmFjZSBhc3NldDwvdGl0bGU+CjxkZWZzPjwvZGVmcz4KICAgICAgPHJlY3QgeD0iOCIgeT0iOCIgd2lkdGg9IjIwNCIgaGVpZ2h0PSIyNjgiIHJ4PSIxNCIgZmlsbD0iIzExMUMyMiIgc3Ryb2tlPSIjNTM2NjZFIiBzdHJva2Utd2lkdGg9IjIiLz4KICAgICAgPHJlY3QgeD0iMTIiIHk9IjEyIiB3aWR0 ...(+3220 chars)\",\"srcOrientation\":\"Right\"},\"position\":[0,0,1,1],\"value\":\"11\"},{\"image\":{\"size\":[0,0],\"src\":\"data:image\\/svg+xml;base64,PHN2ZyB4bWxucz0iaHR0cDovL3d3dy53My5vcmcvMjAwMC9zdmciIHdpZHRoPSIyMjAiIGhlaWdodD0iMjg0IiB2aWV3Qm94PSIwIDAgMjIwIDI4NCIgcm9sZT0iaW1nIiA+Cjx0aXRsZT5IRVhBTE9DSyBtb2R1bGFyIGludGVyZmFjZSBhc3NldDwvdGl0bGU+CjxkZWZzPjxsaW5lYXJHcmFkaWVudCBpZD0ia3JhZnRGcm9udCIgeDE9IjAiIHkxPSIwIiB4Mj0iMSIgeTI9IjEiPjxzdG9wIHN0b3AtY29sb3I9IiNEM0I5OUEiLz48c3RvcCBvZmZzZXQ9IjEiIHN0b3AtY29sb3I9IiNBMzgzNjMiLz48L2xpbmVhckdyYWRpZW50Pjxs ...(+4752 chars)\",\"srcOrientation\":\"Right\"},\"position\":[0,0,1,1],\"value\":\"20\"},{\"image\":{\"size\":[0,0],\"src\":\"data:image\\/svg+xml;base64,PHN2ZyB4bWxucz0iaHR0cDovL3d3dy53My5vcmcvMjAwMC9zdmciIHdpZHRoPSIyMjAiIGhlaWdodD0iMjg0IiB2aWV3Qm94PSIwIDAgMjIwIDI4NCIgcm9sZT0iaW1nIiA+Cjx0aXRsZT5IRVhBTE9DSyBtb2R1bGFyIGludGVyZmFjZSBhc3NldDwvdGl0bGU+CjxkZWZzPjxsaW5lYXJHcmFkaWVudCBpZD0ia3JhZnRGcm9udCIgeDE9IjAiIHkxPSIwIiB4Mj0iMSIgeTI9IjEiPjxzdG9wIHN0b3AtY29sb3I9IiNEM0I5OUEiLz48c3RvcCBvZmZzZXQ9IjEiIHN0b3AtY29sb3I9IiNBMzgzNjMiLz48L2xpbmVhckdyYWRpZW50Pjxs ...(+7264 chars)\",\"srcOrientation\":\"Right\"},\"position\":[0,0,1,1],\"value\":\"21\"},{\"image\":{\"size\":[0,0],\"src\":\"data:image\\/svg+xml;base64,PHN2ZyB4bWxucz0iaHR0cDovL3d3dy53My5vcmcvMjAwMC9zdmciIHdpZHRoPSIyMjAiIGhlaWdodD0iMjg0IiB2aWV3Qm94PSIwIDAgMjIwIDI4NCIgcm9sZT0iaW1nIiA+Cjx0aXRsZT5IRVhBTE9DSyBtb2R1bGFyIGludGVyZmFjZSBhc3NldDwvdGl0bGU+CjxkZWZzPjxsaW5lYXJHcmFkaWVudCBpZD0ia3JhZnRGcm9udCIgeDE9IjAiIHkxPSIwIiB4Mj0iMSIgeTI9IjEiPjxzdG9wIHN0b3AtY29sb3I9IiNEM0I5OUEiLz48c3RvcCBvZmZzZXQ9IjEiIHN0b3AtY29sb3I9IiNBMzgzNjMiLz48L2xpbmVhckdyYWRpZW50Pjxs ...(+7264 chars)\",\"srcOrientation\":\"Right\"},\"position\":[0,0,1,1],\"value\":\"22\"},{\"image\":{\"size\":[0,0],\"src\":\"data:image\\/svg+xml;base64,PHN2ZyB4bWxucz0iaHR0cDovL3d3dy53My5vcmcvMjAwMC9zdmciIHdpZHRoPSIyMjAiIGhlaWdodD0iMjg0IiB2aWV3Qm94PSIwIDAgMjIwIDI4NCIgcm9sZT0iaW1nIiA+Cjx0aXRsZT5IRVhBTE9DSyBtb2R1bGFyIGludGVyZmFjZSBhc3NldDwvdGl0bGU+CjxkZWZzPjxsaW5lYXJHcmFkaWVudCBpZD0ia3JhZnRGcm9udCIgeDE9IjAiIHkxPSIwIiB4Mj0iMSIgeTI9IjEiPjxzdG9wIHN0b3AtY29sb3I9IiNEM0I5OUEiLz48c3RvcCBvZmZzZXQ9IjEiIHN0b3AtY29sb3I9IiNBMzgzNjMiLz48L2xpbmVhckdyYWRpZW50Pjxs ...(+7264 chars)\",\"srcOrientation\":\"Right\"},\"position\":[0,0,1,1],\"value\":\"23\"},{\"image\":{\"size\":[0,0],\"src\":\"data:image\\/svg+xml;base64,PHN2ZyB4bWxucz0iaHR0cDovL3d3dy53My5vcmcvMjAwMC9zdmciIHdpZHRoPSIyMjAiIGhlaWdodD0iMjg0IiB2aWV3Qm94PSIwIDAgMjIwIDI4NCIgcm9sZT0iaW1nIiA+Cjx0aXRsZT5IRVhBTE9DSyBtb2R1bGFyIGludGVyZmFjZSBhc3NldDwvdGl0bGU+CjxkZWZzPjxsaW5lYXJHcmFkaWVudCBpZD0ia3JhZnRGcm9udCIgeDE9IjAiIHkxPSIwIiB4Mj0iMSIgeTI9IjEiPjxzdG9wIHN0b3AtY29sb3I9IiNEM0I5OUEiLz48c3RvcCBvZmZzZXQ9IjEiIHN0b3AtY29sb3I9IiNBMzgzNjMiLz48L2xpbmVhckdyYWRpZW50Pjxs ...(+7260 chars)\",\"srcOrientation\":\"Right\"},\"position\":[0,0,1,1],\"value\":\"24\"},{\"image\":{\"size\":[0,0],\"src\":\"data:image\\/svg+xml;base64,PHN2ZyB4bWxucz0iaHR0cDovL3d3dy53My5vcmcvMjAwMC9zdmciIHdpZHRoPSIyMjAiIGhlaWdodD0iMjg0IiB2aWV3Qm94PSIwIDAgMjIwIDI4NCIgcm9sZT0iaW1nIiA+Cjx0aXRsZT5IRVhBTE9DSyBtb2R1bGFyIGludGVyZmFjZSBhc3NldDwvdGl0bGU+CjxkZWZzPjxsaW5lYXJHcmFkaWVudCBpZD0ia3JhZnRGcm9udCIgeDE9IjAiIHkxPSIwIiB4Mj0iMSIgeTI9IjEiPjxzdG9wIHN0b3AtY29sb3I9IiNEM0I5OUEiLz48c3RvcCBvZmZzZXQ9IjEiIHN0b3AtY29sb3I9IiNBMzgzNjMiLz48L2xpbmVhckdyYWRpZW50Pjxs ...(+7264 chars)\",\"srcOrientation\":\"Right\"},\"position\":[0,0,1,1],\"value\":\"25\"},{\"image\":{\"size\":[0,0],\"src\":\"data:image\\/svg+xml;base64,PHN2ZyB4bWxucz0iaHR0cDovL3d3dy53My5vcmcvMjAwMC9zdmciIHdpZHRoPSIyMjAiIGhlaWdodD0iMjg0IiB2aWV3Qm94PSIwIDAgMjIwIDI4NCIgcm9sZT0iaW1nIiA+Cjx0aXRsZT5IRVhBTE9DSyBtb2R1bGFyIGludGVyZmFjZSBhc3NldDwvdGl0bGU+CjxkZWZzPjxsaW5lYXJHcmFkaWVudCBpZD0ia3JhZnRGcm9udCIgeDE9IjAiIHkxPSIwIiB4Mj0iMSIgeTI9IjEiPjxzdG9wIHN0b3AtY29sb3I9IiNEM0I5OUEiLz48c3RvcCBvZmZzZXQ9IjEiIHN0b3AtY29sb3I9IiNBMzgzNjMiLz48L2xpbmVhckdyYWRpZW50Pjxs ...(+7272 chars)\",\"srcOrientation\":\"Right\"},\"position\":[0,0,1,1],\"value\":\"26\"},{\"image\":{\"size\":[0,0],\"src\":\"data:image\\/svg+xml;base64,PHN2ZyB4bWxucz0iaHR0cDovL3d3dy53My5vcmcvMjAwMC9zdmciIHdpZHRoPSIyMjAiIGhlaWdodD0iMjg0IiB2aWV3Qm94PSIwIDAgMjIwIDI4NCIgcm9sZT0iaW1nIiA+Cjx0aXRsZT5IRVhBTE9DSyBtb2R1bGFyIGludGVyZmFjZSBhc3NldDwvdGl0bGU+CjxkZWZzPjxsaW5lYXJHcmFkaWVudCBpZD0ia3JhZnRGcm9udCIgeDE9IjAiIHkxPSIwIiB4Mj0iMSIgeTI9IjEiPjxzdG9wIHN0b3AtY29sb3I9IiNEM0I5OUEiLz48c3RvcCBvZmZzZXQ9IjEiIHN0b3AtY29sb3I9IiNBMzgzNjMiLz48L2xpbmVhckdyYWRpZW50Pjxs ...(+7264 chars)\",\"srcOrientation\":\"Right\"},\"position\":[0,0,1,1],\"value\":\"27\"},{\"image\":{\"size\":[0,0],\"src\":\"data:image\\/svg+xml;base64,PHN2ZyB4bWxucz0iaHR0cDovL3d3dy53My5vcmcvMjAwMC9zdmciIHdpZHRoPSIyMjAiIGhlaWdodD0iMjg0IiB2aWV3Qm94PSIwIDAgMjIwIDI4NCIgcm9sZT0iaW1nIiA+Cjx0aXRsZT5IRVhBTE9DSyBtb2R1bGFyIGludGVyZmFjZSBhc3NldDwvdGl0bGU+CjxkZWZzPjxsaW5lYXJHcmFkaWVudCBpZD0ia3JhZnRGcm9udCIgeDE9IjAiIHkxPSIwIiB4Mj0iMSIgeTI9IjEiPjxzdG9wIHN0b3AtY29sb3I9IiNEM0I5OUEiLz48c3RvcCBvZmZzZXQ9IjEiIHN0b3AtY29sb3I9IiNBMzgzNjMiLz48L2xpbmVhckdyYWRpZW50Pjxs ...(+7268 chars)\",\"srcOrientation\":\"Right\"},\"position\":[0,0,1,1],\"value\":\"28\"},{\"image\":{\"size\":[0,0],\"src\":\"data:image\\/svg+xml;base64,PHN2ZyB4bWxucz0iaHR0cDovL3d3dy53My5vcmcvMjAwMC9zdmciIHdpZHRoPSIyMjAiIGhlaWdodD0iMjg0IiB2aWV3Qm94PSIwIDAgMjIwIDI4NCIgcm9sZT0iaW1nIiA+Cjx0aXRsZT5IRVhBTE9DSyBtb2R1bGFyIGludGVyZmFjZSBhc3NldDwvdGl0bGU+CjxkZWZzPjxsaW5lYXJHcmFkaWVudCBpZD0ia3JhZnRGcm9udCIgeDE9IjAiIHkxPSIwIiB4Mj0iMSIgeTI9IjEiPjxzdG9wIHN0b3AtY29sb3I9IiNEM0I5OUEiLz48c3RvcCBvZmZzZXQ9IjEiIHN0b3AtY29sb3I9IiNBMzgzNjMiLz48L2xpbmVhckdyYWRpZW50Pjxs ...(+7268 chars)\",\"srcOrientation\":\"Right\"},\"position\":[0,0,1,1],\"value\":\"29\"},{\"image\":{\"size\":[0,0],\"src\":\"data:image\\/svg+xml;base64,PHN2ZyB4bWxucz0iaHR0cDovL3d3dy53My5vcmcvMjAwMC9zdmciIHdpZHRoPSIyMjAiIGhlaWdodD0iMjg0IiB2aWV3Qm94PSIwIDAgMjIwIDI4NCIgcm9sZT0iaW1nIiA+Cjx0aXRsZT5IRVhBTE9DSyBtb2R1bGFyIGludGVyZmFjZSBhc3NldDwvdGl0bGU+CjxkZWZzPjxsaW5lYXJHcmFkaWVudCBpZD0ia3JhZnRGcm9udCIgeDE9IjAiIHkxPSIwIiB4Mj0iMSIgeTI9IjEiPjxzdG9wIHN0b3AtY29sb3I9IiNEM0I5OUEiLz48c3RvcCBvZmZzZXQ9IjEiIHN0b3AtY29sb3I9IiNBMzgzNjMiLz48L2xpbmVhckdyYWRpZW50Pjxs ...(+7268 chars)\",\"srcOrientation\":\"Right\"},\"position\":[0,0,1,1],\"value\":\"30\"},{\"image\":{\"size\":[0,0],\"src\":\"data:image\\/svg+xml;base64,PHN2ZyB4bWxucz0iaHR0cDovL3d3dy53My5vcmcvMjAwMC9zdmciIHdpZHRoPSIyMjAiIGhlaWdodD0iMjg0IiB2aWV3Qm94PSIwIDAgMjIwIDI4NCIgcm9sZT0iaW1nIiA+Cjx0aXRsZT5IRVhBTE9DSyBtb2R1bGFyIGludGVyZmFjZSBhc3NldDwvdGl0bGU+CjxkZWZzPjxsaW5lYXJHcmFkaWVudCBpZD0ia3JhZnRGcm9udCIgeDE9IjAiIHkxPSIwIiB4Mj0iMSIgeTI9IjEiPjxzdG9wIHN0b3AtY29sb3I9IiNEM0I5OUEiLz48c3RvcCBvZmZzZXQ9IjEiIHN0b3AtY29sb3I9IiNBMzgzNjMiLz48L2xpbmVhckdyYWRpZW50Pjxs ...(+4756 chars)\",\"srcOrientation\":\"Right\"},\"position\":[0,0,1,1],\"value\":\"31\"},{\"image\":{\"size\":[0,0],\"src\":\"data:image\\/svg+xml;base64,PHN2ZyB4bWxucz0iaHR0cDovL3d3dy53My5vcmcvMjAwMC9zdmciIHdpZHRoPSIyMjAiIGhlaWdodD0iMjg0IiB2aWV3Qm94PSIwIDAgMjIwIDI4NCIgcm9sZT0iaW1nIiA+Cjx0aXRsZT5IRVhBTE9DSyBtb2R1bGFyIGludGVyZmFjZSBhc3NldDwvdGl0bGU+CjxkZWZzPjxsaW5lYXJHcmFkaWVudCBpZD0ia3JhZnRGcm9udCIgeDE9IjAiIHkxPSIwIiB4Mj0iMSIgeTI9IjEiPjxzdG9wIHN0b3AtY29sb3I9IiNEM0I5OUEiLz48c3RvcCBvZmZzZXQ9IjEiIHN0b3AtY29sb3I9IiNBMzgzNjMiLz48L2xpbmVhckdyYWRpZW50Pjxs ...(+4752 chars)\",\"srcOrientation\":\"Right\"},\"position\":[0,0,1,1],\"value\":\"32\"},{\"image\":{\"size\":[0,0],\"src\":\"data:image\\/svg+xml;base64,PHN2ZyB4bWxucz0iaHR0cDovL3d3dy53My5vcmcvMjAwMC9zdmciIHdpZHRoPSIyMjAiIGhlaWdodD0iMjg0IiB2aWV3Qm94PSIwIDAgMjIwIDI4NCIgcm9sZT0iaW1nIiA+Cjx0aXRsZT5IRVhBTE9DSyBtb2R1bGFyIGludGVyZmFjZSBhc3NldDwvdGl0bGU+CjxkZWZzPjxsaW5lYXJHcmFkaWVudCBpZD0ia3JhZnRGcm9udCIgeDE9IjAiIHkxPSIwIiB4Mj0iMSIgeTI9IjEiPjxzdG9wIHN0b3AtY29sb3I9IiNEM0I5OUEiLz48c3RvcCBvZmZzZXQ9IjEiIHN0b3AtY29sb3I9IiNBMzgzNjMiLz48L2xpbmVhckdyYWRpZW50Pjxs ...(+6860 chars)\",\"srcOrientation\":\"Right\"},\"position\":[0,0,1,1],\"value\":\"33\"},{\"image\":{\"size\":[0,0],\"src\":\"data:image\\/svg+xml;base64,PHN2ZyB4bWxucz0iaHR0cDovL3d3dy53My5vcmcvMjAwMC9zdmciIHdpZHRoPSIyMjAiIGhlaWdodD0iMjg0IiB2aWV3Qm94PSIwIDAgMjIwIDI4NCIgcm9sZT0iaW1nIiA+Cjx0aXRsZT5IRVhBTE9DSyBtb2R1bGFyIGludGVyZmFjZSBhc3NldDwvdGl0bGU+CjxkZWZzPjxsaW5lYXJHcmFkaWVudCBpZD0ia3JhZnRGcm9udCIgeDE9IjAiIHkxPSIwIiB4Mj0iMSIgeTI9IjEiPjxzdG9wIHN0b3AtY29sb3I9IiNEM0I5OUEiLz48c3RvcCBvZmZzZXQ9IjEiIHN0b3AtY29sb3I9IiNBMzgzNjMiLz48L2xpbmVhckdyYWRpZW50Pjxs ...(+6860 chars)\",\"srcOrientation\":\"Right\"},\"position\":[0,0,1,1],\"value\":\"34\"},{\"image\":{\"size\":[0,0],\"src\":\"data:image\\/svg+xml;base64,PHN2ZyB4bWxucz0iaHR0cDovL3d3dy53My5vcmcvMjAwMC9zdmciIHdpZHRoPSIyMjAiIGhlaWdodD0iMjg0IiB2aWV3Qm94PSIwIDAgMjIwIDI4NCIgcm9sZT0iaW1nIiA+Cjx0aXRsZT5IRVhBTE9DSyBtb2R1bGFyIGludGVyZmFjZSBhc3NldDwvdGl0bGU+CjxkZWZzPjxsaW5lYXJHcmFkaWVudCBpZD0ia3JhZnRGcm9udCIgeDE9IjAiIHkxPSIwIiB4Mj0iMSIgeTI9IjEiPjxzdG9wIHN0b3AtY29sb3I9IiNEM0I5OUEiLz48c3RvcCBvZmZzZXQ9IjEiIHN0b3AtY29sb3I9IiNBMzgzNjMiLz48L2xpbmVhckdyYWRpZW50Pjxs ...(+6860 chars)\",\"srcOrientation\":\"Right\"},\"position\":[0,0,1,1],\"value\":\"35\"},{\"image\":{\"size\":[0,0],\"src\":\"data:image\\/svg+xml;base64,PHN2ZyB4bWxucz0iaHR0cDovL3d3dy53My5vcmcvMjAwMC9zdmciIHdpZHRoPSIyMjAiIGhlaWdodD0iMjg0IiB2aWV3Qm94PSIwIDAgMjIwIDI4NCIgcm9sZT0iaW1nIiA+DQo8dGl0bGU+SEVYQUxPQ0sgbW9kdWxhciBpbnRlcmZhY2UgYXNzZXQ8L3RpdGxlPg0KPGRlZnM+PGxpbmVhckdyYWRpZW50IGlkPSJrcmFmdEZyb250IiB4MT0iMCIgeTE9IjAiIHgyPSIxIiB5Mj0iMSI+PHN0b3Agc3RvcC1jb2xvcj0iI0QzQjk5QSIvPjxzdG9wIG9mZnNldD0iMSIgc3RvcC1jb2xvcj0iI0EzODM2MyIvPjwvbGluZWFyR3JhZGllbnQ+ ...(+6912 chars)\",\"srcOrientation\":\"Right\"},\"position\":[0,0,1,1],\"value\":\"36\"},{\"image\":{\"size\":[0,0],\"src\":\"data:image\\/svg+xml;base64,PHN2ZyB4bWxucz0iaHR0cDovL3d3dy53My5vcmcvMjAwMC9zdmciIHdpZHRoPSIyMjAiIGhlaWdodD0iMjg0IiB2aWV3Qm94PSIwIDAgMjIwIDI4NCIgcm9sZT0iaW1nIiA+DQo8dGl0bGU+SEVYQUxPQ0sgbW9kdWxhciBpbnRlcmZhY2UgYXNzZXQ8L3RpdGxlPg0KPGRlZnM+PGxpbmVhckdyYWRpZW50IGlkPSJrcmFmdEZyb250IiB4MT0iMCIgeTE9IjAiIHgyPSIxIiB5Mj0iMSI+PHN0b3Agc3RvcC1jb2xvcj0iI0QzQjk5QSIvPjxzdG9wIG9mZnNldD0iMSIgc3RvcC1jb2xvcj0iI0EzODM2MyIvPjwvbGluZWFyR3JhZGllbnQ+ ...(+6912 chars)\",\"srcOrientation\":\"Right\"},\"position\":[0,0,1,1],\"value\":\"37\"},{\"image\":{\"size\":[0,0],\"src\":\"data:image\\/svg+xml;base64,PHN2ZyB4bWxucz0iaHR0cDovL3d3dy53My5vcmcvMjAwMC9zdmciIHdpZHRoPSIyMjAiIGhlaWdodD0iMjg0IiB2aWV3Qm94PSIwIDAgMjIwIDI4NCIgcm9sZT0iaW1nIiA+DQo8dGl0bGU+SEVYQUxPQ0sgbW9kdWxhciBpbnRlcmZhY2UgYXNzZXQ8L3RpdGxlPg0KPGRlZnM+PGxpbmVhckdyYWRpZW50IGlkPSJrcmFmdEZyb250IiB4MT0iMCIgeTE9IjAiIHgyPSIxIiB5Mj0iMSI+PHN0b3Agc3RvcC1jb2xvcj0iI0QzQjk5QSIvPjxzdG9wIG9mZnNldD0iMSIgc3RvcC1jb2xvcj0iI0EzODM2MyIvPjwvbGluZWFyR3JhZGllbnQ+ ...(+6912 chars)\",\"srcOrientation\":\"Right\"},\"position\":[0,0,1,1],\"value\":\"38\"}],\"valueType\":\"discrete\"}},{\"name\":\"ForegroundImageComponent\",\"settings\":{\"image\":{\"size\":[0,0],\"src\":\"default\",\"srcOrientation\":\"Right\"},\"isForeground\":1,\"position\":[0,0,1,1],\"scaleMode\":\"0\"}}],\"derived\":{\"blockParameters\":{\"DefaultImage\":\"data:image\\/svg+xml;base64,PHN2ZyB4bWxucz0iaHR0cDovL3d3dy53My5vcmcvMjAwMC9zdmciIHdpZHRoPSIyMjAiIGhlaWdodD0iMjg0IiB2aWV3Qm94PSIwIDAgMjIwIDI4NCIgcm9sZT0iaW1nIiA+Cjx0aXRsZT5IRVhBTE9DSyBtb2R1bGFyIGludGVyZmFjZSBhc3NldDwvdGl0bGU+CjxkZWZzPjwvZGVmcz4KICAgICAgPHJlY3QgeD0iOCIgeT0iOCIgd2lkdGg9IjIwNCIgaGVpZ2h0PSIyNjgiIHJ4PSIxNCIgZmlsbD0iIzExMUMyMiIgc3Ryb2tlPSIjNTM2NjZFIiBzdHJva2Utd2lkdGg9IjIiLz4KICAgICAgPHJlY3QgeD0iMTIiIHk9IjEyIiB3aWR0 ...(+3224 chars)\",\"StateValueType\":\"discrete\",\"States\":[{\"image\":\"data:image\\/svg+xml;base64,PHN2ZyB4bWxucz0iaHR0cDovL3d3dy53My5vcmcvMjAwMC9zdmciIHdpZHRoPSIyMjAiIGhlaWdodD0iMjg0IiB2aWV3Qm94PSIwIDAgMjIwIDI4NCIgcm9sZT0iaW1nIiA+Cjx0aXRsZT5IRVhBTE9DSyBtb2R1bGFyIGludGVyZmFjZSBhc3NldDwvdGl0bGU+CjxkZWZzPjwvZGVmcz4KICAgICAgPHJlY3QgeD0iOCIgeT0iOCIgd2lkdGg9IjIwNCIgaGVpZ2h0PSIyNjgiIHJ4PSIxNCIgZmlsbD0iIzExMUMyMiIgc3Ryb2tlPSIjNTM2NjZFIiBzdHJva2Utd2lkdGg9IjIiLz4KICAgICAgPHJlY3QgeD0iMTIiIHk9IjEyIiB3aWR0 ...(+3224 chars)\",\"value\":\"0\"},{\"image\":\"data:image\\/svg+xml;base64,PHN2ZyB4bWxucz0iaHR0cDovL3d3dy53My5vcmcvMjAwMC9zdmciIHdpZHRoPSIyMjAiIGhlaWdodD0iMjg0IiB2aWV3Qm94PSIwIDAgMjIwIDI4NCIgcm9sZT0iaW1nIiA+Cjx0aXRsZT5IRVhBTE9DSyBtb2R1bGFyIGludGVyZmFjZSBhc3NldDwvdGl0bGU+CjxkZWZzPjwvZGVmcz4KICAgICAgPHJlY3QgeD0iOCIgeT0iOCIgd2lkdGg9IjIwNCIgaGVpZ2h0PSIyNjgiIHJ4PSIxNCIgZmlsbD0iIzExMUMyMiIgc3Ryb2tlPSIjNTM2NjZFIiBzdHJva2Utd2lkdGg9IjIiLz4KICAgICAgPHJlY3QgeD0iMTIiIHk9IjEyIiB3aWR0 ...(+3220 chars)\",\"value\":\"1\"},{\"image\":\"data:image\\/svg+xml;base64,PHN2ZyB4bWxucz0iaHR0cDovL3d3dy53My5vcmcvMjAwMC9zdmciIHdpZHRoPSIyMjAiIGhlaWdodD0iMjg0IiB2aWV3Qm94PSIwIDAgMjIwIDI4NCIgcm9sZT0iaW1nIiA+Cjx0aXRsZT5IRVhBTE9DSyBtb2R1bGFyIGludGVyZmFjZSBhc3NldDwvdGl0bGU+CjxkZWZzPjwvZGVmcz4KICAgICAgPHJlY3QgeD0iOCIgeT0iOCIgd2lkdGg9IjIwNCIgaGVpZ2h0PSIyNjgiIHJ4PSIxNCIgZmlsbD0iIzExMUMyMiIgc3Ryb2tlPSIjQjk4NTZFIiBzdHJva2Utd2lkdGg9IjIuNiIvPgogICAgICA8cmVjdCB4PSIxMiIgeT0iMTIiIHdp ...(+3488 chars)\",\"value\":\"2\"},{\"image\":\"data:image\\/svg+xml;base64,PHN2ZyB4bWxucz0iaHR0cDovL3d3dy53My5vcmcvMjAwMC9zdmciIHdpZHRoPSIyMjAiIGhlaWdodD0iMjg0IiB2aWV3Qm94PSIwIDAgMjIwIDI4NCIgcm9sZT0iaW1nIiA+Cjx0aXRsZT5IRVhBTE9DSyBtb2R1bGFyIGludGVyZmFjZSBhc3NldDwvdGl0bGU+CjxkZWZzPjwvZGVmcz4KICAgICAgPHJlY3QgeD0iOCIgeT0iOCIgd2lkdGg9IjIwNCIgaGVpZ2h0PSIyNjgiIHJ4PSIxNCIgZmlsbD0iIzExMUMyMiIgc3Ryb2tlPSIjQjk4NTZFIiBzdHJva2Utd2lkdGg9IjIuNiIvPgogICAgICA8cmVjdCB4PSIxMiIgeT0iMTIiIHdp ...(+3484 chars)\",\"value\":\"3\"},{\"image\":\"data:image\\/svg+xml;base64,PHN2ZyB4bWxucz0iaHR0cDovL3d3dy53My5vcmcvMjAwMC9zdmciIHdpZHRoPSIyMjAiIGhlaWdodD0iMjg0IiB2aWV3Qm94PSIwIDAgMjIwIDI4NCIgcm9sZT0iaW1nIiA+Cjx0aXRsZT5IRVhBTE9DSyBtb2R1bGFyIGludGVyZmFjZSBhc3NldDwvdGl0bGU+CjxkZWZzPjwvZGVmcz4KICAgICAgPHJlY3QgeD0iOCIgeT0iOCIgd2lkdGg9IjIwNCIgaGVpZ2h0PSIyNjgiIHJ4PSIxNCIgZmlsbD0iIzExMUMyMiIgc3Ryb2tlPSIjQjk4NTZFIiBzdHJva2Utd2lkdGg9IjIuNiIvPgogICAgICA8cmVjdCB4PSIxMiIgeT0iMTIiIHdp ...(+3532 chars)\",\"value\":\"4\"},{\"image\":\"data:image\\/svg+xml;base64,PHN2ZyB4bWxucz0iaHR0cDovL3d3dy53My5vcmcvMjAwMC9zdmciIHdpZHRoPSIyMjAiIGhlaWdodD0iMjg0IiB2aWV3Qm94PSIwIDAgMjIwIDI4NCIgcm9sZT0iaW1nIiA+Cjx0aXRsZT5IRVhBTE9DSyBtb2R1bGFyIGludGVyZmFjZSBhc3NldDwvdGl0bGU+CjxkZWZzPjwvZGVmcz4KICAgICAgPHJlY3QgeD0iOCIgeT0iOCIgd2lkdGg9IjIwNCIgaGVpZ2h0PSIyNjgiIHJ4PSIxNCIgZmlsbD0iIzExMUMyMiIgc3Ryb2tlPSIjQjk4NTZFIiBzdHJva2Utd2lkdGg9IjIuNiIvPgogICAgICA8cmVjdCB4PSIxMiIgeT0iMTIiIHdp ...(+3532 chars)\",\"value\":\"5\"},{\"image\":\"data:image\\/svg+xml;base64,PHN2ZyB4bWxucz0iaHR0cDovL3d3dy53My5vcmcvMjAwMC9zdmciIHdpZHRoPSIyMjAiIGhlaWdodD0iMjg0IiB2aWV3Qm94PSIwIDAgMjIwIDI4NCIgcm9sZT0iaW1nIiA+Cjx0aXRsZT5IRVhBTE9DSyBtb2R1bGFyIGludGVyZmFjZSBhc3NldDwvdGl0bGU+CjxkZWZzPjwvZGVmcz4KICAgICAgPHJlY3QgeD0iOCIgeT0iOCIgd2lkdGg9IjIwNCIgaGVpZ2h0PSIyNjgiIHJ4PSIxNCIgZmlsbD0iIzExMUMyMiIgc3Ryb2tlPSIjQjk4NTZFIiBzdHJva2Utd2lkdGg9IjIuNiIvPgogICAgICA8cmVjdCB4PSIxMiIgeT0iMTIiIHdp ...(+3532 chars)\",\"value\":\"6\"},{\"image\":\"data:image\\/svg+xml;base64,PHN2ZyB4bWxucz0iaHR0cDovL3d3dy53My5vcmcvMjAwMC9zdmciIHdpZHRoPSIyMjAiIGhlaWdodD0iMjg0IiB2aWV3Qm94PSIwIDAgMjIwIDI4NCIgcm9sZT0iaW1nIiA+Cjx0aXRsZT5IRVhBTE9DSyBtb2R1bGFyIGludGVyZmFjZSBhc3NldDwvdGl0bGU+CjxkZWZzPjwvZGVmcz4KICAgICAgPHJlY3QgeD0iOCIgeT0iOCIgd2lkdGg9IjIwNCIgaGVpZ2h0PSIyNjgiIHJ4PSIxNCIgZmlsbD0iIzExMUMyMiIgc3Ryb2tlPSIjQjk4NTZFIiBzdHJva2Utd2lkdGg9IjIuNiIvPgogICAgICA8cmVjdCB4PSIxMiIgeT0iMTIiIHdp ...(+3524 chars)\",\"value\":\"7\"},{\"image\":\"data:image\\/svg+xml;base64,PHN2ZyB4bWxucz0iaHR0cDovL3d3dy53My5vcmcvMjAwMC9zdmciIHdpZHRoPSIyMjAiIGhlaWdodD0iMjg0IiB2aWV3Qm94PSIwIDAgMjIwIDI4NCIgcm9sZT0iaW1nIiA+Cjx0aXRsZT5IRVhBTE9DSyBtb2R1bGFyIGludGVyZmFjZSBhc3NldDwvdGl0bGU+CjxkZWZzPjwvZGVmcz4KICAgICAgPHJlY3QgeD0iOCIgeT0iOCIgd2lkdGg9IjIwNCIgaGVpZ2h0PSIyNjgiIHJ4PSIxNCIgZmlsbD0iIzExMUMyMiIgc3Ryb2tlPSIjQjk4NTZFIiBzdHJva2Utd2lkdGg9IjIuNiIvPgogICAgICA8cmVjdCB4PSIxMiIgeT0iMTIiIHdp ...(+3532 chars)\",\"value\":\"8\"},{\"image\":\"data:image\\/svg+xml;base64,PHN2ZyB4bWxucz0iaHR0cDovL3d3dy53My5vcmcvMjAwMC9zdmciIHdpZHRoPSIyMjAiIGhlaWdodD0iMjg0IiB2aWV3Qm94PSIwIDAgMjIwIDI4NCIgcm9sZT0iaW1nIiA+Cjx0aXRsZT5IRVhBTE9DSyBtb2R1bGFyIGludGVyZmFjZSBhc3NldDwvdGl0bGU+CjxkZWZzPjwvZGVmcz4KICAgICAgPHJlY3QgeD0iOCIgeT0iOCIgd2lkdGg9IjIwNCIgaGVpZ2h0PSIyNjgiIHJ4PSIxNCIgZmlsbD0iIzExMUMyMiIgc3Ryb2tlPSIjQjk4NTZFIiBzdHJva2Utd2lkdGg9IjIuNiIvPgogICAgICA8cmVjdCB4PSIxMiIgeT0iMTIiIHdp ...(+3532 chars)\",\"value\":\"9\"},{\"image\":\"data:image\\/svg+xml;base64,PHN2ZyB4bWxucz0iaHR0cDovL3d3dy53My5vcmcvMjAwMC9zdmciIHdpZHRoPSIyMjAiIGhlaWdodD0iMjg0IiB2aWV3Qm94PSIwIDAgMjIwIDI4NCIgcm9sZT0iaW1nIiA+Cjx0aXRsZT5IRVhBTE9DSyBtb2R1bGFyIGludGVyZmFjZSBhc3NldDwvdGl0bGU+CjxkZWZzPjwvZGVmcz4KICAgICAgPHJlY3QgeD0iOCIgeT0iOCIgd2lkdGg9IjIwNCIgaGVpZ2h0PSIyNjgiIHJ4PSIxNCIgZmlsbD0iIzExMUMyMiIgc3Ryb2tlPSIjQjk4NTZFIiBzdHJva2Utd2lkdGg9IjIuNiIvPgogICAgICA8cmVjdCB4PSIxMiIgeT0iMTIiIHdp ...(+3532 chars)\",\"value\":\"10\"},{\"image\":\"data:image\\/svg+xml;base64,PHN2ZyB4bWxucz0iaHR0cDovL3d3dy53My5vcmcvMjAwMC9zdmciIHdpZHRoPSIyMjAiIGhlaWdodD0iMjg0IiB2aWV3Qm94PSIwIDAgMjIwIDI4NCIgcm9sZT0iaW1nIiA+Cjx0aXRsZT5IRVhBTE9DSyBtb2R1bGFyIGludGVyZmFjZSBhc3NldDwvdGl0bGU+CjxkZWZzPjwvZGVmcz4KICAgICAgPHJlY3QgeD0iOCIgeT0iOCIgd2lkdGg9IjIwNCIgaGVpZ2h0PSIyNjgiIHJ4PSIxNCIgZmlsbD0iIzExMUMyMiIgc3Ryb2tlPSIjNTM2NjZFIiBzdHJva2Utd2lkdGg9IjIiLz4KICAgICAgPHJlY3QgeD0iMTIiIHk9IjEyIiB3aWR0 ...(+3220 chars)\",\"value\":\"11\"},{\"image\":\"data:image\\/svg+xml;base64,PHN2ZyB4bWxucz0iaHR0cDovL3d3dy53My5vcmcvMjAwMC9zdmciIHdpZHRoPSIyMjAiIGhlaWdodD0iMjg0IiB2aWV3Qm94PSIwIDAgMjIwIDI4NCIgcm9sZT0iaW1nIiA+Cjx0aXRsZT5IRVhBTE9DSyBtb2R1bGFyIGludGVyZmFjZSBhc3NldDwvdGl0bGU+CjxkZWZzPjxsaW5lYXJHcmFkaWVudCBpZD0ia3JhZnRGcm9udCIgeDE9IjAiIHkxPSIwIiB4Mj0iMSIgeTI9IjEiPjxzdG9wIHN0b3AtY29sb3I9IiNEM0I5OUEiLz48c3RvcCBvZmZzZXQ9IjEiIHN0b3AtY29sb3I9IiNBMzgzNjMiLz48L2xpbmVhckdyYWRpZW50Pjxs ...(+4752 chars)\",\"value\":\"20\"},{\"image\":\"data:image\\/svg+xml;base64,PHN2ZyB4bWxucz0iaHR0cDovL3d3dy53My5vcmcvMjAwMC9zdmciIHdpZHRoPSIyMjAiIGhlaWdodD0iMjg0IiB2aWV3Qm94PSIwIDAgMjIwIDI4NCIgcm9sZT0iaW1nIiA+Cjx0aXRsZT5IRVhBTE9DSyBtb2R1bGFyIGludGVyZmFjZSBhc3NldDwvdGl0bGU+CjxkZWZzPjxsaW5lYXJHcmFkaWVudCBpZD0ia3JhZnRGcm9udCIgeDE9IjAiIHkxPSIwIiB4Mj0iMSIgeTI9IjEiPjxzdG9wIHN0b3AtY29sb3I9IiNEM0I5OUEiLz48c3RvcCBvZmZzZXQ9IjEiIHN0b3AtY29sb3I9IiNBMzgzNjMiLz48L2xpbmVhckdyYWRpZW50Pjxs ...(+7264 chars)\",\"value\":\"21\"},{\"image\":\"data:image\\/svg+xml;base64,PHN2ZyB4bWxucz0iaHR0cDovL3d3dy53My5vcmcvMjAwMC9zdmciIHdpZHRoPSIyMjAiIGhlaWdodD0iMjg0IiB2aWV3Qm94PSIwIDAgMjIwIDI4NCIgcm9sZT0iaW1nIiA+Cjx0aXRsZT5IRVhBTE9DSyBtb2R1bGFyIGludGVyZmFjZSBhc3NldDwvdGl0bGU+CjxkZWZzPjxsaW5lYXJHcmFkaWVudCBpZD0ia3JhZnRGcm9udCIgeDE9IjAiIHkxPSIwIiB4Mj0iMSIgeTI9IjEiPjxzdG9wIHN0b3AtY29sb3I9IiNEM0I5OUEiLz48c3RvcCBvZmZzZXQ9IjEiIHN0b3AtY29sb3I9IiNBMzgzNjMiLz48L2xpbmVhckdyYWRpZW50Pjxs ...(+7264 chars)\",\"value\":\"22\"},{\"image\":\"data:image\\/svg+xml;base64,PHN2ZyB4bWxucz0iaHR0cDovL3d3dy53My5vcmcvMjAwMC9zdmciIHdpZHRoPSIyMjAiIGhlaWdodD0iMjg0IiB2aWV3Qm94PSIwIDAgMjIwIDI4NCIgcm9sZT0iaW1nIiA+Cjx0aXRsZT5IRVhBTE9DSyBtb2R1bGFyIGludGVyZmFjZSBhc3NldDwvdGl0bGU+CjxkZWZzPjxsaW5lYXJHcmFkaWVudCBpZD0ia3JhZnRGcm9udCIgeDE9IjAiIHkxPSIwIiB4Mj0iMSIgeTI9IjEiPjxzdG9wIHN0b3AtY29sb3I9IiNEM0I5OUEiLz48c3RvcCBvZmZzZXQ9IjEiIHN0b3AtY29sb3I9IiNBMzgzNjMiLz48L2xpbmVhckdyYWRpZW50Pjxs ...(+7264 chars)\",\"value\":\"23\"},{\"image\":\"data:image\\/svg+xml;base64,PHN2ZyB4bWxucz0iaHR0cDovL3d3dy53My5vcmcvMjAwMC9zdmciIHdpZHRoPSIyMjAiIGhlaWdodD0iMjg0IiB2aWV3Qm94PSIwIDAgMjIwIDI4NCIgcm9sZT0iaW1nIiA+Cjx0aXRsZT5IRVhBTE9DSyBtb2R1bGFyIGludGVyZmFjZSBhc3NldDwvdGl0bGU+CjxkZWZzPjxsaW5lYXJHcmFkaWVudCBpZD0ia3JhZnRGcm9udCIgeDE9IjAiIHkxPSIwIiB4Mj0iMSIgeTI9IjEiPjxzdG9wIHN0b3AtY29sb3I9IiNEM0I5OUEiLz48c3RvcCBvZmZzZXQ9IjEiIHN0b3AtY29sb3I9IiNBMzgzNjMiLz48L2xpbmVhckdyYWRpZW50Pjxs ...(+7260 chars)\",\"value\":\"24\"},{\"image\":\"data:image\\/svg+xml;base64,PHN2ZyB4bWxucz0iaHR0cDovL3d3dy53My5vcmcvMjAwMC9zdmciIHdpZHRoPSIyMjAiIGhlaWdodD0iMjg0IiB2aWV3Qm94PSIwIDAgMjIwIDI4NCIgcm9sZT0iaW1nIiA+Cjx0aXRsZT5IRVhBTE9DSyBtb2R1bGFyIGludGVyZmFjZSBhc3NldDwvdGl0bGU+CjxkZWZzPjxsaW5lYXJHcmFkaWVudCBpZD0ia3JhZnRGcm9udCIgeDE9IjAiIHkxPSIwIiB4Mj0iMSIgeTI9IjEiPjxzdG9wIHN0b3AtY29sb3I9IiNEM0I5OUEiLz48c3RvcCBvZmZzZXQ9IjEiIHN0b3AtY29sb3I9IiNBMzgzNjMiLz48L2xpbmVhckdyYWRpZW50Pjxs ...(+7264 chars)\",\"value\":\"25\"},{\"image\":\"data:image\\/svg+xml;base64,PHN2ZyB4bWxucz0iaHR0cDovL3d3dy53My5vcmcvMjAwMC9zdmciIHdpZHRoPSIyMjAiIGhlaWdodD0iMjg0IiB2aWV3Qm94PSIwIDAgMjIwIDI4NCIgcm9sZT0iaW1nIiA+Cjx0aXRsZT5IRVhBTE9DSyBtb2R1bGFyIGludGVyZmFjZSBhc3NldDwvdGl0bGU+CjxkZWZzPjxsaW5lYXJHcmFkaWVudCBpZD0ia3JhZnRGcm9udCIgeDE9IjAiIHkxPSIwIiB4Mj0iMSIgeTI9IjEiPjxzdG9wIHN0b3AtY29sb3I9IiNEM0I5OUEiLz48c3RvcCBvZmZzZXQ9IjEiIHN0b3AtY29sb3I9IiNBMzgzNjMiLz48L2xpbmVhckdyYWRpZW50Pjxs ...(+7272 chars)\",\"value\":\"26\"},{\"image\":\"data:image\\/svg+xml;base64,PHN2ZyB4bWxucz0iaHR0cDovL3d3dy53My5vcmcvMjAwMC9zdmciIHdpZHRoPSIyMjAiIGhlaWdodD0iMjg0IiB2aWV3Qm94PSIwIDAgMjIwIDI4NCIgcm9sZT0iaW1nIiA+Cjx0aXRsZT5IRVhBTE9DSyBtb2R1bGFyIGludGVyZmFjZSBhc3NldDwvdGl0bGU+CjxkZWZzPjxsaW5lYXJHcmFkaWVudCBpZD0ia3JhZnRGcm9udCIgeDE9IjAiIHkxPSIwIiB4Mj0iMSIgeTI9IjEiPjxzdG9wIHN0b3AtY29sb3I9IiNEM0I5OUEiLz48c3RvcCBvZmZzZXQ9IjEiIHN0b3AtY29sb3I9IiNBMzgzNjMiLz48L2xpbmVhckdyYWRpZW50Pjxs ...(+7264 chars)\",\"value\":\"27\"},{\"image\":\"data:image\\/svg+xml;base64,PHN2ZyB4bWxucz0iaHR0cDovL3d3dy53My5vcmcvMjAwMC9zdmciIHdpZHRoPSIyMjAiIGhlaWdodD0iMjg0IiB2aWV3Qm94PSIwIDAgMjIwIDI4NCIgcm9sZT0iaW1nIiA+Cjx0aXRsZT5IRVhBTE9DSyBtb2R1bGFyIGludGVyZmFjZSBhc3NldDwvdGl0bGU+CjxkZWZzPjxsaW5lYXJHcmFkaWVudCBpZD0ia3JhZnRGcm9udCIgeDE9IjAiIHkxPSIwIiB4Mj0iMSIgeTI9IjEiPjxzdG9wIHN0b3AtY29sb3I9IiNEM0I5OUEiLz48c3RvcCBvZmZzZXQ9IjEiIHN0b3AtY29sb3I9IiNBMzgzNjMiLz48L2xpbmVhckdyYWRpZW50Pjxs ...(+7268 chars)\",\"value\":\"28\"},{\"image\":\"data:image\\/svg+xml;base64,PHN2ZyB4bWxucz0iaHR0cDovL3d3dy53My5vcmcvMjAwMC9zdmciIHdpZHRoPSIyMjAiIGhlaWdodD0iMjg0IiB2aWV3Qm94PSIwIDAgMjIwIDI4NCIgcm9sZT0iaW1nIiA+Cjx0aXRsZT5IRVhBTE9DSyBtb2R1bGFyIGludGVyZmFjZSBhc3NldDwvdGl0bGU+CjxkZWZzPjxsaW5lYXJHcmFkaWVudCBpZD0ia3JhZnRGcm9udCIgeDE9IjAiIHkxPSIwIiB4Mj0iMSIgeTI9IjEiPjxzdG9wIHN0b3AtY29sb3I9IiNEM0I5OUEiLz48c3RvcCBvZmZzZXQ9IjEiIHN0b3AtY29sb3I9IiNBMzgzNjMiLz48L2xpbmVhckdyYWRpZW50Pjxs ...(+7268 chars)\",\"value\":\"29\"},{\"image\":\"data:image\\/svg+xml;base64,PHN2ZyB4bWxucz0iaHR0cDovL3d3dy53My5vcmcvMjAwMC9zdmciIHdpZHRoPSIyMjAiIGhlaWdodD0iMjg0IiB2aWV3Qm94PSIwIDAgMjIwIDI4NCIgcm9sZT0iaW1nIiA+Cjx0aXRsZT5IRVhBTE9DSyBtb2R1bGFyIGludGVyZmFjZSBhc3NldDwvdGl0bGU+CjxkZWZzPjxsaW5lYXJHcmFkaWVudCBpZD0ia3JhZnRGcm9udCIgeDE9IjAiIHkxPSIwIiB4Mj0iMSIgeTI9IjEiPjxzdG9wIHN0b3AtY29sb3I9IiNEM0I5OUEiLz48c3RvcCBvZmZzZXQ9IjEiIHN0b3AtY29sb3I9IiNBMzgzNjMiLz48L2xpbmVhckdyYWRpZW50Pjxs ...(+7268 chars)\",\"value\":\"30\"},{\"image\":\"data:image\\/svg+xml;base64,PHN2ZyB4bWxucz0iaHR0cDovL3d3dy53My5vcmcvMjAwMC9zdmciIHdpZHRoPSIyMjAiIGhlaWdodD0iMjg0IiB2aWV3Qm94PSIwIDAgMjIwIDI4NCIgcm9sZT0iaW1nIiA+Cjx0aXRsZT5IRVhBTE9DSyBtb2R1bGFyIGludGVyZmFjZSBhc3NldDwvdGl0bGU+CjxkZWZzPjxsaW5lYXJHcmFkaWVudCBpZD0ia3JhZnRGcm9udCIgeDE9IjAiIHkxPSIwIiB4Mj0iMSIgeTI9IjEiPjxzdG9wIHN0b3AtY29sb3I9IiNEM0I5OUEiLz48c3RvcCBvZmZzZXQ9IjEiIHN0b3AtY29sb3I9IiNBMzgzNjMiLz48L2xpbmVhckdyYWRpZW50Pjxs ...(+4756 chars)\",\"value\":\"31\"},{\"image\":\"data:image\\/svg+xml;base64,PHN2ZyB4bWxucz0iaHR0cDovL3d3dy53My5vcmcvMjAwMC9zdmciIHdpZHRoPSIyMjAiIGhlaWdodD0iMjg0IiB2aWV3Qm94PSIwIDAgMjIwIDI4NCIgcm9sZT0iaW1nIiA+Cjx0aXRsZT5IRVhBTE9DSyBtb2R1bGFyIGludGVyZmFjZSBhc3NldDwvdGl0bGU+CjxkZWZzPjxsaW5lYXJHcmFkaWVudCBpZD0ia3JhZnRGcm9udCIgeDE9IjAiIHkxPSIwIiB4Mj0iMSIgeTI9IjEiPjxzdG9wIHN0b3AtY29sb3I9IiNEM0I5OUEiLz48c3RvcCBvZmZzZXQ9IjEiIHN0b3AtY29sb3I9IiNBMzgzNjMiLz48L2xpbmVhckdyYWRpZW50Pjxs ...(+4752 chars)\",\"value\":\"32\"},{\"image\":\"data:image\\/svg+xml;base64,PHN2ZyB4bWxucz0iaHR0cDovL3d3dy53My5vcmcvMjAwMC9zdmciIHdpZHRoPSIyMjAiIGhlaWdodD0iMjg0IiB2aWV3Qm94PSIwIDAgMjIwIDI4NCIgcm9sZT0iaW1nIiA+Cjx0aXRsZT5IRVhBTE9DSyBtb2R1bGFyIGludGVyZmFjZSBhc3NldDwvdGl0bGU+CjxkZWZzPjxsaW5lYXJHcmFkaWVudCBpZD0ia3JhZnRGcm9udCIgeDE9IjAiIHkxPSIwIiB4Mj0iMSIgeTI9IjEiPjxzdG9wIHN0b3AtY29sb3I9IiNEM0I5OUEiLz48c3RvcCBvZmZzZXQ9IjEiIHN0b3AtY29sb3I9IiNBMzgzNjMiLz48L2xpbmVhckdyYWRpZW50Pjxs ...(+6860 chars)\",\"value\":\"33\"},{\"image\":\"data:image\\/svg+xml;base64,PHN2ZyB4bWxucz0iaHR0cDovL3d3dy53My5vcmcvMjAwMC9zdmciIHdpZHRoPSIyMjAiIGhlaWdodD0iMjg0IiB2aWV3Qm94PSIwIDAgMjIwIDI4NCIgcm9sZT0iaW1nIiA+Cjx0aXRsZT5IRVhBTE9DSyBtb2R1bGFyIGludGVyZmFjZSBhc3NldDwvdGl0bGU+CjxkZWZzPjxsaW5lYXJHcmFkaWVudCBpZD0ia3JhZnRGcm9udCIgeDE9IjAiIHkxPSIwIiB4Mj0iMSIgeTI9IjEiPjxzdG9wIHN0b3AtY29sb3I9IiNEM0I5OUEiLz48c3RvcCBvZmZzZXQ9IjEiIHN0b3AtY29sb3I9IiNBMzgzNjMiLz48L2xpbmVhckdyYWRpZW50Pjxs ...(+6860 chars)\",\"value\":\"34\"},{\"image\":\"data:image\\/svg+xml;base64,PHN2ZyB4bWxucz0iaHR0cDovL3d3dy53My5vcmcvMjAwMC9zdmciIHdpZHRoPSIyMjAiIGhlaWdodD0iMjg0IiB2aWV3Qm94PSIwIDAgMjIwIDI4NCIgcm9sZT0iaW1nIiA+Cjx0aXRsZT5IRVhBTE9DSyBtb2R1bGFyIGludGVyZmFjZSBhc3NldDwvdGl0bGU+CjxkZWZzPjxsaW5lYXJHcmFkaWVudCBpZD0ia3JhZnRGcm9udCIgeDE9IjAiIHkxPSIwIiB4Mj0iMSIgeTI9IjEiPjxzdG9wIHN0b3AtY29sb3I9IiNEM0I5OUEiLz48c3RvcCBvZmZzZXQ9IjEiIHN0b3AtY29sb3I9IiNBMzgzNjMiLz48L2xpbmVhckdyYWRpZW50Pjxs ...(+6860 chars)\",\"value\":\"35\"},{\"image\":\"data:image\\/svg+xml;base64,PHN2ZyB4bWxucz0iaHR0cDovL3d3dy53My5vcmcvMjAwMC9zdmciIHdpZHRoPSIyMjAiIGhlaWdodD0iMjg0IiB2aWV3Qm94PSIwIDAgMjIwIDI4NCIgcm9sZT0iaW1nIiA+DQo8dGl0bGU+SEVYQUxPQ0sgbW9kdWxhciBpbnRlcmZhY2UgYXNzZXQ8L3RpdGxlPg0KPGRlZnM+PGxpbmVhckdyYWRpZW50IGlkPSJrcmFmdEZyb250IiB4MT0iMCIgeTE9IjAiIHgyPSIxIiB5Mj0iMSI+PHN0b3Agc3RvcC1jb2xvcj0iI0QzQjk5QSIvPjxzdG9wIG9mZnNldD0iMSIgc3RvcC1jb2xvcj0iI0EzODM2MyIvPjwvbGluZWFyR3JhZGllbnQ+ ...(+6912 chars)\",\"value\":\"36\"},{\"image\":\"data:image\\/svg+xml;base64,PHN2ZyB4bWxucz0iaHR0cDovL3d3dy53My5vcmcvMjAwMC9zdmciIHdpZHRoPSIyMjAiIGhlaWdodD0iMjg0IiB2aWV3Qm94PSIwIDAgMjIwIDI4NCIgcm9sZT0iaW1nIiA+DQo8dGl0bGU+SEVYQUxPQ0sgbW9kdWxhciBpbnRlcmZhY2UgYXNzZXQ8L3RpdGxlPg0KPGRlZnM+PGxpbmVhckdyYWRpZW50IGlkPSJrcmFmdEZyb250IiB4MT0iMCIgeTE9IjAiIHgyPSIxIiB5Mj0iMSI+PHN0b3Agc3RvcC1jb2xvcj0iI0QzQjk5QSIvPjxzdG9wIG9mZnNldD0iMSIgc3RvcC1jb2xvcj0iI0EzODM2MyIvPjwvbGluZWFyR3JhZGllbnQ+ ...(+6912 chars)\",\"value\":\"37\"},{\"image\":\"data:image\\/svg+xml;base64,PHN2ZyB4bWxucz0iaHR0cDovL3d3dy53My5vcmcvMjAwMC9zdmciIHdpZHRoPSIyMjAiIGhlaWdodD0iMjg0IiB2aWV3Qm94PSIwIDAgMjIwIDI4NCIgcm9sZT0iaW1nIiA+DQo8dGl0bGU+SEVYQUxPQ0sgbW9kdWxhciBpbnRlcmZhY2UgYXNzZXQ8L3RpdGxlPg0KPGRlZnM+PGxpbmVhckdyYWRpZW50IGlkPSJrcmFmdEZyb250IiB4MT0iMCIgeTE9IjAiIHgyPSIxIiB5Mj0iMSI+PHN0b3Agc3RvcC1jb2xvcj0iI0QzQjk5QSIvPjxzdG9wIG9mZnNldD0iMSIgc3RvcC1jb2xvcj0iI0EzODM2MyIvPjwvbGluZWFyR3JhZGllbnQ+ ...(+6912 chars)\",\"value\":\"38\"}],\"fixedAspectRatio\":\"on\"}},\"settings\":{\"BindingType\":\"signal\",\"backgroundColor\":[0,0,0],\"backgroundOffset\":0.14,\"backgroundOpacity\":1,\"blockOrientation\":\"Right\",\"fixedAspectRatio\":\"on\",\"showBackgroundColor\":false,\"value\":0,\"version\":\"R2026b\"},\"type\":\"MultistateImage\"}"
  MultiStateImage7 : CustomWebBlock  LabelPosition=Hide  ShowInitialText=on  Configuration="{\"components\":[{\"name\":\"BackgroundImageComponent\",\"settings\":{\"image\":{\"size\":[0,0],\"src\":\"default\",\"srcOrientation\":\"Right\"},\"position\":[0,0,1,1],\"scaleMode\":\"0\"}},{\"name\":\"MultistateImageStateComponent\",\"settings\":{\"applyDefaults\":true,\"position\":[0,0,1,1],\"states\":[{\"image\":{\"size\":[0.7746478873239436,1],\"src\":\"data:image\\/svg+xml;base64,PHN2ZyB4bWxucz0iaHR0cDovL3d3dy53My5vcmcvMjAwMC9zdmciIHdpZHRoPSIyMjAiIGhlaWdodD0iMjg0IiB2aWV3Qm94PSIwIDAgMjIwIDI4NCIgcm9sZT0iaW1nIiA+Cjx0aXRsZT5IRVhBTE9DSyBtb2R1bGFyIGludGVyZmFjZSBhc3NldDwvdGl0bGU+CjxkZWZzPjwvZGVmcz4KICAgICAgPHJlY3QgeD0iOCIgeT0iOCIgd2lkdGg9IjIwNCIgaGVpZ2h0PSIyNjgiIHJ4PSIxNCIgZmlsbD0iIzExMUMyMiIgc3Ryb2tlPSIjNTM2NjZFIiBzdHJva2Utd2lkdGg9IjIiLz4KICAgICAgPHJlY3QgeD0iMTIiIHk9IjEyIiB3aWR0 ...(+3224 chars)\",\"srcOrientation\":\"Right\"},\"position\":[0,0,1,1],\"value\":[]},{\"image\":{\"size\":[0,0],\"src\":\"data:image\\/svg+xml;base64,PHN2ZyB4bWxucz0iaHR0cDovL3d3dy53My5vcmcvMjAwMC9zdmciIHdpZHRoPSIyMjAiIGhlaWdodD0iMjg0IiB2aWV3Qm94PSIwIDAgMjIwIDI4NCIgcm9sZT0iaW1nIiA+Cjx0aXRsZT5IRVhBTE9DSyBtb2R1bGFyIGludGVyZmFjZSBhc3NldDwvdGl0bGU+CjxkZWZzPjwvZGVmcz4KICAgICAgPHJlY3QgeD0iOCIgeT0iOCIgd2lkdGg9IjIwNCIgaGVpZ2h0PSIyNjgiIHJ4PSIxNCIgZmlsbD0iIzExMUMyMiIgc3Ryb2tlPSIjNTM2NjZFIiBzdHJva2Utd2lkdGg9IjIiLz4KICAgICAgPHJlY3QgeD0iMTIiIHk9IjEyIiB3aWR0 ...(+3224 chars)\",\"srcOrientation\":\"Right\"},\"position\":[0,0,1,1],\"value\":\"0\"},{\"image\":{\"size\":[0,0],\"src\":\"data:image\\/svg+xml;base64,PHN2ZyB4bWxucz0iaHR0cDovL3d3dy53My5vcmcvMjAwMC9zdmciIHdpZHRoPSIyMjAiIGhlaWdodD0iMjg0IiB2aWV3Qm94PSIwIDAgMjIwIDI4NCIgcm9sZT0iaW1nIiA+Cjx0aXRsZT5IRVhBTE9DSyBtb2R1bGFyIGludGVyZmFjZSBhc3NldDwvdGl0bGU+CjxkZWZzPjwvZGVmcz4KICAgICAgPHJlY3QgeD0iOCIgeT0iOCIgd2lkdGg9IjIwNCIgaGVpZ2h0PSIyNjgiIHJ4PSIxNCIgZmlsbD0iIzExMUMyMiIgc3Ryb2tlPSIjNTM2NjZFIiBzdHJva2Utd2lkdGg9IjIiLz4KICAgICAgPHJlY3QgeD0iMTIiIHk9IjEyIiB3aWR0 ...(+3220 chars)\",\"srcOrientation\":\"Right\"},\"position\":[0,0,1,1],\"value\":\"1\"},{\"image\":{\"size\":[0,0],\"src\":\"data:image\\/svg+xml;base64,PHN2ZyB4bWxucz0iaHR0cDovL3d3dy53My5vcmcvMjAwMC9zdmciIHdpZHRoPSIyMjAiIGhlaWdodD0iMjg0IiB2aWV3Qm94PSIwIDAgMjIwIDI4NCIgcm9sZT0iaW1nIiA+Cjx0aXRsZT5IRVhBTE9DSyBtb2R1bGFyIGludGVyZmFjZSBhc3NldDwvdGl0bGU+CjxkZWZzPjwvZGVmcz4KICAgICAgPHJlY3QgeD0iOCIgeT0iOCIgd2lkdGg9IjIwNCIgaGVpZ2h0PSIyNjgiIHJ4PSIxNCIgZmlsbD0iIzExMUMyMiIgc3Ryb2tlPSIjQjk4NTZFIiBzdHJva2Utd2lkdGg9IjIuNiIvPgogICAgICA8cmVjdCB4PSIxMiIgeT0iMTIiIHdp ...(+3488 chars)\",\"srcOrientation\":\"Right\"},\"position\":[0,0,1,1],\"value\":\"2\"},{\"image\":{\"size\":[0,0],\"src\":\"data:image\\/svg+xml;base64,PHN2ZyB4bWxucz0iaHR0cDovL3d3dy53My5vcmcvMjAwMC9zdmciIHdpZHRoPSIyMjAiIGhlaWdodD0iMjg0IiB2aWV3Qm94PSIwIDAgMjIwIDI4NCIgcm9sZT0iaW1nIiA+Cjx0aXRsZT5IRVhBTE9DSyBtb2R1bGFyIGludGVyZmFjZSBhc3NldDwvdGl0bGU+CjxkZWZzPjwvZGVmcz4KICAgICAgPHJlY3QgeD0iOCIgeT0iOCIgd2lkdGg9IjIwNCIgaGVpZ2h0PSIyNjgiIHJ4PSIxNCIgZmlsbD0iIzExMUMyMiIgc3Ryb2tlPSIjQjk4NTZFIiBzdHJva2Utd2lkdGg9IjIuNiIvPgogICAgICA8cmVjdCB4PSIxMiIgeT0iMTIiIHdp ...(+3484 chars)\",\"srcOrientation\":\"Right\"},\"position\":[0,0,1,1],\"value\":\"3\"},{\"image\":{\"size\":[0,0],\"src\":\"data:image\\/svg+xml;base64,PHN2ZyB4bWxucz0iaHR0cDovL3d3dy53My5vcmcvMjAwMC9zdmciIHdpZHRoPSIyMjAiIGhlaWdodD0iMjg0IiB2aWV3Qm94PSIwIDAgMjIwIDI4NCIgcm9sZT0iaW1nIiA+Cjx0aXRsZT5IRVhBTE9DSyBtb2R1bGFyIGludGVyZmFjZSBhc3NldDwvdGl0bGU+CjxkZWZzPjwvZGVmcz4KICAgICAgPHJlY3QgeD0iOCIgeT0iOCIgd2lkdGg9IjIwNCIgaGVpZ2h0PSIyNjgiIHJ4PSIxNCIgZmlsbD0iIzExMUMyMiIgc3Ryb2tlPSIjQjk4NTZFIiBzdHJva2Utd2lkdGg9IjIuNiIvPgogICAgICA8cmVjdCB4PSIxMiIgeT0iMTIiIHdp ...(+3532 chars)\",\"srcOrientation\":\"Right\"},\"position\":[0,0,1,1],\"value\":\"4\"},{\"image\":{\"size\":[0,0],\"src\":\"data:image\\/svg+xml;base64,PHN2ZyB4bWxucz0iaHR0cDovL3d3dy53My5vcmcvMjAwMC9zdmciIHdpZHRoPSIyMjAiIGhlaWdodD0iMjg0IiB2aWV3Qm94PSIwIDAgMjIwIDI4NCIgcm9sZT0iaW1nIiA+Cjx0aXRsZT5IRVhBTE9DSyBtb2R1bGFyIGludGVyZmFjZSBhc3NldDwvdGl0bGU+CjxkZWZzPjwvZGVmcz4KICAgICAgPHJlY3QgeD0iOCIgeT0iOCIgd2lkdGg9IjIwNCIgaGVpZ2h0PSIyNjgiIHJ4PSIxNCIgZmlsbD0iIzExMUMyMiIgc3Ryb2tlPSIjQjk4NTZFIiBzdHJva2Utd2lkdGg9IjIuNiIvPgogICAgICA8cmVjdCB4PSIxMiIgeT0iMTIiIHdp ...(+3532 chars)\",\"srcOrientation\":\"Right\"},\"position\":[0,0,1,1],\"value\":\"5\"},{\"image\":{\"size\":[0,0],\"src\":\"data:image\\/svg+xml;base64,PHN2ZyB4bWxucz0iaHR0cDovL3d3dy53My5vcmcvMjAwMC9zdmciIHdpZHRoPSIyMjAiIGhlaWdodD0iMjg0IiB2aWV3Qm94PSIwIDAgMjIwIDI4NCIgcm9sZT0iaW1nIiA+Cjx0aXRsZT5IRVhBTE9DSyBtb2R1bGFyIGludGVyZmFjZSBhc3NldDwvdGl0bGU+CjxkZWZzPjwvZGVmcz4KICAgICAgPHJlY3QgeD0iOCIgeT0iOCIgd2lkdGg9IjIwNCIgaGVpZ2h0PSIyNjgiIHJ4PSIxNCIgZmlsbD0iIzExMUMyMiIgc3Ryb2tlPSIjQjk4NTZFIiBzdHJva2Utd2lkdGg9IjIuNiIvPgogICAgICA8cmVjdCB4PSIxMiIgeT0iMTIiIHdp ...(+3532 chars)\",\"srcOrientation\":\"Right\"},\"position\":[0,0,1,1],\"value\":\"6\"},{\"image\":{\"size\":[0,0],\"src\":\"data:image\\/svg+xml;base64,PHN2ZyB4bWxucz0iaHR0cDovL3d3dy53My5vcmcvMjAwMC9zdmciIHdpZHRoPSIyMjAiIGhlaWdodD0iMjg0IiB2aWV3Qm94PSIwIDAgMjIwIDI4NCIgcm9sZT0iaW1nIiA+Cjx0aXRsZT5IRVhBTE9DSyBtb2R1bGFyIGludGVyZmFjZSBhc3NldDwvdGl0bGU+CjxkZWZzPjwvZGVmcz4KICAgICAgPHJlY3QgeD0iOCIgeT0iOCIgd2lkdGg9IjIwNCIgaGVpZ2h0PSIyNjgiIHJ4PSIxNCIgZmlsbD0iIzExMUMyMiIgc3Ryb2tlPSIjQjk4NTZFIiBzdHJva2Utd2lkdGg9IjIuNiIvPgogICAgICA8cmVjdCB4PSIxMiIgeT0iMTIiIHdp ...(+3524 chars)\",\"srcOrientation\":\"Right\"},\"position\":[0,0,1,1],\"value\":\"7\"},{\"image\":{\"size\":[0,0],\"src\":\"data:image\\/svg+xml;base64,PHN2ZyB4bWxucz0iaHR0cDovL3d3dy53My5vcmcvMjAwMC9zdmciIHdpZHRoPSIyMjAiIGhlaWdodD0iMjg0IiB2aWV3Qm94PSIwIDAgMjIwIDI4NCIgcm9sZT0iaW1nIiA+Cjx0aXRsZT5IRVhBTE9DSyBtb2R1bGFyIGludGVyZmFjZSBhc3NldDwvdGl0bGU+CjxkZWZzPjwvZGVmcz4KICAgICAgPHJlY3QgeD0iOCIgeT0iOCIgd2lkdGg9IjIwNCIgaGVpZ2h0PSIyNjgiIHJ4PSIxNCIgZmlsbD0iIzExMUMyMiIgc3Ryb2tlPSIjQjk4NTZFIiBzdHJva2Utd2lkdGg9IjIuNiIvPgogICAgICA8cmVjdCB4PSIxMiIgeT0iMTIiIHdp ...(+3532 chars)\",\"srcOrientation\":\"Right\"},\"position\":[0,0,1,1],\"value\":\"8\"},{\"image\":{\"size\":[0,0],\"src\":\"data:image\\/svg+xml;base64,PHN2ZyB4bWxucz0iaHR0cDovL3d3dy53My5vcmcvMjAwMC9zdmciIHdpZHRoPSIyMjAiIGhlaWdodD0iMjg0IiB2aWV3Qm94PSIwIDAgMjIwIDI4NCIgcm9sZT0iaW1nIiA+Cjx0aXRsZT5IRVhBTE9DSyBtb2R1bGFyIGludGVyZmFjZSBhc3NldDwvdGl0bGU+CjxkZWZzPjwvZGVmcz4KICAgICAgPHJlY3QgeD0iOCIgeT0iOCIgd2lkdGg9IjIwNCIgaGVpZ2h0PSIyNjgiIHJ4PSIxNCIgZmlsbD0iIzExMUMyMiIgc3Ryb2tlPSIjQjk4NTZFIiBzdHJva2Utd2lkdGg9IjIuNiIvPgogICAgICA8cmVjdCB4PSIxMiIgeT0iMTIiIHdp ...(+3532 chars)\",\"srcOrientation\":\"Right\"},\"position\":[0,0,1,1],\"value\":\"9\"},{\"image\":{\"size\":[0,0],\"src\":\"data:image\\/svg+xml;base64,PHN2ZyB4bWxucz0iaHR0cDovL3d3dy53My5vcmcvMjAwMC9zdmciIHdpZHRoPSIyMjAiIGhlaWdodD0iMjg0IiB2aWV3Qm94PSIwIDAgMjIwIDI4NCIgcm9sZT0iaW1nIiA+Cjx0aXRsZT5IRVhBTE9DSyBtb2R1bGFyIGludGVyZmFjZSBhc3NldDwvdGl0bGU+CjxkZWZzPjwvZGVmcz4KICAgICAgPHJlY3QgeD0iOCIgeT0iOCIgd2lkdGg9IjIwNCIgaGVpZ2h0PSIyNjgiIHJ4PSIxNCIgZmlsbD0iIzExMUMyMiIgc3Ryb2tlPSIjQjk4NTZFIiBzdHJva2Utd2lkdGg9IjIuNiIvPgogICAgICA8cmVjdCB4PSIxMiIgeT0iMTIiIHdp ...(+3532 chars)\",\"srcOrientation\":\"Right\"},\"position\":[0,0,1,1],\"value\":\"10\"},{\"image\":{\"size\":[0,0],\"src\":\"data:image\\/svg+xml;base64,PHN2ZyB4bWxucz0iaHR0cDovL3d3dy53My5vcmcvMjAwMC9zdmciIHdpZHRoPSIyMjAiIGhlaWdodD0iMjg0IiB2aWV3Qm94PSIwIDAgMjIwIDI4NCIgcm9sZT0iaW1nIiA+Cjx0aXRsZT5IRVhBTE9DSyBtb2R1bGFyIGludGVyZmFjZSBhc3NldDwvdGl0bGU+CjxkZWZzPjwvZGVmcz4KICAgICAgPHJlY3QgeD0iOCIgeT0iOCIgd2lkdGg9IjIwNCIgaGVpZ2h0PSIyNjgiIHJ4PSIxNCIgZmlsbD0iIzExMUMyMiIgc3Ryb2tlPSIjNTM2NjZFIiBzdHJva2Utd2lkdGg9IjIiLz4KICAgICAgPHJlY3QgeD0iMTIiIHk9IjEyIiB3aWR0 ...(+3220 chars)\",\"srcOrientation\":\"Right\"},\"position\":[0,0,1,1],\"value\":\"11\"},{\"image\":{\"size\":[0,0],\"src\":\"data:image\\/svg+xml;base64,PHN2ZyB4bWxucz0iaHR0cDovL3d3dy53My5vcmcvMjAwMC9zdmciIHdpZHRoPSIyMjAiIGhlaWdodD0iMjg0IiB2aWV3Qm94PSIwIDAgMjIwIDI4NCIgcm9sZT0iaW1nIiA+Cjx0aXRsZT5IRVhBTE9DSyBtb2R1bGFyIGludGVyZmFjZSBhc3NldDwvdGl0bGU+CjxkZWZzPjxsaW5lYXJHcmFkaWVudCBpZD0ia3JhZnRGcm9udCIgeDE9IjAiIHkxPSIwIiB4Mj0iMSIgeTI9IjEiPjxzdG9wIHN0b3AtY29sb3I9IiNEM0I5OUEiLz48c3RvcCBvZmZzZXQ9IjEiIHN0b3AtY29sb3I9IiNBMzgzNjMiLz48L2xpbmVhckdyYWRpZW50Pjxs ...(+4752 chars)\",\"srcOrientation\":\"Right\"},\"position\":[0,0,1,1],\"value\":\"20\"},{\"image\":{\"size\":[0,0],\"src\":\"data:image\\/svg+xml;base64,PHN2ZyB4bWxucz0iaHR0cDovL3d3dy53My5vcmcvMjAwMC9zdmciIHdpZHRoPSIyMjAiIGhlaWdodD0iMjg0IiB2aWV3Qm94PSIwIDAgMjIwIDI4NCIgcm9sZT0iaW1nIiA+Cjx0aXRsZT5IRVhBTE9DSyBtb2R1bGFyIGludGVyZmFjZSBhc3NldDwvdGl0bGU+CjxkZWZzPjxsaW5lYXJHcmFkaWVudCBpZD0ia3JhZnRGcm9udCIgeDE9IjAiIHkxPSIwIiB4Mj0iMSIgeTI9IjEiPjxzdG9wIHN0b3AtY29sb3I9IiNEM0I5OUEiLz48c3RvcCBvZmZzZXQ9IjEiIHN0b3AtY29sb3I9IiNBMzgzNjMiLz48L2xpbmVhckdyYWRpZW50Pjxs ...(+7264 chars)\",\"srcOrientation\":\"Right\"},\"position\":[0,0,1,1],\"value\":\"21\"},{\"image\":{\"size\":[0,0],\"src\":\"data:image\\/svg+xml;base64,PHN2ZyB4bWxucz0iaHR0cDovL3d3dy53My5vcmcvMjAwMC9zdmciIHdpZHRoPSIyMjAiIGhlaWdodD0iMjg0IiB2aWV3Qm94PSIwIDAgMjIwIDI4NCIgcm9sZT0iaW1nIiA+Cjx0aXRsZT5IRVhBTE9DSyBtb2R1bGFyIGludGVyZmFjZSBhc3NldDwvdGl0bGU+CjxkZWZzPjxsaW5lYXJHcmFkaWVudCBpZD0ia3JhZnRGcm9udCIgeDE9IjAiIHkxPSIwIiB4Mj0iMSIgeTI9IjEiPjxzdG9wIHN0b3AtY29sb3I9IiNEM0I5OUEiLz48c3RvcCBvZmZzZXQ9IjEiIHN0b3AtY29sb3I9IiNBMzgzNjMiLz48L2xpbmVhckdyYWRpZW50Pjxs ...(+7264 chars)\",\"srcOrientation\":\"Right\"},\"position\":[0,0,1,1],\"value\":\"22\"},{\"image\":{\"size\":[0,0],\"src\":\"data:image\\/svg+xml;base64,PHN2ZyB4bWxucz0iaHR0cDovL3d3dy53My5vcmcvMjAwMC9zdmciIHdpZHRoPSIyMjAiIGhlaWdodD0iMjg0IiB2aWV3Qm94PSIwIDAgMjIwIDI4NCIgcm9sZT0iaW1nIiA+Cjx0aXRsZT5IRVhBTE9DSyBtb2R1bGFyIGludGVyZmFjZSBhc3NldDwvdGl0bGU+CjxkZWZzPjxsaW5lYXJHcmFkaWVudCBpZD0ia3JhZnRGcm9udCIgeDE9IjAiIHkxPSIwIiB4Mj0iMSIgeTI9IjEiPjxzdG9wIHN0b3AtY29sb3I9IiNEM0I5OUEiLz48c3RvcCBvZmZzZXQ9IjEiIHN0b3AtY29sb3I9IiNBMzgzNjMiLz48L2xpbmVhckdyYWRpZW50Pjxs ...(+7264 chars)\",\"srcOrientation\":\"Right\"},\"position\":[0,0,1,1],\"value\":\"23\"},{\"image\":{\"size\":[0,0],\"src\":\"data:image\\/svg+xml;base64,PHN2ZyB4bWxucz0iaHR0cDovL3d3dy53My5vcmcvMjAwMC9zdmciIHdpZHRoPSIyMjAiIGhlaWdodD0iMjg0IiB2aWV3Qm94PSIwIDAgMjIwIDI4NCIgcm9sZT0iaW1nIiA+Cjx0aXRsZT5IRVhBTE9DSyBtb2R1bGFyIGludGVyZmFjZSBhc3NldDwvdGl0bGU+CjxkZWZzPjxsaW5lYXJHcmFkaWVudCBpZD0ia3JhZnRGcm9udCIgeDE9IjAiIHkxPSIwIiB4Mj0iMSIgeTI9IjEiPjxzdG9wIHN0b3AtY29sb3I9IiNEM0I5OUEiLz48c3RvcCBvZmZzZXQ9IjEiIHN0b3AtY29sb3I9IiNBMzgzNjMiLz48L2xpbmVhckdyYWRpZW50Pjxs ...(+7260 chars)\",\"srcOrientation\":\"Right\"},\"position\":[0,0,1,1],\"value\":\"24\"},{\"image\":{\"size\":[0,0],\"src\":\"data:image\\/svg+xml;base64,PHN2ZyB4bWxucz0iaHR0cDovL3d3dy53My5vcmcvMjAwMC9zdmciIHdpZHRoPSIyMjAiIGhlaWdodD0iMjg0IiB2aWV3Qm94PSIwIDAgMjIwIDI4NCIgcm9sZT0iaW1nIiA+Cjx0aXRsZT5IRVhBTE9DSyBtb2R1bGFyIGludGVyZmFjZSBhc3NldDwvdGl0bGU+CjxkZWZzPjxsaW5lYXJHcmFkaWVudCBpZD0ia3JhZnRGcm9udCIgeDE9IjAiIHkxPSIwIiB4Mj0iMSIgeTI9IjEiPjxzdG9wIHN0b3AtY29sb3I9IiNEM0I5OUEiLz48c3RvcCBvZmZzZXQ9IjEiIHN0b3AtY29sb3I9IiNBMzgzNjMiLz48L2xpbmVhckdyYWRpZW50Pjxs ...(+7264 chars)\",\"srcOrientation\":\"Right\"},\"position\":[0,0,1,1],\"value\":\"25\"},{\"image\":{\"size\":[0,0],\"src\":\"data:image\\/svg+xml;base64,PHN2ZyB4bWxucz0iaHR0cDovL3d3dy53My5vcmcvMjAwMC9zdmciIHdpZHRoPSIyMjAiIGhlaWdodD0iMjg0IiB2aWV3Qm94PSIwIDAgMjIwIDI4NCIgcm9sZT0iaW1nIiA+Cjx0aXRsZT5IRVhBTE9DSyBtb2R1bGFyIGludGVyZmFjZSBhc3NldDwvdGl0bGU+CjxkZWZzPjxsaW5lYXJHcmFkaWVudCBpZD0ia3JhZnRGcm9udCIgeDE9IjAiIHkxPSIwIiB4Mj0iMSIgeTI9IjEiPjxzdG9wIHN0b3AtY29sb3I9IiNEM0I5OUEiLz48c3RvcCBvZmZzZXQ9IjEiIHN0b3AtY29sb3I9IiNBMzgzNjMiLz48L2xpbmVhckdyYWRpZW50Pjxs ...(+7272 chars)\",\"srcOrientation\":\"Right\"},\"position\":[0,0,1,1],\"value\":\"26\"},{\"image\":{\"size\":[0,0],\"src\":\"data:image\\/svg+xml;base64,PHN2ZyB4bWxucz0iaHR0cDovL3d3dy53My5vcmcvMjAwMC9zdmciIHdpZHRoPSIyMjAiIGhlaWdodD0iMjg0IiB2aWV3Qm94PSIwIDAgMjIwIDI4NCIgcm9sZT0iaW1nIiA+Cjx0aXRsZT5IRVhBTE9DSyBtb2R1bGFyIGludGVyZmFjZSBhc3NldDwvdGl0bGU+CjxkZWZzPjxsaW5lYXJHcmFkaWVudCBpZD0ia3JhZnRGcm9udCIgeDE9IjAiIHkxPSIwIiB4Mj0iMSIgeTI9IjEiPjxzdG9wIHN0b3AtY29sb3I9IiNEM0I5OUEiLz48c3RvcCBvZmZzZXQ9IjEiIHN0b3AtY29sb3I9IiNBMzgzNjMiLz48L2xpbmVhckdyYWRpZW50Pjxs ...(+7264 chars)\",\"srcOrientation\":\"Right\"},\"position\":[0,0,1,1],\"value\":\"27\"},{\"image\":{\"size\":[0,0],\"src\":\"data:image\\/svg+xml;base64,PHN2ZyB4bWxucz0iaHR0cDovL3d3dy53My5vcmcvMjAwMC9zdmciIHdpZHRoPSIyMjAiIGhlaWdodD0iMjg0IiB2aWV3Qm94PSIwIDAgMjIwIDI4NCIgcm9sZT0iaW1nIiA+Cjx0aXRsZT5IRVhBTE9DSyBtb2R1bGFyIGludGVyZmFjZSBhc3NldDwvdGl0bGU+CjxkZWZzPjxsaW5lYXJHcmFkaWVudCBpZD0ia3JhZnRGcm9udCIgeDE9IjAiIHkxPSIwIiB4Mj0iMSIgeTI9IjEiPjxzdG9wIHN0b3AtY29sb3I9IiNEM0I5OUEiLz48c3RvcCBvZmZzZXQ9IjEiIHN0b3AtY29sb3I9IiNBMzgzNjMiLz48L2xpbmVhckdyYWRpZW50Pjxs ...(+7268 chars)\",\"srcOrientation\":\"Right\"},\"position\":[0,0,1,1],\"value\":\"28\"},{\"image\":{\"size\":[0,0],\"src\":\"data:image\\/svg+xml;base64,PHN2ZyB4bWxucz0iaHR0cDovL3d3dy53My5vcmcvMjAwMC9zdmciIHdpZHRoPSIyMjAiIGhlaWdodD0iMjg0IiB2aWV3Qm94PSIwIDAgMjIwIDI4NCIgcm9sZT0iaW1nIiA+Cjx0aXRsZT5IRVhBTE9DSyBtb2R1bGFyIGludGVyZmFjZSBhc3NldDwvdGl0bGU+CjxkZWZzPjxsaW5lYXJHcmFkaWVudCBpZD0ia3JhZnRGcm9udCIgeDE9IjAiIHkxPSIwIiB4Mj0iMSIgeTI9IjEiPjxzdG9wIHN0b3AtY29sb3I9IiNEM0I5OUEiLz48c3RvcCBvZmZzZXQ9IjEiIHN0b3AtY29sb3I9IiNBMzgzNjMiLz48L2xpbmVhckdyYWRpZW50Pjxs ...(+7268 chars)\",\"srcOrientation\":\"Right\"},\"position\":[0,0,1,1],\"value\":\"29\"},{\"image\":{\"size\":[0,0],\"src\":\"data:image\\/svg+xml;base64,PHN2ZyB4bWxucz0iaHR0cDovL3d3dy53My5vcmcvMjAwMC9zdmciIHdpZHRoPSIyMjAiIGhlaWdodD0iMjg0IiB2aWV3Qm94PSIwIDAgMjIwIDI4NCIgcm9sZT0iaW1nIiA+Cjx0aXRsZT5IRVhBTE9DSyBtb2R1bGFyIGludGVyZmFjZSBhc3NldDwvdGl0bGU+CjxkZWZzPjxsaW5lYXJHcmFkaWVudCBpZD0ia3JhZnRGcm9udCIgeDE9IjAiIHkxPSIwIiB4Mj0iMSIgeTI9IjEiPjxzdG9wIHN0b3AtY29sb3I9IiNEM0I5OUEiLz48c3RvcCBvZmZzZXQ9IjEiIHN0b3AtY29sb3I9IiNBMzgzNjMiLz48L2xpbmVhckdyYWRpZW50Pjxs ...(+7268 chars)\",\"srcOrientation\":\"Right\"},\"position\":[0,0,1,1],\"value\":\"30\"},{\"image\":{\"size\":[0,0],\"src\":\"data:image\\/svg+xml;base64,PHN2ZyB4bWxucz0iaHR0cDovL3d3dy53My5vcmcvMjAwMC9zdmciIHdpZHRoPSIyMjAiIGhlaWdodD0iMjg0IiB2aWV3Qm94PSIwIDAgMjIwIDI4NCIgcm9sZT0iaW1nIiA+Cjx0aXRsZT5IRVhBTE9DSyBtb2R1bGFyIGludGVyZmFjZSBhc3NldDwvdGl0bGU+CjxkZWZzPjxsaW5lYXJHcmFkaWVudCBpZD0ia3JhZnRGcm9udCIgeDE9IjAiIHkxPSIwIiB4Mj0iMSIgeTI9IjEiPjxzdG9wIHN0b3AtY29sb3I9IiNEM0I5OUEiLz48c3RvcCBvZmZzZXQ9IjEiIHN0b3AtY29sb3I9IiNBMzgzNjMiLz48L2xpbmVhckdyYWRpZW50Pjxs ...(+4756 chars)\",\"srcOrientation\":\"Right\"},\"position\":[0,0,1,1],\"value\":\"31\"},{\"image\":{\"size\":[0,0],\"src\":\"data:image\\/svg+xml;base64,PHN2ZyB4bWxucz0iaHR0cDovL3d3dy53My5vcmcvMjAwMC9zdmciIHdpZHRoPSIyMjAiIGhlaWdodD0iMjg0IiB2aWV3Qm94PSIwIDAgMjIwIDI4NCIgcm9sZT0iaW1nIiA+Cjx0aXRsZT5IRVhBTE9DSyBtb2R1bGFyIGludGVyZmFjZSBhc3NldDwvdGl0bGU+CjxkZWZzPjxsaW5lYXJHcmFkaWVudCBpZD0ia3JhZnRGcm9udCIgeDE9IjAiIHkxPSIwIiB4Mj0iMSIgeTI9IjEiPjxzdG9wIHN0b3AtY29sb3I9IiNEM0I5OUEiLz48c3RvcCBvZmZzZXQ9IjEiIHN0b3AtY29sb3I9IiNBMzgzNjMiLz48L2xpbmVhckdyYWRpZW50Pjxs ...(+4752 chars)\",\"srcOrientation\":\"Right\"},\"position\":[0,0,1,1],\"value\":\"32\"},{\"image\":{\"size\":[0,0],\"src\":\"data:image\\/svg+xml;base64,PHN2ZyB4bWxucz0iaHR0cDovL3d3dy53My5vcmcvMjAwMC9zdmciIHdpZHRoPSIyMjAiIGhlaWdodD0iMjg0IiB2aWV3Qm94PSIwIDAgMjIwIDI4NCIgcm9sZT0iaW1nIiA+Cjx0aXRsZT5IRVhBTE9DSyBtb2R1bGFyIGludGVyZmFjZSBhc3NldDwvdGl0bGU+CjxkZWZzPjxsaW5lYXJHcmFkaWVudCBpZD0ia3JhZnRGcm9udCIgeDE9IjAiIHkxPSIwIiB4Mj0iMSIgeTI9IjEiPjxzdG9wIHN0b3AtY29sb3I9IiNEM0I5OUEiLz48c3RvcCBvZmZzZXQ9IjEiIHN0b3AtY29sb3I9IiNBMzgzNjMiLz48L2xpbmVhckdyYWRpZW50Pjxs ...(+6860 chars)\",\"srcOrientation\":\"Right\"},\"position\":[0,0,1,1],\"value\":\"33\"},{\"image\":{\"size\":[0,0],\"src\":\"data:image\\/svg+xml;base64,PHN2ZyB4bWxucz0iaHR0cDovL3d3dy53My5vcmcvMjAwMC9zdmciIHdpZHRoPSIyMjAiIGhlaWdodD0iMjg0IiB2aWV3Qm94PSIwIDAgMjIwIDI4NCIgcm9sZT0iaW1nIiA+Cjx0aXRsZT5IRVhBTE9DSyBtb2R1bGFyIGludGVyZmFjZSBhc3NldDwvdGl0bGU+CjxkZWZzPjxsaW5lYXJHcmFkaWVudCBpZD0ia3JhZnRGcm9udCIgeDE9IjAiIHkxPSIwIiB4Mj0iMSIgeTI9IjEiPjxzdG9wIHN0b3AtY29sb3I9IiNEM0I5OUEiLz48c3RvcCBvZmZzZXQ9IjEiIHN0b3AtY29sb3I9IiNBMzgzNjMiLz48L2xpbmVhckdyYWRpZW50Pjxs ...(+6860 chars)\",\"srcOrientation\":\"Right\"},\"position\":[0,0,1,1],\"value\":\"34\"},{\"image\":{\"size\":[0,0],\"src\":\"data:image\\/svg+xml;base64,PHN2ZyB4bWxucz0iaHR0cDovL3d3dy53My5vcmcvMjAwMC9zdmciIHdpZHRoPSIyMjAiIGhlaWdodD0iMjg0IiB2aWV3Qm94PSIwIDAgMjIwIDI4NCIgcm9sZT0iaW1nIiA+Cjx0aXRsZT5IRVhBTE9DSyBtb2R1bGFyIGludGVyZmFjZSBhc3NldDwvdGl0bGU+CjxkZWZzPjxsaW5lYXJHcmFkaWVudCBpZD0ia3JhZnRGcm9udCIgeDE9IjAiIHkxPSIwIiB4Mj0iMSIgeTI9IjEiPjxzdG9wIHN0b3AtY29sb3I9IiNEM0I5OUEiLz48c3RvcCBvZmZzZXQ9IjEiIHN0b3AtY29sb3I9IiNBMzgzNjMiLz48L2xpbmVhckdyYWRpZW50Pjxs ...(+6860 chars)\",\"srcOrientation\":\"Right\"},\"position\":[0,0,1,1],\"value\":\"35\"},{\"image\":{\"size\":[0,0],\"src\":\"data:image\\/svg+xml;base64,PHN2ZyB4bWxucz0iaHR0cDovL3d3dy53My5vcmcvMjAwMC9zdmciIHdpZHRoPSIyMjAiIGhlaWdodD0iMjg0IiB2aWV3Qm94PSIwIDAgMjIwIDI4NCIgcm9sZT0iaW1nIiA+DQo8dGl0bGU+SEVYQUxPQ0sgbW9kdWxhciBpbnRlcmZhY2UgYXNzZXQ8L3RpdGxlPg0KPGRlZnM+PGxpbmVhckdyYWRpZW50IGlkPSJrcmFmdEZyb250IiB4MT0iMCIgeTE9IjAiIHgyPSIxIiB5Mj0iMSI+PHN0b3Agc3RvcC1jb2xvcj0iI0QzQjk5QSIvPjxzdG9wIG9mZnNldD0iMSIgc3RvcC1jb2xvcj0iI0EzODM2MyIvPjwvbGluZWFyR3JhZGllbnQ+ ...(+6912 chars)\",\"srcOrientation\":\"Right\"},\"position\":[0,0,1,1],\"value\":\"36\"},{\"image\":{\"size\":[0,0],\"src\":\"data:image\\/svg+xml;base64,PHN2ZyB4bWxucz0iaHR0cDovL3d3dy53My5vcmcvMjAwMC9zdmciIHdpZHRoPSIyMjAiIGhlaWdodD0iMjg0IiB2aWV3Qm94PSIwIDAgMjIwIDI4NCIgcm9sZT0iaW1nIiA+DQo8dGl0bGU+SEVYQUxPQ0sgbW9kdWxhciBpbnRlcmZhY2UgYXNzZXQ8L3RpdGxlPg0KPGRlZnM+PGxpbmVhckdyYWRpZW50IGlkPSJrcmFmdEZyb250IiB4MT0iMCIgeTE9IjAiIHgyPSIxIiB5Mj0iMSI+PHN0b3Agc3RvcC1jb2xvcj0iI0QzQjk5QSIvPjxzdG9wIG9mZnNldD0iMSIgc3RvcC1jb2xvcj0iI0EzODM2MyIvPjwvbGluZWFyR3JhZGllbnQ+ ...(+6912 chars)\",\"srcOrientation\":\"Right\"},\"position\":[0,0,1,1],\"value\":\"37\"},{\"image\":{\"size\":[0,0],\"src\":\"data:image\\/svg+xml;base64,PHN2ZyB4bWxucz0iaHR0cDovL3d3dy53My5vcmcvMjAwMC9zdmciIHdpZHRoPSIyMjAiIGhlaWdodD0iMjg0IiB2aWV3Qm94PSIwIDAgMjIwIDI4NCIgcm9sZT0iaW1nIiA+DQo8dGl0bGU+SEVYQUxPQ0sgbW9kdWxhciBpbnRlcmZhY2UgYXNzZXQ8L3RpdGxlPg0KPGRlZnM+PGxpbmVhckdyYWRpZW50IGlkPSJrcmFmdEZyb250IiB4MT0iMCIgeTE9IjAiIHgyPSIxIiB5Mj0iMSI+PHN0b3Agc3RvcC1jb2xvcj0iI0QzQjk5QSIvPjxzdG9wIG9mZnNldD0iMSIgc3RvcC1jb2xvcj0iI0EzODM2MyIvPjwvbGluZWFyR3JhZGllbnQ+ ...(+6912 chars)\",\"srcOrientation\":\"Right\"},\"position\":[0,0,1,1],\"value\":\"38\"}],\"valueType\":\"discrete\"}},{\"name\":\"ForegroundImageComponent\",\"settings\":{\"image\":{\"size\":[0,0],\"src\":\"default\",\"srcOrientation\":\"Right\"},\"isForeground\":1,\"position\":[0,0,1,1],\"scaleMode\":\"0\"}}],\"derived\":{\"blockParameters\":{\"DefaultImage\":\"data:image\\/svg+xml;base64,PHN2ZyB4bWxucz0iaHR0cDovL3d3dy53My5vcmcvMjAwMC9zdmciIHdpZHRoPSIyMjAiIGhlaWdodD0iMjg0IiB2aWV3Qm94PSIwIDAgMjIwIDI4NCIgcm9sZT0iaW1nIiA+Cjx0aXRsZT5IRVhBTE9DSyBtb2R1bGFyIGludGVyZmFjZSBhc3NldDwvdGl0bGU+CjxkZWZzPjwvZGVmcz4KICAgICAgPHJlY3QgeD0iOCIgeT0iOCIgd2lkdGg9IjIwNCIgaGVpZ2h0PSIyNjgiIHJ4PSIxNCIgZmlsbD0iIzExMUMyMiIgc3Ryb2tlPSIjNTM2NjZFIiBzdHJva2Utd2lkdGg9IjIiLz4KICAgICAgPHJlY3QgeD0iMTIiIHk9IjEyIiB3aWR0 ...(+3224 chars)\",\"StateValueType\":\"discrete\",\"States\":[{\"image\":\"data:image\\/svg+xml;base64,PHN2ZyB4bWxucz0iaHR0cDovL3d3dy53My5vcmcvMjAwMC9zdmciIHdpZHRoPSIyMjAiIGhlaWdodD0iMjg0IiB2aWV3Qm94PSIwIDAgMjIwIDI4NCIgcm9sZT0iaW1nIiA+Cjx0aXRsZT5IRVhBTE9DSyBtb2R1bGFyIGludGVyZmFjZSBhc3NldDwvdGl0bGU+CjxkZWZzPjwvZGVmcz4KICAgICAgPHJlY3QgeD0iOCIgeT0iOCIgd2lkdGg9IjIwNCIgaGVpZ2h0PSIyNjgiIHJ4PSIxNCIgZmlsbD0iIzExMUMyMiIgc3Ryb2tlPSIjNTM2NjZFIiBzdHJva2Utd2lkdGg9IjIiLz4KICAgICAgPHJlY3QgeD0iMTIiIHk9IjEyIiB3aWR0 ...(+3224 chars)\",\"value\":\"0\"},{\"image\":\"data:image\\/svg+xml;base64,PHN2ZyB4bWxucz0iaHR0cDovL3d3dy53My5vcmcvMjAwMC9zdmciIHdpZHRoPSIyMjAiIGhlaWdodD0iMjg0IiB2aWV3Qm94PSIwIDAgMjIwIDI4NCIgcm9sZT0iaW1nIiA+Cjx0aXRsZT5IRVhBTE9DSyBtb2R1bGFyIGludGVyZmFjZSBhc3NldDwvdGl0bGU+CjxkZWZzPjwvZGVmcz4KICAgICAgPHJlY3QgeD0iOCIgeT0iOCIgd2lkdGg9IjIwNCIgaGVpZ2h0PSIyNjgiIHJ4PSIxNCIgZmlsbD0iIzExMUMyMiIgc3Ryb2tlPSIjNTM2NjZFIiBzdHJva2Utd2lkdGg9IjIiLz4KICAgICAgPHJlY3QgeD0iMTIiIHk9IjEyIiB3aWR0 ...(+3220 chars)\",\"value\":\"1\"},{\"image\":\"data:image\\/svg+xml;base64,PHN2ZyB4bWxucz0iaHR0cDovL3d3dy53My5vcmcvMjAwMC9zdmciIHdpZHRoPSIyMjAiIGhlaWdodD0iMjg0IiB2aWV3Qm94PSIwIDAgMjIwIDI4NCIgcm9sZT0iaW1nIiA+Cjx0aXRsZT5IRVhBTE9DSyBtb2R1bGFyIGludGVyZmFjZSBhc3NldDwvdGl0bGU+CjxkZWZzPjwvZGVmcz4KICAgICAgPHJlY3QgeD0iOCIgeT0iOCIgd2lkdGg9IjIwNCIgaGVpZ2h0PSIyNjgiIHJ4PSIxNCIgZmlsbD0iIzExMUMyMiIgc3Ryb2tlPSIjQjk4NTZFIiBzdHJva2Utd2lkdGg9IjIuNiIvPgogICAgICA8cmVjdCB4PSIxMiIgeT0iMTIiIHdp ...(+3488 chars)\",\"value\":\"2\"},{\"image\":\"data:image\\/svg+xml;base64,PHN2ZyB4bWxucz0iaHR0cDovL3d3dy53My5vcmcvMjAwMC9zdmciIHdpZHRoPSIyMjAiIGhlaWdodD0iMjg0IiB2aWV3Qm94PSIwIDAgMjIwIDI4NCIgcm9sZT0iaW1nIiA+Cjx0aXRsZT5IRVhBTE9DSyBtb2R1bGFyIGludGVyZmFjZSBhc3NldDwvdGl0bGU+CjxkZWZzPjwvZGVmcz4KICAgICAgPHJlY3QgeD0iOCIgeT0iOCIgd2lkdGg9IjIwNCIgaGVpZ2h0PSIyNjgiIHJ4PSIxNCIgZmlsbD0iIzExMUMyMiIgc3Ryb2tlPSIjQjk4NTZFIiBzdHJva2Utd2lkdGg9IjIuNiIvPgogICAgICA8cmVjdCB4PSIxMiIgeT0iMTIiIHdp ...(+3484 chars)\",\"value\":\"3\"},{\"image\":\"data:image\\/svg+xml;base64,PHN2ZyB4bWxucz0iaHR0cDovL3d3dy53My5vcmcvMjAwMC9zdmciIHdpZHRoPSIyMjAiIGhlaWdodD0iMjg0IiB2aWV3Qm94PSIwIDAgMjIwIDI4NCIgcm9sZT0iaW1nIiA+Cjx0aXRsZT5IRVhBTE9DSyBtb2R1bGFyIGludGVyZmFjZSBhc3NldDwvdGl0bGU+CjxkZWZzPjwvZGVmcz4KICAgICAgPHJlY3QgeD0iOCIgeT0iOCIgd2lkdGg9IjIwNCIgaGVpZ2h0PSIyNjgiIHJ4PSIxNCIgZmlsbD0iIzExMUMyMiIgc3Ryb2tlPSIjQjk4NTZFIiBzdHJva2Utd2lkdGg9IjIuNiIvPgogICAgICA8cmVjdCB4PSIxMiIgeT0iMTIiIHdp ...(+3532 chars)\",\"value\":\"4\"},{\"image\":\"data:image\\/svg+xml;base64,PHN2ZyB4bWxucz0iaHR0cDovL3d3dy53My5vcmcvMjAwMC9zdmciIHdpZHRoPSIyMjAiIGhlaWdodD0iMjg0IiB2aWV3Qm94PSIwIDAgMjIwIDI4NCIgcm9sZT0iaW1nIiA+Cjx0aXRsZT5IRVhBTE9DSyBtb2R1bGFyIGludGVyZmFjZSBhc3NldDwvdGl0bGU+CjxkZWZzPjwvZGVmcz4KICAgICAgPHJlY3QgeD0iOCIgeT0iOCIgd2lkdGg9IjIwNCIgaGVpZ2h0PSIyNjgiIHJ4PSIxNCIgZmlsbD0iIzExMUMyMiIgc3Ryb2tlPSIjQjk4NTZFIiBzdHJva2Utd2lkdGg9IjIuNiIvPgogICAgICA8cmVjdCB4PSIxMiIgeT0iMTIiIHdp ...(+3532 chars)\",\"value\":\"5\"},{\"image\":\"data:image\\/svg+xml;base64,PHN2ZyB4bWxucz0iaHR0cDovL3d3dy53My5vcmcvMjAwMC9zdmciIHdpZHRoPSIyMjAiIGhlaWdodD0iMjg0IiB2aWV3Qm94PSIwIDAgMjIwIDI4NCIgcm9sZT0iaW1nIiA+Cjx0aXRsZT5IRVhBTE9DSyBtb2R1bGFyIGludGVyZmFjZSBhc3NldDwvdGl0bGU+CjxkZWZzPjwvZGVmcz4KICAgICAgPHJlY3QgeD0iOCIgeT0iOCIgd2lkdGg9IjIwNCIgaGVpZ2h0PSIyNjgiIHJ4PSIxNCIgZmlsbD0iIzExMUMyMiIgc3Ryb2tlPSIjQjk4NTZFIiBzdHJva2Utd2lkdGg9IjIuNiIvPgogICAgICA8cmVjdCB4PSIxMiIgeT0iMTIiIHdp ...(+3532 chars)\",\"value\":\"6\"},{\"image\":\"data:image\\/svg+xml;base64,PHN2ZyB4bWxucz0iaHR0cDovL3d3dy53My5vcmcvMjAwMC9zdmciIHdpZHRoPSIyMjAiIGhlaWdodD0iMjg0IiB2aWV3Qm94PSIwIDAgMjIwIDI4NCIgcm9sZT0iaW1nIiA+Cjx0aXRsZT5IRVhBTE9DSyBtb2R1bGFyIGludGVyZmFjZSBhc3NldDwvdGl0bGU+CjxkZWZzPjwvZGVmcz4KICAgICAgPHJlY3QgeD0iOCIgeT0iOCIgd2lkdGg9IjIwNCIgaGVpZ2h0PSIyNjgiIHJ4PSIxNCIgZmlsbD0iIzExMUMyMiIgc3Ryb2tlPSIjQjk4NTZFIiBzdHJva2Utd2lkdGg9IjIuNiIvPgogICAgICA8cmVjdCB4PSIxMiIgeT0iMTIiIHdp ...(+3524 chars)\",\"value\":\"7\"},{\"image\":\"data:image\\/svg+xml;base64,PHN2ZyB4bWxucz0iaHR0cDovL3d3dy53My5vcmcvMjAwMC9zdmciIHdpZHRoPSIyMjAiIGhlaWdodD0iMjg0IiB2aWV3Qm94PSIwIDAgMjIwIDI4NCIgcm9sZT0iaW1nIiA+Cjx0aXRsZT5IRVhBTE9DSyBtb2R1bGFyIGludGVyZmFjZSBhc3NldDwvdGl0bGU+CjxkZWZzPjwvZGVmcz4KICAgICAgPHJlY3QgeD0iOCIgeT0iOCIgd2lkdGg9IjIwNCIgaGVpZ2h0PSIyNjgiIHJ4PSIxNCIgZmlsbD0iIzExMUMyMiIgc3Ryb2tlPSIjQjk4NTZFIiBzdHJva2Utd2lkdGg9IjIuNiIvPgogICAgICA8cmVjdCB4PSIxMiIgeT0iMTIiIHdp ...(+3532 chars)\",\"value\":\"8\"},{\"image\":\"data:image\\/svg+xml;base64,PHN2ZyB4bWxucz0iaHR0cDovL3d3dy53My5vcmcvMjAwMC9zdmciIHdpZHRoPSIyMjAiIGhlaWdodD0iMjg0IiB2aWV3Qm94PSIwIDAgMjIwIDI4NCIgcm9sZT0iaW1nIiA+Cjx0aXRsZT5IRVhBTE9DSyBtb2R1bGFyIGludGVyZmFjZSBhc3NldDwvdGl0bGU+CjxkZWZzPjwvZGVmcz4KICAgICAgPHJlY3QgeD0iOCIgeT0iOCIgd2lkdGg9IjIwNCIgaGVpZ2h0PSIyNjgiIHJ4PSIxNCIgZmlsbD0iIzExMUMyMiIgc3Ryb2tlPSIjQjk4NTZFIiBzdHJva2Utd2lkdGg9IjIuNiIvPgogICAgICA8cmVjdCB4PSIxMiIgeT0iMTIiIHdp ...(+3532 chars)\",\"value\":\"9\"},{\"image\":\"data:image\\/svg+xml;base64,PHN2ZyB4bWxucz0iaHR0cDovL3d3dy53My5vcmcvMjAwMC9zdmciIHdpZHRoPSIyMjAiIGhlaWdodD0iMjg0IiB2aWV3Qm94PSIwIDAgMjIwIDI4NCIgcm9sZT0iaW1nIiA+Cjx0aXRsZT5IRVhBTE9DSyBtb2R1bGFyIGludGVyZmFjZSBhc3NldDwvdGl0bGU+CjxkZWZzPjwvZGVmcz4KICAgICAgPHJlY3QgeD0iOCIgeT0iOCIgd2lkdGg9IjIwNCIgaGVpZ2h0PSIyNjgiIHJ4PSIxNCIgZmlsbD0iIzExMUMyMiIgc3Ryb2tlPSIjQjk4NTZFIiBzdHJva2Utd2lkdGg9IjIuNiIvPgogICAgICA8cmVjdCB4PSIxMiIgeT0iMTIiIHdp ...(+3532 chars)\",\"value\":\"10\"},{\"image\":\"data:image\\/svg+xml;base64,PHN2ZyB4bWxucz0iaHR0cDovL3d3dy53My5vcmcvMjAwMC9zdmciIHdpZHRoPSIyMjAiIGhlaWdodD0iMjg0IiB2aWV3Qm94PSIwIDAgMjIwIDI4NCIgcm9sZT0iaW1nIiA+Cjx0aXRsZT5IRVhBTE9DSyBtb2R1bGFyIGludGVyZmFjZSBhc3NldDwvdGl0bGU+CjxkZWZzPjwvZGVmcz4KICAgICAgPHJlY3QgeD0iOCIgeT0iOCIgd2lkdGg9IjIwNCIgaGVpZ2h0PSIyNjgiIHJ4PSIxNCIgZmlsbD0iIzExMUMyMiIgc3Ryb2tlPSIjNTM2NjZFIiBzdHJva2Utd2lkdGg9IjIiLz4KICAgICAgPHJlY3QgeD0iMTIiIHk9IjEyIiB3aWR0 ...(+3220 chars)\",\"value\":\"11\"},{\"image\":\"data:image\\/svg+xml;base64,PHN2ZyB4bWxucz0iaHR0cDovL3d3dy53My5vcmcvMjAwMC9zdmciIHdpZHRoPSIyMjAiIGhlaWdodD0iMjg0IiB2aWV3Qm94PSIwIDAgMjIwIDI4NCIgcm9sZT0iaW1nIiA+Cjx0aXRsZT5IRVhBTE9DSyBtb2R1bGFyIGludGVyZmFjZSBhc3NldDwvdGl0bGU+CjxkZWZzPjxsaW5lYXJHcmFkaWVudCBpZD0ia3JhZnRGcm9udCIgeDE9IjAiIHkxPSIwIiB4Mj0iMSIgeTI9IjEiPjxzdG9wIHN0b3AtY29sb3I9IiNEM0I5OUEiLz48c3RvcCBvZmZzZXQ9IjEiIHN0b3AtY29sb3I9IiNBMzgzNjMiLz48L2xpbmVhckdyYWRpZW50Pjxs ...(+4752 chars)\",\"value\":\"20\"},{\"image\":\"data:image\\/svg+xml;base64,PHN2ZyB4bWxucz0iaHR0cDovL3d3dy53My5vcmcvMjAwMC9zdmciIHdpZHRoPSIyMjAiIGhlaWdodD0iMjg0IiB2aWV3Qm94PSIwIDAgMjIwIDI4NCIgcm9sZT0iaW1nIiA+Cjx0aXRsZT5IRVhBTE9DSyBtb2R1bGFyIGludGVyZmFjZSBhc3NldDwvdGl0bGU+CjxkZWZzPjxsaW5lYXJHcmFkaWVudCBpZD0ia3JhZnRGcm9udCIgeDE9IjAiIHkxPSIwIiB4Mj0iMSIgeTI9IjEiPjxzdG9wIHN0b3AtY29sb3I9IiNEM0I5OUEiLz48c3RvcCBvZmZzZXQ9IjEiIHN0b3AtY29sb3I9IiNBMzgzNjMiLz48L2xpbmVhckdyYWRpZW50Pjxs ...(+7264 chars)\",\"value\":\"21\"},{\"image\":\"data:image\\/svg+xml;base64,PHN2ZyB4bWxucz0iaHR0cDovL3d3dy53My5vcmcvMjAwMC9zdmciIHdpZHRoPSIyMjAiIGhlaWdodD0iMjg0IiB2aWV3Qm94PSIwIDAgMjIwIDI4NCIgcm9sZT0iaW1nIiA+Cjx0aXRsZT5IRVhBTE9DSyBtb2R1bGFyIGludGVyZmFjZSBhc3NldDwvdGl0bGU+CjxkZWZzPjxsaW5lYXJHcmFkaWVudCBpZD0ia3JhZnRGcm9udCIgeDE9IjAiIHkxPSIwIiB4Mj0iMSIgeTI9IjEiPjxzdG9wIHN0b3AtY29sb3I9IiNEM0I5OUEiLz48c3RvcCBvZmZzZXQ9IjEiIHN0b3AtY29sb3I9IiNBMzgzNjMiLz48L2xpbmVhckdyYWRpZW50Pjxs ...(+7264 chars)\",\"value\":\"22\"},{\"image\":\"data:image\\/svg+xml;base64,PHN2ZyB4bWxucz0iaHR0cDovL3d3dy53My5vcmcvMjAwMC9zdmciIHdpZHRoPSIyMjAiIGhlaWdodD0iMjg0IiB2aWV3Qm94PSIwIDAgMjIwIDI4NCIgcm9sZT0iaW1nIiA+Cjx0aXRsZT5IRVhBTE9DSyBtb2R1bGFyIGludGVyZmFjZSBhc3NldDwvdGl0bGU+CjxkZWZzPjxsaW5lYXJHcmFkaWVudCBpZD0ia3JhZnRGcm9udCIgeDE9IjAiIHkxPSIwIiB4Mj0iMSIgeTI9IjEiPjxzdG9wIHN0b3AtY29sb3I9IiNEM0I5OUEiLz48c3RvcCBvZmZzZXQ9IjEiIHN0b3AtY29sb3I9IiNBMzgzNjMiLz48L2xpbmVhckdyYWRpZW50Pjxs ...(+7264 chars)\",\"value\":\"23\"},{\"image\":\"data:image\\/svg+xml;base64,PHN2ZyB4bWxucz0iaHR0cDovL3d3dy53My5vcmcvMjAwMC9zdmciIHdpZHRoPSIyMjAiIGhlaWdodD0iMjg0IiB2aWV3Qm94PSIwIDAgMjIwIDI4NCIgcm9sZT0iaW1nIiA+Cjx0aXRsZT5IRVhBTE9DSyBtb2R1bGFyIGludGVyZmFjZSBhc3NldDwvdGl0bGU+CjxkZWZzPjxsaW5lYXJHcmFkaWVudCBpZD0ia3JhZnRGcm9udCIgeDE9IjAiIHkxPSIwIiB4Mj0iMSIgeTI9IjEiPjxzdG9wIHN0b3AtY29sb3I9IiNEM0I5OUEiLz48c3RvcCBvZmZzZXQ9IjEiIHN0b3AtY29sb3I9IiNBMzgzNjMiLz48L2xpbmVhckdyYWRpZW50Pjxs ...(+7260 chars)\",\"value\":\"24\"},{\"image\":\"data:image\\/svg+xml;base64,PHN2ZyB4bWxucz0iaHR0cDovL3d3dy53My5vcmcvMjAwMC9zdmciIHdpZHRoPSIyMjAiIGhlaWdodD0iMjg0IiB2aWV3Qm94PSIwIDAgMjIwIDI4NCIgcm9sZT0iaW1nIiA+Cjx0aXRsZT5IRVhBTE9DSyBtb2R1bGFyIGludGVyZmFjZSBhc3NldDwvdGl0bGU+CjxkZWZzPjxsaW5lYXJHcmFkaWVudCBpZD0ia3JhZnRGcm9udCIgeDE9IjAiIHkxPSIwIiB4Mj0iMSIgeTI9IjEiPjxzdG9wIHN0b3AtY29sb3I9IiNEM0I5OUEiLz48c3RvcCBvZmZzZXQ9IjEiIHN0b3AtY29sb3I9IiNBMzgzNjMiLz48L2xpbmVhckdyYWRpZW50Pjxs ...(+7264 chars)\",\"value\":\"25\"},{\"image\":\"data:image\\/svg+xml;base64,PHN2ZyB4bWxucz0iaHR0cDovL3d3dy53My5vcmcvMjAwMC9zdmciIHdpZHRoPSIyMjAiIGhlaWdodD0iMjg0IiB2aWV3Qm94PSIwIDAgMjIwIDI4NCIgcm9sZT0iaW1nIiA+Cjx0aXRsZT5IRVhBTE9DSyBtb2R1bGFyIGludGVyZmFjZSBhc3NldDwvdGl0bGU+CjxkZWZzPjxsaW5lYXJHcmFkaWVudCBpZD0ia3JhZnRGcm9udCIgeDE9IjAiIHkxPSIwIiB4Mj0iMSIgeTI9IjEiPjxzdG9wIHN0b3AtY29sb3I9IiNEM0I5OUEiLz48c3RvcCBvZmZzZXQ9IjEiIHN0b3AtY29sb3I9IiNBMzgzNjMiLz48L2xpbmVhckdyYWRpZW50Pjxs ...(+7272 chars)\",\"value\":\"26\"},{\"image\":\"data:image\\/svg+xml;base64,PHN2ZyB4bWxucz0iaHR0cDovL3d3dy53My5vcmcvMjAwMC9zdmciIHdpZHRoPSIyMjAiIGhlaWdodD0iMjg0IiB2aWV3Qm94PSIwIDAgMjIwIDI4NCIgcm9sZT0iaW1nIiA+Cjx0aXRsZT5IRVhBTE9DSyBtb2R1bGFyIGludGVyZmFjZSBhc3NldDwvdGl0bGU+CjxkZWZzPjxsaW5lYXJHcmFkaWVudCBpZD0ia3JhZnRGcm9udCIgeDE9IjAiIHkxPSIwIiB4Mj0iMSIgeTI9IjEiPjxzdG9wIHN0b3AtY29sb3I9IiNEM0I5OUEiLz48c3RvcCBvZmZzZXQ9IjEiIHN0b3AtY29sb3I9IiNBMzgzNjMiLz48L2xpbmVhckdyYWRpZW50Pjxs ...(+7264 chars)\",\"value\":\"27\"},{\"image\":\"data:image\\/svg+xml;base64,PHN2ZyB4bWxucz0iaHR0cDovL3d3dy53My5vcmcvMjAwMC9zdmciIHdpZHRoPSIyMjAiIGhlaWdodD0iMjg0IiB2aWV3Qm94PSIwIDAgMjIwIDI4NCIgcm9sZT0iaW1nIiA+Cjx0aXRsZT5IRVhBTE9DSyBtb2R1bGFyIGludGVyZmFjZSBhc3NldDwvdGl0bGU+CjxkZWZzPjxsaW5lYXJHcmFkaWVudCBpZD0ia3JhZnRGcm9udCIgeDE9IjAiIHkxPSIwIiB4Mj0iMSIgeTI9IjEiPjxzdG9wIHN0b3AtY29sb3I9IiNEM0I5OUEiLz48c3RvcCBvZmZzZXQ9IjEiIHN0b3AtY29sb3I9IiNBMzgzNjMiLz48L2xpbmVhckdyYWRpZW50Pjxs ...(+7268 chars)\",\"value\":\"28\"},{\"image\":\"data:image\\/svg+xml;base64,PHN2ZyB4bWxucz0iaHR0cDovL3d3dy53My5vcmcvMjAwMC9zdmciIHdpZHRoPSIyMjAiIGhlaWdodD0iMjg0IiB2aWV3Qm94PSIwIDAgMjIwIDI4NCIgcm9sZT0iaW1nIiA+Cjx0aXRsZT5IRVhBTE9DSyBtb2R1bGFyIGludGVyZmFjZSBhc3NldDwvdGl0bGU+CjxkZWZzPjxsaW5lYXJHcmFkaWVudCBpZD0ia3JhZnRGcm9udCIgeDE9IjAiIHkxPSIwIiB4Mj0iMSIgeTI9IjEiPjxzdG9wIHN0b3AtY29sb3I9IiNEM0I5OUEiLz48c3RvcCBvZmZzZXQ9IjEiIHN0b3AtY29sb3I9IiNBMzgzNjMiLz48L2xpbmVhckdyYWRpZW50Pjxs ...(+7268 chars)\",\"value\":\"29\"},{\"image\":\"data:image\\/svg+xml;base64,PHN2ZyB4bWxucz0iaHR0cDovL3d3dy53My5vcmcvMjAwMC9zdmciIHdpZHRoPSIyMjAiIGhlaWdodD0iMjg0IiB2aWV3Qm94PSIwIDAgMjIwIDI4NCIgcm9sZT0iaW1nIiA+Cjx0aXRsZT5IRVhBTE9DSyBtb2R1bGFyIGludGVyZmFjZSBhc3NldDwvdGl0bGU+CjxkZWZzPjxsaW5lYXJHcmFkaWVudCBpZD0ia3JhZnRGcm9udCIgeDE9IjAiIHkxPSIwIiB4Mj0iMSIgeTI9IjEiPjxzdG9wIHN0b3AtY29sb3I9IiNEM0I5OUEiLz48c3RvcCBvZmZzZXQ9IjEiIHN0b3AtY29sb3I9IiNBMzgzNjMiLz48L2xpbmVhckdyYWRpZW50Pjxs ...(+7268 chars)\",\"value\":\"30\"},{\"image\":\"data:image\\/svg+xml;base64,PHN2ZyB4bWxucz0iaHR0cDovL3d3dy53My5vcmcvMjAwMC9zdmciIHdpZHRoPSIyMjAiIGhlaWdodD0iMjg0IiB2aWV3Qm94PSIwIDAgMjIwIDI4NCIgcm9sZT0iaW1nIiA+Cjx0aXRsZT5IRVhBTE9DSyBtb2R1bGFyIGludGVyZmFjZSBhc3NldDwvdGl0bGU+CjxkZWZzPjxsaW5lYXJHcmFkaWVudCBpZD0ia3JhZnRGcm9udCIgeDE9IjAiIHkxPSIwIiB4Mj0iMSIgeTI9IjEiPjxzdG9wIHN0b3AtY29sb3I9IiNEM0I5OUEiLz48c3RvcCBvZmZzZXQ9IjEiIHN0b3AtY29sb3I9IiNBMzgzNjMiLz48L2xpbmVhckdyYWRpZW50Pjxs ...(+4756 chars)\",\"value\":\"31\"},{\"image\":\"data:image\\/svg+xml;base64,PHN2ZyB4bWxucz0iaHR0cDovL3d3dy53My5vcmcvMjAwMC9zdmciIHdpZHRoPSIyMjAiIGhlaWdodD0iMjg0IiB2aWV3Qm94PSIwIDAgMjIwIDI4NCIgcm9sZT0iaW1nIiA+Cjx0aXRsZT5IRVhBTE9DSyBtb2R1bGFyIGludGVyZmFjZSBhc3NldDwvdGl0bGU+CjxkZWZzPjxsaW5lYXJHcmFkaWVudCBpZD0ia3JhZnRGcm9udCIgeDE9IjAiIHkxPSIwIiB4Mj0iMSIgeTI9IjEiPjxzdG9wIHN0b3AtY29sb3I9IiNEM0I5OUEiLz48c3RvcCBvZmZzZXQ9IjEiIHN0b3AtY29sb3I9IiNBMzgzNjMiLz48L2xpbmVhckdyYWRpZW50Pjxs ...(+4752 chars)\",\"value\":\"32\"},{\"image\":\"data:image\\/svg+xml;base64,PHN2ZyB4bWxucz0iaHR0cDovL3d3dy53My5vcmcvMjAwMC9zdmciIHdpZHRoPSIyMjAiIGhlaWdodD0iMjg0IiB2aWV3Qm94PSIwIDAgMjIwIDI4NCIgcm9sZT0iaW1nIiA+Cjx0aXRsZT5IRVhBTE9DSyBtb2R1bGFyIGludGVyZmFjZSBhc3NldDwvdGl0bGU+CjxkZWZzPjxsaW5lYXJHcmFkaWVudCBpZD0ia3JhZnRGcm9udCIgeDE9IjAiIHkxPSIwIiB4Mj0iMSIgeTI9IjEiPjxzdG9wIHN0b3AtY29sb3I9IiNEM0I5OUEiLz48c3RvcCBvZmZzZXQ9IjEiIHN0b3AtY29sb3I9IiNBMzgzNjMiLz48L2xpbmVhckdyYWRpZW50Pjxs ...(+6860 chars)\",\"value\":\"33\"},{\"image\":\"data:image\\/svg+xml;base64,PHN2ZyB4bWxucz0iaHR0cDovL3d3dy53My5vcmcvMjAwMC9zdmciIHdpZHRoPSIyMjAiIGhlaWdodD0iMjg0IiB2aWV3Qm94PSIwIDAgMjIwIDI4NCIgcm9sZT0iaW1nIiA+Cjx0aXRsZT5IRVhBTE9DSyBtb2R1bGFyIGludGVyZmFjZSBhc3NldDwvdGl0bGU+CjxkZWZzPjxsaW5lYXJHcmFkaWVudCBpZD0ia3JhZnRGcm9udCIgeDE9IjAiIHkxPSIwIiB4Mj0iMSIgeTI9IjEiPjxzdG9wIHN0b3AtY29sb3I9IiNEM0I5OUEiLz48c3RvcCBvZmZzZXQ9IjEiIHN0b3AtY29sb3I9IiNBMzgzNjMiLz48L2xpbmVhckdyYWRpZW50Pjxs ...(+6860 chars)\",\"value\":\"34\"},{\"image\":\"data:image\\/svg+xml;base64,PHN2ZyB4bWxucz0iaHR0cDovL3d3dy53My5vcmcvMjAwMC9zdmciIHdpZHRoPSIyMjAiIGhlaWdodD0iMjg0IiB2aWV3Qm94PSIwIDAgMjIwIDI4NCIgcm9sZT0iaW1nIiA+Cjx0aXRsZT5IRVhBTE9DSyBtb2R1bGFyIGludGVyZmFjZSBhc3NldDwvdGl0bGU+CjxkZWZzPjxsaW5lYXJHcmFkaWVudCBpZD0ia3JhZnRGcm9udCIgeDE9IjAiIHkxPSIwIiB4Mj0iMSIgeTI9IjEiPjxzdG9wIHN0b3AtY29sb3I9IiNEM0I5OUEiLz48c3RvcCBvZmZzZXQ9IjEiIHN0b3AtY29sb3I9IiNBMzgzNjMiLz48L2xpbmVhckdyYWRpZW50Pjxs ...(+6860 chars)\",\"value\":\"35\"},{\"image\":\"data:image\\/svg+xml;base64,PHN2ZyB4bWxucz0iaHR0cDovL3d3dy53My5vcmcvMjAwMC9zdmciIHdpZHRoPSIyMjAiIGhlaWdodD0iMjg0IiB2aWV3Qm94PSIwIDAgMjIwIDI4NCIgcm9sZT0iaW1nIiA+DQo8dGl0bGU+SEVYQUxPQ0sgbW9kdWxhciBpbnRlcmZhY2UgYXNzZXQ8L3RpdGxlPg0KPGRlZnM+PGxpbmVhckdyYWRpZW50IGlkPSJrcmFmdEZyb250IiB4MT0iMCIgeTE9IjAiIHgyPSIxIiB5Mj0iMSI+PHN0b3Agc3RvcC1jb2xvcj0iI0QzQjk5QSIvPjxzdG9wIG9mZnNldD0iMSIgc3RvcC1jb2xvcj0iI0EzODM2MyIvPjwvbGluZWFyR3JhZGllbnQ+ ...(+6912 chars)\",\"value\":\"36\"},{\"image\":\"data:image\\/svg+xml;base64,PHN2ZyB4bWxucz0iaHR0cDovL3d3dy53My5vcmcvMjAwMC9zdmciIHdpZHRoPSIyMjAiIGhlaWdodD0iMjg0IiB2aWV3Qm94PSIwIDAgMjIwIDI4NCIgcm9sZT0iaW1nIiA+DQo8dGl0bGU+SEVYQUxPQ0sgbW9kdWxhciBpbnRlcmZhY2UgYXNzZXQ8L3RpdGxlPg0KPGRlZnM+PGxpbmVhckdyYWRpZW50IGlkPSJrcmFmdEZyb250IiB4MT0iMCIgeTE9IjAiIHgyPSIxIiB5Mj0iMSI+PHN0b3Agc3RvcC1jb2xvcj0iI0QzQjk5QSIvPjxzdG9wIG9mZnNldD0iMSIgc3RvcC1jb2xvcj0iI0EzODM2MyIvPjwvbGluZWFyR3JhZGllbnQ+ ...(+6912 chars)\",\"value\":\"37\"},{\"image\":\"data:image\\/svg+xml;base64,PHN2ZyB4bWxucz0iaHR0cDovL3d3dy53My5vcmcvMjAwMC9zdmciIHdpZHRoPSIyMjAiIGhlaWdodD0iMjg0IiB2aWV3Qm94PSIwIDAgMjIwIDI4NCIgcm9sZT0iaW1nIiA+DQo8dGl0bGU+SEVYQUxPQ0sgbW9kdWxhciBpbnRlcmZhY2UgYXNzZXQ8L3RpdGxlPg0KPGRlZnM+PGxpbmVhckdyYWRpZW50IGlkPSJrcmFmdEZyb250IiB4MT0iMCIgeTE9IjAiIHgyPSIxIiB5Mj0iMSI+PHN0b3Agc3RvcC1jb2xvcj0iI0QzQjk5QSIvPjxzdG9wIG9mZnNldD0iMSIgc3RvcC1jb2xvcj0iI0EzODM2MyIvPjwvbGluZWFyR3JhZGllbnQ+ ...(+6912 chars)\",\"value\":\"38\"}],\"fixedAspectRatio\":\"on\"}},\"settings\":{\"BindingType\":\"signal\",\"backgroundColor\":[0,0,0],\"backgroundOffset\":0.14,\"backgroundOpacity\":1,\"blockOrientation\":\"Right\",\"fixedAspectRatio\":\"on\",\"showBackgroundColor\":false,\"value\":0,\"version\":\"R2026b\"},\"type\":\"MultistateImage\"}"
